simulink model "solar_pv_protected_c07_circuit"  (R2026b)
(part 2 of 16)

      | モデルの範囲　　　　; Simscape標準コンデンサの集中定数表現。材質、DCバイアス、周波数依存ESR/ESL、寿命・温度特性を型番から自動再現するモデルではない。
      | モデル設定　　　　　; c=470 µF、r=1 µΩ、g=0 S。これらは保存モデルの設定値であり、すべてが実部品の保証値という意味ではない。
      | 損失の扱い　　　　　; 保存モデルの直列抵抗rと実部品の周波数・温度依存ESRは区別する。容量値が一致しても損失・リプル電流・寿命の成立確認にはならない。
      | 確認の範囲　　　　　; 本説明は保存回路の部品情報・端子割当・既存設計意図を整理したもの。今回の説明更新によって新たな動作試験や実機検証を実施した意味ではない。
      | 設計記録　　　　　　; evaluation\component_annotations_20261022_r01\before_graph.json
      | evaluation\component_annotations_20261022_r01\before_metadata.json
      | evaluation\protection_capacitor_integration_20261021_r01\final_delivery\independent_readback\physical_bom.json
      | evaluation\protection_capacitor_integration_20261021_r01\capacitor_review\capacitor_inventory_after_c04.json
      | evaluation\layout_readability_20261022_r01\capacitor_review\exact_snapshot_capacitor_review.json
      | 
      | 【周波数・ノイズと配置の説明】
      | 周波数面の役割　　　; 12 V共通電源の負荷変動へ、比較的大きな電荷を供給する。
      | 対象周波数の目安　　; 起動や負荷切替えなど比較的低い周波数側の蓄積が主眼。ただしハイブリッド電解は一般的な液体電解と同一特性ではなく、型番別のインピーダンス曲線で分担を決める。
      | ノイズの発生源　　　; U10/U12の消費電流変化とゲートドライバ負荷。旧K1のコイル負荷は現回路の発生源として扱わない。
      | 他のコンデンサとの差; C45の22 µF MLCCはU11直近のリプル経路を補う。本品470 µFが現回路で必要最小かは未確定で、旧負荷由来の容量を残している。
      | 周波数説明の範囲　　; 狙うノイズの周波数と、この部品が実装後に有効な周波数範囲は別である。実効容量、等価直列抵抗、等価直列インダクタンス、配線を含む自己共振で変わるため、型番名や公称容量だけから有効帯域の上限を断定しない。
      | 周波数説明の根拠　　; 村田製作所：コンデンサのインピーダンス・ESRと周波数の関係
      | https://article.murata.com/en-global/article/impedance-esr-frequency-characteristics-in-capacitors
      | TRACO POWER：TSR 1WI datasheet
      | https://www.tracopower.com/tsr1wi-datasheet
      | 
      | 【この説明欄の略語・記号】
      | 用語1　　　　　　　 ; MLCC：Multilayer Ceramic Capacitor（積層セラミックコンデンサ）。薄いセラミック誘電体と電極を重ねたコンデンサ。対象周波数は容量・実装・寄生成分で変わるため、MLCCという分類だけでは決めない。
      | 用語2　　　　　　　 ; ESR：Equivalent Series Resistance（等価直列抵抗）。コンデンサの損失を直列抵抗で表した量。周波数・温度で変わり、損失とリプル電圧に関係する。
      | 用語3　　　　　　　 ; ESL：Equivalent Series Inductance（等価直列インダクタンス）。端子や電極などの寄生インダクタンスを表す。高い周波数ではバイパス効果を制限する。
      | 用語4　　　　　　　 ; DC：Direct Current（直流）。ここでは直流電源または直流成分。DCバイアスはコンデンサに重なる直流電圧を指す。
      | 用語5　　　　　　　 ; IC：Integrated Circuit（集積回路）。複数の電子素子と機能を小さな半導体チップに集積した部品。
      | 用語6　　　　　　　 ; GND：Ground（回路の基準電位・電流帰路）。この図の共通基準。保護接地や大地への接続を意味するとは限らない。
      settings: AttributesFormatString=|
      | ハイブリッド
      | 470 µF
  C47 : fl_lib/Electrical/Electrical Elements/Capacitor  Description=|  c=1e-06 F  r=1e-6 Ohm  g=0 1/Ohm  i_specify=off  i_priority=None  i=0 A  i_nominal_specify=off  i_nominal_value=1  i_nominal_unit=A  v_specify=off  v_priority=None  v=0 V  v_nominal_specify=off  v_nominal_value=1  v_nominal_unit=V  vc_specify=off  vc_priority=High  vc=0 V  vc_nominal_specify=off  vc_nominal_value=1  vc_nominal_unit=V
      | この回路での名前　　; C47
      | 部品名　　　　　　　; GRM21BR71H105KA12L
      | この回路での役割　　; 12 Vから5 Vを作る補助電源U12の入力を支え、電流の脈動を近くで受け止めるためのコンデンサ。
      | ここでの動き　　　　; U12の12 V入力P12と共通GNDの間に1 µFを置き、入力端子近くで電流の短い往復経路を作る。同じ12 VにつながるC45・C46が離れていても、U12の直近に電荷を用意する役割。
      | 
      | 【詳しい働き・仕様・接続・確認の範囲】
      | 部品種別　　　　　　; 積層セラミックコンデンサ（MLCC）
      | 部品分類　　　　　　; 積層セラミックコンデンサ（MLCC）
      | 公称値　　　　　　　; 1uF 50V X7R
      | 配置目的　　　　　　; 5Vレギュレータ入力局所バイパス。対象ICはU12（TSR 1-2450）。
      | 意図する動作　　　　; U12のP12入力/GND直近。 U12は12V入力で外付22µF必須条件には該当しないが、配線/高周波源インピーダンスを持つ1µF局所Cを維持。
      | 端子と接続　　　　　; 1 1 → P12、2 2 → GND
      | モデルの範囲　　　　; Simscape標準コンデンサの集中定数表現。材質、DCバイアス、周波数依存ESR/ESL、寿命・温度特性を型番から自動再現するモデルではない。
      | モデル設定　　　　　; c=1 µF、r=1 µΩ、g=0 S。これらは保存モデルの設定値であり、すべてが実部品の保証値という意味ではない。
      | 損失の扱い　　　　　; 保存モデルの直列抵抗rと実部品の周波数・温度依存ESRは区別する。容量値が一致しても損失・リプル電流・寿命の成立確認にはならない。
      | 確認の範囲　　　　　; 本説明は保存回路の部品情報・端子割当・既存設計意図を整理したもの。今回の説明更新によって新たな動作試験や実機検証を実施した意味ではない。
      | 設計記録　　　　　　; evaluation\component_annotations_20261022_r01\before_graph.json
      | evaluation\component_annotations_20261022_r01\before_metadata.json
      | evaluation\protection_capacitor_integration_20261021_r01\final_delivery\independent_readback\physical_bom.json
      | evaluation\protection_capacitor_integration_20261021_r01\capacitor_review\capacitor_inventory_after_c04.json
      | evaluation\layout_readability_20261022_r01\capacitor_review\exact_snapshot_capacitor_review.json
      | 
      | 【周波数・ノイズと配置の説明】
      | 周波数面の役割　　　; 5 V補助電源U12の入力直近で電流の脈動を受け止める。
      | 対象周波数の目安　　; U12のメーカー指定スイッチング周波数400～600 kHz（典型500 kHz）と高調波を対象とする。
      | ノイズの発生源　　　; U12が12 Vから5 Vへ降圧する内部スイッチング、およびU7の負荷変動。
      | 他のコンデンサとの差; 離れた12 V共通容量C45/C46と同じネットでも、U12直近の短い電流経路を作る点に意味がある。
      | 周波数説明の範囲　　; 狙うノイズの周波数と、この部品が実装後に有効な周波数範囲は別である。実効容量、等価直列抵抗、等価直列インダクタンス、配線を含む自己共振で変わるため、型番名や公称容量だけから有効帯域の上限を断定しない。
      | 周波数説明の根拠　　; TRACO POWER：TSR 1 datasheet
      | https://www.tracopower.com/products/tsr1.pdf
      | 村田製作所：コンデンサを使いこなす
      | https://www.murata.com/en-GB/products/emc/emifil/library/knowhow/basic/chapter06-p8
      | 
      | 【この説明欄の略語・記号】
      | 用語1　　　　　　　 ; MLCC：Multilayer Ceramic Capacitor（積層セラミックコンデンサ）。薄いセラミック誘電体と電極を重ねたコンデンサ。対象周波数は容量・実装・寄生成分で変わるため、MLCCという分類だけでは決めない。
      | 用語2　　　　　　　 ; ESR：Equivalent Series Resistance（等価直列抵抗）。コンデンサの損失を直列抵抗で表した量。周波数・温度で変わり、損失とリプル電圧に関係する。
      | 用語3　　　　　　　 ; ESL：Equivalent Series Inductance（等価直列インダクタンス）。端子や電極などの寄生インダクタンスを表す。高い周波数ではバイパス効果を制限する。
      | 用語4　　　　　　　 ; DC：Direct Current（直流）。ここでは直流電源または直流成分。DCバイアスはコンデンサに重なる直流電圧を指す。
      | 用語5　　　　　　　 ; X7R：セラミックコンデンサの温度特性記号。英語の頭文字ではなく分類コード。X＝下限−55 ℃、7＝上限+125 ℃、R＝その範囲の容量変化±15%。直流バイアスによる容量変化は別に確認する。
      | 用語6　　　　　　　 ; IC：Integrated Circuit（集積回路）。複数の電子素子と機能を小さな半導体チップに集積した部品。
      | 用語7　　　　　　　 ; GND：Ground（回路の基準電位・電流帰路）。この図の共通基準。保護接地や大地への接続を意味するとは限らない。
      settings: AttributesFormatString=|
      | MLCC
      | 1 µF
  C48 : fl_lib/Electrical/Electrical Elements/Capacitor  Description=|  c=2.2e-05 F  r=1e-6 Ohm  g=0 1/Ohm  i_specify=off  i_priority=None  i=0 A  i_nominal_specify=off  i_nominal_value=1  i_nominal_unit=A  v_specify=off  v_priority=None  v=0 V  v_nominal_specify=off  v_nominal_value=1  v_nominal_unit=V  vc_specify=off  vc_priority=High  vc=0 V  vc_nominal_specify=off  vc_nominal_value=1  vc_nominal_unit=V
      | この回路での名前　　; C48
      | 部品名　　　　　　　; GRM32ER71E226KE15L
      | この回路での役割　　; マイコン基板などへ渡す5 V電源に電荷を蓄え、消費電流の変化を支えるためのコンデンサ。
      | ここでの動き　　　　; 補助電源U12の出力P5と共通GNDの間に22 µFを置き、マイコン基板などが一時的に必要とする電荷を補う。マイコン基板内の各部品のすぐ近くにある小容量コンデンサを置き換えるものではない。
      | 
      | 【詳しい働き・仕様・接続・確認の範囲】
      | 部品種別　　　　　　; 積層セラミックコンデンサ（MLCC）
      | 部品分類　　　　　　; 積層セラミックコンデンサ（MLCC）
      | 公称値　　　　　　　; 22uF 25V X7R
      | 配置目的　　　　　　; 5V出力局所バルク。対象ICはU12（TSR 1-2450）。
      | 意図する動作　　　　; P5分配点とMCU負荷を結ぶ短い往復配線。 Pico無線/制御負荷の過渡とLED電流窓を守るため22µF維持。U12出力max470µFにも余裕。
      | 端子と接続　　　　　; 1 1 → P5、2 2 → GND
      | モデルの範囲　　　　; Simscape標準コンデンサの集中定数表現。材質、DCバイアス、周波数依存ESR/ESL、寿命・温度特性を型番から自動再現するモデルではない。
      | モデル設定　　　　　; c=22 µF、r=1 µΩ、g=0 S。これらは保存モデルの設定値であり、すべてが実部品の保証値という意味ではない。
      | 損失の扱い　　　　　; 保存モデルの直列抵抗rと実部品の周波数・温度依存ESRは区別する。容量値が一致しても損失・リプル電流・寿命の成立確認にはならない。
      | 確認の範囲　　　　　; 本説明は保存回路の部品情報・端子割当・既存設計意図を整理したもの。今回の説明更新によって新たな動作試験や実機検証を実施した意味ではない。
      | 設計記録　　　　　　; evaluation\component_annotations_20261022_r01\before_graph.json
      | evaluation\component_annotations_20261022_r01\before_metadata.json
      | evaluation\protection_capacitor_integration_20261021_r01\final_delivery\independent_readback\physical_bom.json
      | evaluation\protection_capacitor_integration_20261021_r01\capacitor_review\capacitor_inventory_after_c04.json
      | evaluation\layout_readability_20261022_r01\capacitor_review\exact_snapshot_capacitor_review.json
      | 
      | 【周波数・ノイズと配置の説明】
      | 周波数面の役割　　　; 5 V出力の局所蓄積としてRP2040基板などの負荷変動を支える。
      | 対象周波数の目安　　; U12の400～600 kHz（典型500 kHz）の変換成分と高調波、マイコン/無線負荷によるより遅い電流変化を対象にする。
      | ノイズの発生源　　　; U12内部スイッチングとPico Wの処理・通信に伴う電源電流変化。ゲートドライバ入力の発光ダイオードへ供給する電流の変化も5 V系に流れる。
      | 他のコンデンサとの差; 22 µFのMLCCでも電荷蓄積を担う。マイコン基板内の各IC直近の小容量バイパスまで置き換えるものではない。
      | 周波数説明の範囲　　; 狙うノイズの周波数と、この部品が実装後に有効な周波数範囲は別である。実効容量、等価直列抵抗、等価直列インダクタンス、配線を含む自己共振で変わるため、型番名や公称容量だけから有効帯域の上限を断定しない。
      | 周波数説明の根拠　　; TRACO POWER：TSR 1 datasheet
      | https://www.tracopower.com/products/tsr1.pdf
      | TDK：Low-ESL Multilayer Ceramic Capacitors
      | https://product.tdk.com/system/files/dam/doc/content/emc-guidebook/en/eemc_product_01.pdf
      | 村田製作所：コンデンサを使いこなす
      | https://www.murata.com/en-GB/products/emc/emifil/library/knowhow/basic/chapter06-p8
      | 
      | 【この説明欄の略語・記号】
      | 用語1　　　　　　　 ; MLCC：Multilayer Ceramic Capacitor（積層セラミックコンデンサ）。薄いセラミック誘電体と電極を重ねたコンデンサ。対象周波数は容量・実装・寄生成分で変わるため、MLCCという分類だけでは決めない。
      | 用語2　　　　　　　 ; ESR：Equivalent Series Resistance（等価直列抵抗）。コンデンサの損失を直列抵抗で表した量。周波数・温度で変わり、損失とリプル電圧に関係する。
      | 用語3　　　　　　　 ; ESL：Equivalent Series Inductance（等価直列インダクタンス）。端子や電極などの寄生インダクタンスを表す。高い周波数ではバイパス効果を制限する。
      | 用語4　　　　　　　 ; DC：Direct Current（直流）。ここでは直流電源または直流成分。DCバイアスはコンデンサに重なる直流電圧を指す。
      | 用語5　　　　　　　 ; X7R：セラミックコンデンサの温度特性記号。英語の頭文字ではなく分類コード。X＝下限−55 ℃、7＝上限+125 ℃、R＝その範囲の容量変化±15%。直流バイアスによる容量変化は別に確認する。
      | 用語6　　　　　　　 ; IC：Integrated Circuit（集積回路）。複数の電子素子と機能を小さな半導体チップに集積した部品。
      | 用語7　　　　　　　 ; MCU：Microcontroller Unit（マイクロコントローラ）。プログラムを実行し、測定値の処理や出力制御を担当する小型計算機。
      | 用語8　　　　　　　 ; LED：Light-Emitting Diode（発光ダイオード）。本回路のゲートドライバ入力では光によって信号を伝え、入力側と出力側を絶縁するために用いる。
      | 用語9　　　　　　　 ; GND：Ground（回路の基準電位・電流帰路）。この図の共通基準。保護接地や大地への接続を意味するとは限らない。
      settings: AttributesFormatString=|
      | MLCC
      | 22 µF
  C7 : fl_lib/Electrical/Electrical Elements/Capacitor  Description=|  c=3.3e-06 F  r=1e-6 Ohm  g=0 1/Ohm  i_specify=off  i_priority=None  i=0 A  i_nominal_specify=off  i_nominal_value=1  i_nominal_unit=A  v_specify=off  v_priority=None  v=0 V  v_nominal_specify=off  v_nominal_value=1  v_nominal_unit=V  vc_specify=off  vc_priority=High  vc=0 V  vc_nominal_specify=off  vc_nominal_value=1  vc_nominal_unit=V
      | この回路での名前　　; C7
      | 部品名　　　　　　　; R76IR433050H3J
      | この回路での役割　　; 主電力段の切替えに伴う短い電流を近くで受け持ち、入力側の大容量コンデンサを補うためのフィルムコンデンサ。
      | ここでの動き　　　　; 入力電源VINと共通GNDの間に置き、Q1・Q2の切替えに必要な電流の往復経路を短くする。C2〜C4の電解コンデンサとC8〜C10の積層セラミックコンデンサが受け持つ電流を補う設計。
      | 
      | 【詳しい働き・仕様・接続・確認の範囲】
      | 部品種別　　　　　　; フィルムコンデンサ
      | 部品分類　　　　　　; フィルムコンデンサ
      | 公称値　　　　　　　; 3.3 uF
      | 配置目的　　　　　　; 入力フィルム。対象はQ1/Q2、VIN、GND。
      | 意図する動作　　　　; 電力段のパルス電流閉路を短くし、電解だけへ高速成分を押し付けない。 3.3µF維持。10µFへの大型化は本削減数を増やさず、初回の要因を増やすため保留。
      | 端子と接続　　　　　; 2 n → GND、1 p → VIN
      | モデルの範囲　　　　; Simscape標準コンデンサの集中定数表現。材質、DCバイアス、周波数依存ESR/ESL、寿命・温度特性を型番から自動再現するモデルではない。
      | モデル設定　　　　　; c=3.3 µF、r=1 µΩ、g=0 S。これらは保存モデルの設定値であり、すべてが実部品の保証値という意味ではない。
      | 損失の扱い　　　　　; 保存モデルの直列抵抗rと実部品の周波数・温度依存ESRは区別する。容量値が一致しても損失・リプル電流・寿命の成立確認にはならない。
      | 確認の範囲　　　　　; 本説明は保存回路の部品情報・端子割当・既存設計意図を整理したもの。今回の説明更新によって新たな動作試験や実機検証を実施した意味ではない。
      | 設計記録　　　　　　; evaluation\component_annotations_20261022_r01\before_graph.json
      | evaluation\component_annotations_20261022_r01\before_metadata.json
      | evaluation\protection_capacitor_integration_20261021_r01\final_delivery\independent_readback\physical_bom.json
      | evaluation\protection_capacitor_integration_20261021_r01\capacitor_review\capacitor_inventory_after_c04.json
      | 
      | 【周波数・ノイズと配置の説明】
      | 周波数面の役割　　　; 主電力段の反復するパルス電流を受け、入力電解だけに高速成分が集中するのを補う。
      | 対象周波数の目安　　; 主スイッチング周波数とその高調波を対象とする。主電力段の既存比較計算では50 kHzを仮定している。これは比較シナリオの値であり、今回の保存図から実行中PWM周波数を測定した値ではない。 フィルムだから必ずMLCCと電解の中間周波数という固定分類にはしない。
      | ノイズの発生源　　　; Q1/Q2の切替えで入力ループの電流が急変する。配線や部品の寄生成分による振動も重なる。
      | 他のコンデンサとの差; 大容量のC2～C4は電荷蓄積、C8～C10は低い寄生インダクタンスを生かした局所的な帰路を狙う。本品3.3 µFはフィルムのパルス電流特性を使う意図であり、実際の分流は別確認。
      | 周波数説明の範囲　　; 狙うノイズの周波数と、この部品が実装後に有効な周波数範囲は別である。実効容量、等価直列抵抗、等価直列インダクタンス、配線を含む自己共振で変わるため、型番名や公称容量だけから有効帯域の上限を断定しない。
      | 周波数説明の根拠　　; 村田製作所：コンデンサのインピーダンス・ESRと周波数の関係
      | https://article.murata.com/en-global/article/impedance-esr-frequency-characteristics-in-capacitors
      | 村田製作所：コンデンサを使いこなす
      | https://www.murata.com/en-GB/products/emc/emifil/library/knowhow/basic/chapter06-p8
      | 
      | 【この説明欄の略語・記号】
      | 用語1　　　　　　　 ; MLCC：Multilayer Ceramic Capacitor（積層セラミックコンデンサ）。薄いセラミック誘電体と電極を重ねたコンデンサ。対象周波数は容量・実装・寄生成分で変わるため、MLCCという分類だけでは決めない。
      | 用語2　　　　　　　 ; ESR：Equivalent Series Resistance（等価直列抵抗）。コンデンサの損失を直列抵抗で表した量。周波数・温度で変わり、損失とリプル電圧に関係する。
      | 用語3　　　　　　　 ; ESL：Equivalent Series Inductance（等価直列インダクタンス）。端子や電極などの寄生インダクタンスを表す。高い周波数ではバイパス効果を制限する。
      | 用語4　　　　　　　 ; DC：Direct Current（直流）。ここでは直流電源または直流成分。DCバイアスはコンデンサに重なる直流電圧を指す。
      | 用語5　　　　　　　 ; PWM：Pulse Width Modulation（パルス幅変調）。周期に対するON時間の割合を変えて、スイッチの平均的な電力伝達を調整する方式。
      | 用語6　　　　　　　 ; GND：Ground（回路の基準電位・電流帰路）。この図の共通基準。保護接地や大地への接続を意味するとは限らない。
      | 用語7　　　　　　　 ; VIN/VOUT：入力電圧・出力電圧を表す端子／ネット名。INは入力、OUTは出力。電源変換器の電力端子なのか、検出用端子なのかは対象部品によって異なるため、端子と接続の説明に従う。
      settings: AttributesFormatString=|
      | フィルム
      | 3.3 µF
  C8 : fl_lib/Electrical/Electrical Elements/Capacitor  Description=|  c=2.2000000000000001e-06 F  r=1e-6 Ohm  g=0 1/Ohm  i_specify=off  i_priority=None  i=0 A  i_nominal_specify=off  i_nominal_value=1  i_nominal_unit=A  v_specify=off  v_priority=None  v=0 V  v_nominal_specify=off  v_nominal_value=1  v_nominal_unit=V  vc_specify=off  vc_priority=High  vc=0 V  vc_nominal_specify=off  vc_nominal_value=1  vc_nominal_unit=V
      | この回路での名前　　; C8
      | 部品名　　　　　　　; C5750X7T2E225K250KE
      | この回路での役割　　; 主電力段のすぐ近くで速い電流変化を受け止め、遠い電源配線へ流れ出す高周波成分を減らすためのコンデンサ。
      | ここでの動き　　　　; 入力電源VINと共通GNDの間に2.2 µFを3個並列に置き、Q1・Q2が切り替わる瞬間の電流に短い往復経路を作る。C2〜C4の大きな電荷蓄積を補う役割。
      | 
      | 【詳しい働き・仕様・接続・確認の範囲】
      | 部品種別　　　　　　; 積層セラミックコンデンサ（MLCC）
      | 部品分類　　　　　　; 積層セラミックコンデンサ（MLCC）
      | 公称値　　　　　　　; 2.2 uF
      | 配置目的　　　　　　; 入力高速バイパス。対象はQ1ドレインとQ2ソース間のホットループ。
      | 意図する動作　　　　; 現構成は2.2 µFを3個。電力段付近でパルス電流の短い往復経路を作る意図。DCバイアス下の実効容量と高周波の分流・寄生は公称容量だけでは保証しない。
      | 端子と接続　　　　　; 2 n → GND、1 p → VIN
      | モデルの範囲　　　　; Simscape標準コンデンサの集中定数表現。材質、DCバイアス、周波数依存ESR/ESL、寿命・温度特性を型番から自動再現するモデルではない。
      | モデル設定　　　　　; c=2.2 µF、r=1 µΩ、g=0 S。これらは保存モデルの設定値であり、すべてが実部品の保証値という意味ではない。
      | 損失の扱い　　　　　; 保存モデルの直列抵抗rと実部品の周波数・温度依存ESRは区別する。容量値が一致しても損失・リプル電流・寿命の成立確認にはならない。
      | 確認の範囲　　　　　; 本説明は保存回路の部品情報・端子割当・既存設計意図を整理したもの。今回の説明更新によって新たな動作試験や実機検証を実施した意味ではない。
      | 設計記録　　　　　　; evaluation\component_annotations_20261022_r01\before_graph.json
      | evaluation\component_annotations_20261022_r01\before_metadata.json
      | evaluation\protection_capacitor_integration_20261021_r01\final_delivery\independent_readback\physical_bom.json
      | evaluation\protection_capacitor_integration_20261021_r01\capacitor_review\capacitor_inventory_after_c04.json
      | 
      | 【周波数・ノイズと配置の説明】
      | 材質の分類　　　　　; 本品の温度特性分類はX7T。-55～125 ℃の範囲で容量変化+22/-33%を規定する分類コードであり、英単語の略ではない。これは温度による変化の分類で、直流電圧を加えた際の実効容量や高周波特性は別に確認する。
      | 周波数面の役割　　　; 入力側の速い電流変化を電力段の近くで受け止め、遠い電源配線へ流れる高周波成分を減らす。
      | 対象周波数の目安　　; 主スイッチング周波数とその高調波、切替え端の速い変化を対象とする。主電力段の既存比較計算では50 kHzを仮定している。これは比較シナリオの値であり、今回の保存図から実行中PWM周波数を測定した値ではない。 50 kHzなら100 kHz、150 kHzなども成分となり、端の速さや寄生共振によってMHz域も検討対象になる。ただしMHz域での本品の有効性を保証した意味ではない。
      | ノイズの発生源　　　; Q1のオン期間に主電力段へ流れ込む入力電流が脈動し、Q1/Q2の切替え時には寄生容量の充放電電流も加わる。配線の寄生インダクタンスは急な電流変化を電圧の突起や振動に変える。
      | 他のコンデンサとの差; C2～C4の470 µF電解が比較的長い時間の電荷を補い、本品2.2 µFは短い局所経路を作る。C7フィルムとも分担し、3種類の役割には重なりがある。
      | 周波数説明の範囲　　; 狙うノイズの周波数と、この部品が実装後に有効な周波数範囲は別である。実効容量、等価直列抵抗、等価直列インダクタンス、配線を含む自己共振で変わるため、型番名や公称容量だけから有効帯域の上限を断定しない。
      | 周波数説明の根拠　　; TDK：C5750X7T2E225K250KE
      | https://product.tdk.com/ja/search/capacitor/ceramic/mlcc/info?part_no=C5750X7T2E225K250KE
      | 村田製作所：コンデンサのインピーダンス・ESRと周波数の関係
      | https://article.murata.com/en-global/article/impedance-esr-frequency-characteristics-in-capacitors
      | 村田製作所：コンデンサを使いこなす
      | https://www.murata.com/en-GB/products/emc/emifil/library/knowhow/basic/chapter06-p8
      | 
      | 【この説明欄の略語・記号】
      | 用語1　　　　　　　 ; MLCC：Multilayer Ceramic Capacitor（積層セラミックコンデンサ）。薄いセラミック誘電体と電極を重ねたコンデンサ。対象周波数は容量・実装・寄生成分で変わるため、MLCCという分類だけでは決めない。
      | 用語2　　　　　　　 ; ESR：Equivalent Series Resistance（等価直列抵抗）。コンデンサの損失を直列抵抗で表した量。周波数・温度で変わり、損失とリプル電圧に関係する。
      | 用語3　　　　　　　 ; ESL：Equivalent Series Inductance（等価直列インダクタンス）。端子や電極などの寄生インダクタンスを表す。高い周波数ではバイパス効果を制限する。
      | 用語4　　　　　　　 ; DC：Direct Current（直流）。ここでは直流電源または直流成分。DCバイアスはコンデンサに重なる直流電圧を指す。
      | 用語5　　　　　　　 ; X7T：セラミックコンデンサの温度特性記号。英語の頭文字ではなく分類コード。X＝下限−55 ℃、7＝上限+125 ℃、T＝容量変化+22%/−33%。直流バイアスによる容量変化は別に確認する。
      | 用語6　　　　　　　 ; PWM：Pulse Width Modulation（パルス幅変調）。周期に対するON時間の割合を変えて、スイッチの平均的な電力伝達を調整する方式。
      | 用語7　　　　　　　 ; GND：Ground（回路の基準電位・電流帰路）。この図の共通基準。保護接地や大地への接続を意味するとは限らない。
      | 用語8　　　　　　　 ; VIN/VOUT：入力電圧・出力電圧を表す端子／ネット名。INは入力、OUTは出力。電源変換器の電力端子なのか、検出用端子なのかは対象部品によって異なるため、端子と接続の説明に従う。
      settings: AttributesFormatString=|
      | MLCC
      | 2.2 µF
  C9 : fl_lib/Electrical/Electrical Elements/Capacitor  Description=|  c=2.2000000000000001e-06 F  r=1e-6 Ohm  g=0 1/Ohm  i_specify=off  i_priority=None  i=0 A  i_nominal_specify=off  i_nominal_value=1  i_nominal_unit=A  v_specify=off  v_priority=None  v=0 V  v_nominal_specify=off  v_nominal_value=1  v_nominal_unit=V  vc_specify=off  vc_priority=High  vc=0 V  vc_nominal_specify=off  vc_nominal_value=1  vc_nominal_unit=V
      | この回路での名前　　; C9
      | 部品名　　　　　　　; C5750X7T2E225K250KE
      | この回路での役割　　; 主電力段のすぐ近くで速い電流変化を受け止め、遠い電源配線へ流れ出す高周波成分を減らすためのコンデンサ。
      | ここでの動き　　　　; 入力電源VINと共通GNDの間に2.2 µFを3個並列に置き、Q1・Q2が切り替わる瞬間の電流に短い往復経路を作る。C2〜C4の大きな電荷蓄積を補う役割。
      | 
      | 【詳しい働き・仕様・接続・確認の範囲】
      | 部品種別　　　　　　; 積層セラミックコンデンサ（MLCC）
      | 部品分類　　　　　　; 積層セラミックコンデンサ（MLCC）
      | 公称値　　　　　　　; 2.2 uF
      | 配置目的　　　　　　; 入力高速バイパス。対象はQ1ドレインとQ2ソース間のホットループ。
      | 意図する動作　　　　; 現構成は2.2 µFを3個。電力段付近でパルス電流の短い往復経路を作る意図。DCバイアス下の実効容量と高周波の分流・寄生は公称容量だけでは保証しない。
      | 端子と接続　　　　　; 2 n → GND、1 p → VIN
      | モデルの範囲　　　　; Simscape標準コンデンサの集中定数表現。材質、DCバイアス、周波数依存ESR/ESL、寿命・温度特性を型番から自動再現するモデルではない。
      | モデル設定　　　　　; c=2.2 µF、r=1 µΩ、g=0 S。これらは保存モデルの設定値であり、すべてが実部品の保証値という意味ではない。
      | 損失の扱い　　　　　; 保存モデルの直列抵抗rと実部品の周波数・温度依存ESRは区別する。容量値が一致しても損失・リプル電流・寿命の成立確認にはならない。
      | 確認の範囲　　　　　; 本説明は保存回路の部品情報・端子割当・既存設計意図を整理したもの。今回の説明更新によって新たな動作試験や実機検証を実施した意味ではない。
      | 設計記録　　　　　　; evaluation\component_annotations_20261022_r01\before_graph.json
      | evaluation\component_annotations_20261022_r01\before_metadata.json
      | evaluation\protection_capacitor_integration_20261021_r01\final_delivery\independent_readback\physical_bom.json
      | evaluation\protection_capacitor_integration_20261021_r01\capacitor_review\capacitor_inventory_after_c04.json
      | 
      | 【周波数・ノイズと配置の説明】
      | 材質の分類　　　　　; 本品の温度特性分類はX7T。-55～125 ℃の範囲で容量変化+22/-33%を規定する分類コードであり、英単語の略ではない。これは温度による変化の分類で、直流電圧を加えた際の実効容量や高周波特性は別に確認する。
      | 周波数面の役割　　　; 入力側の速い電流変化を電力段の近くで受け止め、遠い電源配線へ流れる高周波成分を減らす。
      | 対象周波数の目安　　; 主スイッチング周波数とその高調波、切替え端の速い変化を対象とする。主電力段の既存比較計算では50 kHzを仮定している。これは比較シナリオの値であり、今回の保存図から実行中PWM周波数を測定した値ではない。 50 kHzなら100 kHz、150 kHzなども成分となり、端の速さや寄生共振によってMHz域も検討対象になる。ただしMHz域での本品の有効性を保証した意味ではない。
      | ノイズの発生源　　　; Q1のオン期間に主電力段へ流れ込む入力電流が脈動し、Q1/Q2の切替え時には寄生容量の充放電電流も加わる。配線の寄生インダクタンスは急な電流変化を電圧の突起や振動に変える。
      | 他のコンデンサとの差; C2～C4の470 µF電解が比較的長い時間の電荷を補い、本品2.2 µFは短い局所経路を作る。C7フィルムとも分担し、3種類の役割には重なりがある。
      | 周波数説明の範囲　　; 狙うノイズの周波数と、この部品が実装後に有効な周波数範囲は別である。実効容量、等価直列抵抗、等価直列インダクタンス、配線を含む自己共振で変わるため、型番名や公称容量だけから有効帯域の上限を断定しない。
      | 周波数説明の根拠　　; TDK：C5750X7T2E225K250KE
      | https://product.tdk.com/ja/search/capacitor/ceramic/mlcc/info?part_no=C5750X7T2E225K250KE
      | 村田製作所：コンデンサのインピーダンス・ESRと周波数の関係
      | https://article.murata.com/en-global/article/impedance-esr-frequency-characteristics-in-capacitors
      | 村田製作所：コンデンサを使いこなす
      | https://www.murata.com/en-GB/products/emc/emifil/library/knowhow/basic/chapter06-p8
      | 
      | 【この説明欄の略語・記号】
      | 用語1　　　　　　　 ; MLCC：Multilayer Ceramic Capacitor（積層セラミックコンデンサ）。薄いセラミック誘電体と電極を重ねたコンデンサ。対象周波数は容量・実装・寄生成分で変わるため、MLCCという分類だけでは決めない。
      | 用語2　　　　　　　 ; ESR：Equivalent Series Resistance（等価直列抵抗）。コンデンサの損失を直列抵抗で表した量。周波数・温度で変わり、損失とリプル電圧に関係する。
      | 用語3　　　　　　　 ; ESL：Equivalent Series Inductance（等価直列インダクタンス）。端子や電極などの寄生インダクタンスを表す。高い周波数ではバイパス効果を制限する。
      | 用語4　　　　　　　 ; DC：Direct Current（直流）。ここでは直流電源または直流成分。DCバイアスはコンデンサに重なる直流電圧を指す。
      | 用語5　　　　　　　 ; X7T：セラミックコンデンサの温度特性記号。英語の頭文字ではなく分類コード。X＝下限−55 ℃、7＝上限+125 ℃、T＝容量変化+22%/−33%。直流バイアスによる容量変化は別に確認する。
      | 用語6　　　　　　　 ; PWM：Pulse Width Modulation（パルス幅変調）。周期に対するON時間の割合を変えて、スイッチの平均的な電力伝達を調整する方式。
      | 用語7　　　　　　　 ; GND：Ground（回路の基準電位・電流帰路）。この図の共通基準。保護接地や大地への接続を意味するとは限らない。
      | 用語8　　　　　　　 ; VIN/VOUT：入力電圧・出力電圧を表す端子／ネット名。INは入力、OUTは出力。電源変換器の電力端子なのか、検出用端子なのかは対象部品によって異なるため、端子と接続の説明に従う。
      settings: AttributesFormatString=|
      | MLCC
      | 2.2 µF
  CircuitNet_BAT_PLUS : ConnectionLabel  Description=|  Label=BAT_PLUS
      | この回路での名前　　; BAT_PLUS
      | 種別　　　　　　　　; ConnectionLabel
      | この回路での役割　　; 保護回路の出力、充電経路のヒューズF3、電池側電圧測定の分圧抵抗R22上側を結ぶ。BT1正極へはF3を介してつながる。
      | この場所の直接接続　; F3（BT1と充電器の間の充電経路を保護するヒューズ／25A DC）: 2
      |                     ; P_COUT（保護回路出力側のコンデンサ／330 µF）: P
      |                     ; P_R7（BAT_PLUSからP_FBへ接続し、P_R8とともに出力電圧クランプの帰還比を作る／236 kΩ）: 1
      |                     ; P_RSNS（保護ICの電流検出抵抗／2.7 mΩ）: 2
      |                     ; P_U1（保護MOSFETを制御する保護IC／LTC4364IMS-1#PBF）: OUT
      | 直接接続の範囲　　　; このラベルから実際の線・分岐・明示的な境界端子だけを追った接続。同名ラベルによる離れた場所への接続はこの欄に含めない。
      | 同一ネットの主接続　; F3（BT1と充電器の間の充電経路を保護するヒューズ／25A DC）: 2
      |                     ; R22（電池側電圧の分圧抵抗・上側／75 kohm 0.1%）: 1
      |                     ; P_U1（保護MOSFETを制御する保護IC／LTC4364IMS-1#PBF）: OUT
      |                     ; P_RSNS（保護ICの電流検出抵抗／2.7 mΩ）: 2
      |                     ; P_COUT（保護回路出力側のコンデンサ／330 µF）: P
      |                     ; P_R7（BAT_PLUSからP_FBへ接続し、P_R8とともに出力電圧クランプの帰還比を作る／236 kΩ）: 1
      | 部品を介する経路　　; R22→R23の上側抵抗とR24の下側抵抗で分圧し、C21とADC U1のCH6へ渡す。ADC入力はBAT_PLUSと同じ導線ではない。F3の反対側はBT1正極のBAT_RAW。
      | 同一ネット全端子　　; F3: 2
      |                     ; P_COUT: P
      |                     ; P_R7: 1
      |                     ; P_RSNS: 2
      |                     ; P_U1: OUT
      |                     ; R22: 1
      | 接続部品数　　　　　; 6部品（部品番号で集計。同一ネット全体）
      | 接続端子数　　　　　; 6端子（423端子の部品対応表で集計。ラベル・境界ポートの重複は含めない）
      | この場所の端子数　　; 5端子／5部品（同名ラベルによる接続を除く）
      | 同階層同名ラベル数　; 2個（このラベル自身を含む）
      | 全階層の接続ラベル　; 2個（実際に同じノードへつながるラベル。名前が違う別名も含む）
      | 接続ルール　　　　　; 同じ階層の同じラベル名を仮想配線として結ぶ。別のSubsystem内とは名前だけでつながらず、明示的なConnection Portと配線をたどる。色は用途の表示であり接続を決めない。
      | 確認の範囲　　　　　; 現在の保存回路の端子・配線から求めた静的接続。抵抗やICの内部を導線として短絡せずに集計した。説明の更新は動作シミュレーション、タイミング、実部品の性能・実機動作を保証するものではない。
      | 記録の基準　　　　　; measurement_label_layout_20261022_r01/after_layout_graph.json。部品対応表は端子名の対応付けにのみ使用。
      | 
      | 【この説明欄の略語・記号】
      | 用語1　　　　　　　 ; DC：Direct Current（直流）。ここでは直流電源または直流成分。DCバイアスはコンデンサに重なる直流電圧を指す。
      | 用語2　　　　　　　 ; ADC：Analog-to-Digital Converter（アナログ・デジタル変換器）。測定電圧をデジタル値へ変換する回路。電流や温度も、センサーで電圧へ変換した後に読み取る。
      | 用語3　　　　　　　 ; IC：Integrated Circuit（集積回路）。複数の電子素子と機能を小さな半導体チップに集積した部品。
      | 用語4　　　　　　　 ; CH：Channel（測定チャネル）。CH0〜CH7はADCの入力番号であり、同時測定を意味しない。
      | 用語5　　　　　　　 ; MOSFET：Metal-Oxide-Semiconductor Field-Effect Transistor（金属・酸化膜・半導体構造の電界効果トランジスタ）。ゲートとソースの電圧でドレインとソースの導通を制御する素子。N-MOSはNチャネル型を表す。
      | 用語6　　　　　　　 ; FB：Feedback（帰還）。出力などを検出して内部制御へ戻すための信号・端子。
  CircuitNet_MAIN_EN : ConnectionLabel  Description=|  Label=MAIN_EN
      | この回路での名前　　; MAIN_EN
      | 種別　　　　　　　　; ConnectionLabel
      | この回路での役割　　; RP2040基板U7のGP11から、保護回路の停止入力へ指令を渡す。直接同じノードなのは直列抵抗P_RSHDN_SERの入力側までで、保護ICのSHDNにはこの抵抗を介して接続する。
      | この場所の直接接続　; U7（RP2040搭載Pico W／SC0918）: 15(GP11)
      | 直接接続の範囲　　　; このラベルから実際の線・分岐・明示的な境界端子だけを追った接続。同名ラベルによる離れた場所への接続はこの欄に含めない。
      | 同一ネットの主接続　; U7（RP2040搭載Pico W／SC0918）: 15(GP11)
      |                     ; P_RSHDN_SER（RP2040のMAIN_ENとLTC4364のSHDN間へ入る／1 kΩ）: 1
      | 同一ネット全端子　　; P_RSHDN_SER: 1
      |                     ; U7: 15(GP11)
      | 接続部品数　　　　　; 2部品（部品番号で集計。同一ネット全体）
      | 接続端子数　　　　　; 2端子（423端子の部品対応表で集計。ラベル・境界ポートの重複は含めない）
      | この場所の端子数　　; 1端子／1部品（同名ラベルによる接続を除く）
      | 同階層同名ラベル数　; 2個（このラベル自身を含む）
      | 全階層の接続ラベル　; 2個（実際に同じノードへつながるラベル。名前が違う別名も含む）
      | 接続ルール　　　　　; 同じ階層の同じラベル名を仮想配線として結ぶ。別のSubsystem内とは名前だけでつながらず、明示的なConnection Portと配線をたどる。色は用途の表示であり接続を決めない。
      | 確認の範囲　　　　　; 現在の保存回路の端子・配線から求めた静的接続。抵抗やICの内部を導線として短絡せずに集計した。説明の更新は動作シミュレーション、タイミング、実部品の性能・実機動作を保証するものではない。
      | 記録の基準　　　　　; measurement_label_layout_20261022_r01/after_layout_graph.json。部品対応表は端子名の対応付けにのみ使用。
      | 
      | 【この説明欄の略語・記号】
      | 用語1　　　　　　　 ; IC：Integrated Circuit（集積回路）。複数の電子素子と機能を小さな半導体チップに集積した部品。
      | 用語2　　　　　　　 ; GPIO：General-Purpose Input/Output（汎用入出力端子）。入力・出力や周辺機能に割り当てられる端子。GPの後の数字はRP2040の端子信号番号で、基板上の物理ピン番号とは別。
      | 用語3　　　　　　　 ; SHDN：Shutdown（停止制御端子）。LTC4364ではLowで停止を指示する。Highは動作許可であり、保護判定を無効にするものではない。
      | 用語4　　　　　　　 ; EN：Enable（動作許可）。対象機能の動作を許可する信号。端子ごとの有効レベルや接続状態に従う。
  CircuitNet_VOUT : ConnectionLabel  Description=|  Label=VOUT
      | この回路での名前　　; VOUT
      | 種別　　　　　　　　; ConnectionLabel
      | この回路での役割　　; 降圧電力段の出力平滑コンデンサ、L1後の出力電流検出抵抗R2の出力側、保護回路の入力を結ぶ。保護回路より上流の電圧をR19の分圧回路でも測る。
      | この場所の直接接続　; C13（出力バルク／470 uF）: 1(p)
      |                     ; C14（出力バルク／470 uF）: 1(p)
      |                     ; C15（出力高速バイパス／10 uF）: 1(p)
      |                     ; C16（出力高速バイパス／10 uF）: 1(p)
      |                     ; R2（L1直後の出力電流を検出する4端子シャント抵抗／CSS4J-4026R-1L00F）: IM, KM
      | 直接接続の範囲　　　; このラベルから実際の線・分岐・明示的な境界端子だけを追った接続。同名ラベルによる離れた場所への接続はこの欄に含めない。
      | 同一ネットの主接続　; C13（出力バルク／470 uF）: 1(p)
      |                     ; C14（出力バルク／470 uF）: 1(p)
      |                     ; C15（出力高速バイパス／10 uF）: 1(p)
      |                     ; C16（出力高速バイパス／10 uF）: 1(p)
      |                     ; R2（L1直後の出力電流を検出する4端子シャント抵抗／CSS4J-4026R-1L00F）: IM, KM
      |                     ; U3（L1直後の出力電流の検出アンプ／INA241A3IDDFR）: 1(IN-)
      |                     ; P_Q1（充電器から蓄電池へ向かう電力経路を開閉し、起動時や異常時には流れる電流・出力電圧を制限するために置く／150V / 4.8mOhm max at25C10V）: D
      |                     ; R19（保護回路より上流の出力電圧の分圧抵抗・上側／75 kohm 0.1%）: 1
      | 部品を介する経路　　; R19→R20の上側抵抗とR21の下側抵抗で分圧し、C20とADC U1のCH2へ渡す。ADC入力はVOUTと同じ導線ではない。電流の測定経路はR2両端→U3→R26/C25→U1 CH3。R2より下流に出力コンデンサがあるため、過渡時の電池端子電流と常時同一ではない。
      | 同一ネット全端子　　; C13: 1(p)
      |                     ; C14: 1(p)
      |                     ; C15: 1(p)
      |                     ; C16: 1(p)
      |                     ; P_Q1: D
      |                     ; P_R1: 1
      |                     ; P_R4: 1
      |                     ; R2: IM, KM
      |                     ; R19: 1
      |                     ; U3: 1(IN-)
      | 接続部品数　　　　　; 10部品（部品番号で集計。同一ネット全体）
      | 接続端子数　　　　　; 11端子（423端子の部品対応表で集計。ラベル・境界ポートの重複は含めない）
      | この場所の端子数　　; 6端子／5部品（同名ラベルによる接続を除く）
      | 同階層同名ラベル数　; 3個（このラベル自身を含む）
      | 全階層の接続ラベル　; 5個（実際に同じノードへつながるラベル。名前が違う別名も含む）
      | 接続ルール　　　　　; 同じ階層の同じラベル名を仮想配線として結ぶ。別のSubsystem内とは名前だけでつながらず、明示的なConnection Portと配線をたどる。色は用途の表示であり接続を決めない。
      | 確認の範囲　　　　　; 現在の保存回路の端子・配線から求めた静的接続。抵抗やICの内部を導線として短絡せずに集計した。説明の更新は動作シミュレーション、タイミング、実部品の性能・実機動作を保証するものではない。
      | 記録の基準　　　　　; measurement_label_layout_20261022_r01/after_layout_graph.json。部品対応表は端子名の対応付けにのみ使用。
      | 
      | 【この説明欄の略語・記号】
      | 用語1　　　　　　　 ; ADC：Analog-to-Digital Converter（アナログ・デジタル変換器）。測定電圧をデジタル値へ変換する回路。電流や温度も、センサーで電圧へ変換した後に読み取る。
      | 用語2　　　　　　　 ; IC：Integrated Circuit（集積回路）。複数の電子素子と機能を小さな半導体チップに集積した部品。
      | 用語3　　　　　　　 ; CH：Channel（測定チャネル）。CH0〜CH7はADCの入力番号であり、同時測定を意味しない。
      | 用語4　　　　　　　 ; GND：Ground（回路の基準電位・電流帰路）。この図の共通基準。保護接地や大地への接続を意味するとは限らない。
      | 用語5　　　　　　　 ; VIN/VOUT：入力電圧・出力電圧を表す端子／ネット名。INは入力、OUTは出力。電源変換器の電力端子なのか、検出用端子なのかは対象部品によって異なるため、端子と接続の説明に従う。
      | 用語6　　　　　　　 ; IP/IM・KP/KM：4端子シャントの端子役割を区別する設計上の表記。IP/IMは主電流端子、KP/KMはKelvin（4端子測定）の検出端子。P/Mは正側・負側の区別であり、端子番号は採用部品の割当を参照する。
      | 用語7　　　　　　　 ; IN+/IN−：差動測定の正側・負側入力。電流検出アンプは両端子の電圧差を読む。IN−は必ずGNDという意味ではない。
  Connection Label : ConnectionLabel  Tag=simrfV2util1/Connection Label  Description=|  Label=GP6
      | この回路での名前　　; GP6
      | 種別　　　　　　　　; ConnectionLabel
      | この回路での役割　　; RP2040基板U7のGP6と、高側ゲート駆動の入力抵抗R34を結ぶPWM指令線。R34の先でQ3の第1ゲートを駆動し、光ゲートドライバの入力LED電流を制御する構成。
      | この場所の直接接続　; U7（RP2040搭載Pico W／SC0918）: 9(GP6)
      | 直接接続の範囲　　　; このラベルから実際の線・分岐・明示的な境界端子だけを追った接続。同名ラベルによる離れた場所への接続はこの欄に含めない。
      | 同一ネットの主接続　; U7（RP2040搭載Pico W／SC0918）: 9(GP6)
      |                     ; R34（高側LED制御MOSFETのゲート直列抵抗／330 ohm 1%）: 1
      | 同一ネット全端子　　; R34: 1
      |                     ; U7: 9(GP6)
      | 接続部品数　　　　　; 2部品（部品番号で集計。同一ネット全体）
      | 接続端子数　　　　　; 2端子（423端子の部品対応表で集計。ラベル・境界ポートの重複は含めない）
      | この場所の端子数　　; 1端子／1部品（同名ラベルによる接続を除く）
      | 同階層同名ラベル数　; 2個（このラベル自身を含む）
      | 全階層の接続ラベル　; 2個（実際に同じノードへつながるラベル。名前が違う別名も含む）
      | 接続ルール　　　　　; 同じ階層の同じラベル名を仮想配線として結ぶ。別のSubsystem内とは名前だけでつながらず、明示的なConnection Portと配線をたどる。色は用途の表示であり接続を決めない。
      | 確認の範囲　　　　　; 現在の保存回路の端子・配線から求めた静的接続。抵抗やICの内部を導線として短絡せずに集計した。説明の更新は動作シミュレーション、タイミング、実部品の性能・実機動作を保証するものではない。
      | 記録の基準　　　　　; measurement_label_layout_20261022_r01/after_layout_graph.json。部品対応表は端子名の対応付けにのみ使用。
      | 
      | 【この説明欄の略語・記号】
      | 用語1　　　　　　　 ; IC：Integrated Circuit（集積回路）。複数の電子素子と機能を小さな半導体チップに集積した部品。
      | 用語2　　　　　　　 ; PWM：Pulse Width Modulation（パルス幅変調）。周期に対するON時間の割合を変えて、スイッチの平均的な電力伝達を調整する方式。
      | 用語3　　　　　　　 ; GPIO：General-Purpose Input/Output（汎用入出力端子）。入力・出力や周辺機能に割り当てられる端子。GPの後の数字はRP2040の端子信号番号で、基板上の物理ピン番号とは別。
      | 用語4　　　　　　　 ; MOSFET：Metal-Oxide-Semiconductor Field-Effect Transistor（金属・酸化膜・半導体構造の電界効果トランジスタ）。ゲートとソースの電圧でドレインとソースの導通を制御する素子。N-MOSはNチャネル型を表す。
      | 用語5　　　　　　　 ; LED：Light-Emitting Diode（発光ダイオード）。本回路のゲートドライバ入力では光によって信号を伝え、入力側と出力側を絶縁するために用いる。
  Connection Label1 : ConnectionLabel  Tag=simrfV2util1/Connection Label  Description=|  Label=GP6
      | この回路での名前　　; GP6
      | 種別　　　　　　　　; ConnectionLabel
      | この回路での役割　　; RP2040基板U7のGP6と、高側ゲート駆動の入力抵抗R34を結ぶPWM指令線。R34の先でQ3の第1ゲートを駆動し、光ゲートドライバの入力LED電流を制御する構成。
      | この場所の直接接続　; R34（高側LED制御MOSFETのゲート直列抵抗／330 ohm 1%）: 1
      | 直接接続の範囲　　　; このラベルから実際の線・分岐・明示的な境界端子だけを追った接続。同名ラベルによる離れた場所への接続はこの欄に含めない。
      | 同一ネットの主接続　; U7（RP2040搭載Pico W／SC0918）: 9(GP6)
      |                     ; R34（高側LED制御MOSFETのゲート直列抵抗／330 ohm 1%）: 1
      | 同一ネット全端子　　; R34: 1
      |                     ; U7: 9(GP6)
      | 接続部品数　　　　　; 2部品（部品番号で集計。同一ネット全体）
      | 接続端子数　　　　　; 2端子（423端子の部品対応表で集計。ラベル・境界ポートの重複は含めない）
      | この場所の端子数　　; 1端子／1部品（同名ラベルによる接続を除く）
      | 同階層同名ラベル数　; 2個（このラベル自身を含む）
      | 全階層の接続ラベル　; 2個（実際に同じノードへつながるラベル。名前が違う別名も含む）
      | 接続ルール　　　　　; 同じ階層の同じラベル名を仮想配線として結ぶ。別のSubsystem内とは名前だけでつながらず、明示的なConnection Portと配線をたどる。色は用途の表示であり接続を決めない。
      | 確認の範囲　　　　　; 現在の保存回路の端子・配線から求めた静的接続。抵抗やICの内部を導線として短絡せずに集計した。説明の更新は動作シミュレーション、タイミング、実部品の性能・実機動作を保証するものではない。
      | 記録の基準　　　　　; measurement_label_layout_20261022_r01/after_layout_graph.json。部品対応表は端子名の対応付けにのみ使用。
      | 
      | 【この説明欄の略語・記号】
      | 用語1　　　　　　　 ; IC：Integrated Circuit（集積回路）。複数の電子素子と機能を小さな半導体チップに集積した部品。
      | 用語2　　　　　　　 ; PWM：Pulse Width Modulation（パルス幅変調）。周期に対するON時間の割合を変えて、スイッチの平均的な電力伝達を調整する方式。
      | 用語3　　　　　　　 ; GPIO：General-Purpose Input/Output（汎用入出力端子）。入力・出力や周辺機能に割り当てられる端子。GPの後の数字はRP2040の端子信号番号で、基板上の物理ピン番号とは別。
      | 用語4　　　　　　　 ; MOSFET：Metal-Oxide-Semiconductor Field-Effect Transistor（金属・酸化膜・半導体構造の電界効果トランジスタ）。ゲートとソースの電圧でドレインとソースの導通を制御する素子。N-MOSはNチャネル型を表す。
      | 用語5　　　　　　　 ; LED：Light-Emitting Diode（発光ダイオード）。本回路のゲートドライバ入力では光によって信号を伝え、入力側と出力側を絶縁するために用いる。
  Connection Label2 : ConnectionLabel  Tag=simrfV2util1/Connection Label  Description=|  Label=GP7
      | この回路での名前　　; GP7
      | 種別　　　　　　　　; ConnectionLabel
      | この回路での役割　　; RP2040基板U7のGP7と、低側ゲート駆動の入力抵抗R41を結ぶPWM指令線。R41の先でQ3の第2ゲートを駆動し、光ゲートドライバの入力LED電流を制御する構成。
      | この場所の直接接続　; U7（RP2040搭載Pico W／SC0918）: 10(GP7)
      | 直接接続の範囲　　　; このラベルから実際の線・分岐・明示的な境界端子だけを追った接続。同名ラベルによる離れた場所への接続はこの欄に含めない。
      | 同一ネットの主接続　; U7（RP2040搭載Pico W／SC0918）: 10(GP7)
      |                     ; R41（低側LED制御MOSFETのゲート直列抵抗／330 ohm 1%）: 1
      | 同一ネット全端子　　; R41: 1
      |                     ; U7: 10(GP7)
      | 接続部品数　　　　　; 2部品（部品番号で集計。同一ネット全体）
      | 接続端子数　　　　　; 2端子（423端子の部品対応表で集計。ラベル・境界ポートの重複は含めない）
      | この場所の端子数　　; 1端子／1部品（同名ラベルによる接続を除く）
      | 同階層同名ラベル数　; 2個（このラベル自身を含む）
      | 全階層の接続ラベル　; 2個（実際に同じノードへつながるラベル。名前が違う別名も含む）
      | 接続ルール　　　　　; 同じ階層の同じラベル名を仮想配線として結ぶ。別のSubsystem内とは名前だけでつながらず、明示的なConnection Portと配線をたどる。色は用途の表示であり接続を決めない。
      | 確認の範囲　　　　　; 現在の保存回路の端子・配線から求めた静的接続。抵抗やICの内部を導線として短絡せずに集計した。説明の更新は動作シミュレーション、タイミング、実部品の性能・実機動作を保証するものではない。
      | 記録の基準　　　　　; measurement_label_layout_20261022_r01/after_layout_graph.json。部品対応表は端子名の対応付けにのみ使用。
      | 
      | 【この説明欄の略語・記号】
      | 用語1　　　　　　　 ; IC：Integrated Circuit（集積回路）。複数の電子素子と機能を小さな半導体チップに集積した部品。
      | 用語2　　　　　　　 ; PWM：Pulse Width Modulation（パルス幅変調）。周期に対するON時間の割合を変えて、スイッチの平均的な電力伝達を調整する方式。
      | 用語3　　　　　　　 ; GPIO：General-Purpose Input/Output（汎用入出力端子）。入力・出力や周辺機能に割り当てられる端子。GPの後の数字はRP2040の端子信号番号で、基板上の物理ピン番号とは別。
      | 用語4　　　　　　　 ; MOSFET：Metal-Oxide-Semiconductor Field-Effect Transistor（金属・酸化膜・半導体構造の電界効果トランジスタ）。ゲートとソースの電圧でドレインとソースの導通を制御する素子。N-MOSはNチャネル型を表す。
      | 用語5　　　　　　　 ; LED：Light-Emitting Diode（発光ダイオード）。本回路のゲートドライバ入力では光によって信号を伝え、入力側と出力側を絶縁するために用いる。
  Connection Label3 : ConnectionLabel  Tag=simrfV2util1/Connection Label  Description=|  Label=GP7
      | この回路での名前　　; GP7
      | 種別　　　　　　　　; ConnectionLabel
      | この回路での役割　　; RP2040基板U7のGP7と、低側ゲート駆動の入力抵抗R41を結ぶPWM指令線。R41の先でQ3の第2ゲートを駆動し、光ゲートドライバの入力LED電流を制御する構成。
      | この場所の直接接続　; R41（低側LED制御MOSFETのゲート直列抵抗／330 ohm 1%）: 1
      | 直接接続の範囲　　　; このラベルから実際の線・分岐・明示的な境界端子だけを追った接続。同名ラベルによる離れた場所への接続はこの欄に含めない。
      | 同一ネットの主接続　; U7（RP2040搭載Pico W／SC0918）: 10(GP7)
      |                     ; R41（低側LED制御MOSFETのゲート直列抵抗／330 ohm 1%）: 1
      | 同一ネット全端子　　; R41: 1
      |                     ; U7: 10(GP7)
      | 接続部品数　　　　　; 2部品（部品番号で集計。同一ネット全体）
      | 接続端子数　　　　　; 2端子（423端子の部品対応表で集計。ラベル・境界ポートの重複は含めない）
      | この場所の端子数　　; 1端子／1部品（同名ラベルによる接続を除く）
      | 同階層同名ラベル数　; 2個（このラベル自身を含む）
      | 全階層の接続ラベル　; 2個（実際に同じノードへつながるラベル。名前が違う別名も含む）
      | 接続ルール　　　　　; 同じ階層の同じラベル名を仮想配線として結ぶ。別のSubsystem内とは名前だけでつながらず、明示的なConnection Portと配線をたどる。色は用途の表示であり接続を決めない。
      | 確認の範囲　　　　　; 現在の保存回路の端子・配線から求めた静的接続。抵抗やICの内部を導線として短絡せずに集計した。説明の更新は動作シミュレーション、タイミング、実部品の性能・実機動作を保証するものではない。
      | 記録の基準　　　　　; measurement_label_layout_20261022_r01/after_layout_graph.json。部品対応表は端子名の対応付けにのみ使用。
      | 
      | 【この説明欄の略語・記号】
      | 用語1　　　　　　　 ; IC：Integrated Circuit（集積回路）。複数の電子素子と機能を小さな半導体チップに集積した部品。
      | 用語2　　　　　　　 ; PWM：Pulse Width Modulation（パルス幅変調）。周期に対するON時間の割合を変えて、スイッチの平均的な電力伝達を調整する方式。
      | 用語3　　　　　　　 ; GPIO：General-Purpose Input/Output（汎用入出力端子）。入力・出力や周辺機能に割り当てられる端子。GPの後の数字はRP2040の端子信号番号で、基板上の物理ピン番号とは別。
      | 用語4　　　　　　　 ; MOSFET：Metal-Oxide-Semiconductor Field-Effect Transistor（金属・酸化膜・半導体構造の電界効果トランジスタ）。ゲートとソースの電圧でドレインとソースの導通を制御する素子。N-MOSはNチャネル型を表す。
      | 用語5　　　　　　　 ; LED：Light-Emitting Diode（発光ダイオード）。本回路のゲートドライバ入力では光によって信号を伝え、入力側と出力側を絶縁するために用いる。
  Connection Label4 : ConnectionLabel  Tag=simrfV2util1/Connection Label  Description=|  Label=BAT_RAW
      | この回路での名前　　; BAT_RAW
      | 種別　　　　　　　　; ConnectionLabel
      | この回路での役割　　; 蓄電池BT1の正極と、充電経路のヒューズF3・補助電源分岐のヒューズF4を結ぶ。電池端子側の電源ノード。
      | この場所の直接接続　; F4（BT1から補助電源への分岐を保護するヒューズ／3.2A DC）: 1
      | 直接接続の範囲　　　; このラベルから実際の線・分岐・明示的な境界端子だけを追った接続。同名ラベルによる離れた場所への接続はこの欄に含めない。
      | 同一ネットの主接続　; BT1（充電先の蓄電池／51.2V 100Ah LiFePO4）: +
      |                     ; F3（BT1と充電器の間の充電経路を保護するヒューズ／25A DC）: 1
      |                     ; F4（BT1から補助電源への分岐を保護するヒューズ／3.2A DC）: 1
      | 同一ネット全端子　　; BT1: +
      |                     ; F3: 1
      |                     ; F4: 1
      | 接続部品数　　　　　; 3部品（部品番号で集計。同一ネット全体）
      | 接続端子数　　　　　; 3端子（423端子の部品対応表で集計。ラベル・境界ポートの重複は含めない）
      | この場所の端子数　　; 1端子／1部品（同名ラベルによる接続を除く）
      | 同階層同名ラベル数　; 2個（このラベル自身を含む）
      | 全階層の接続ラベル　; 2個（実際に同じノードへつながるラベル。名前が違う別名も含む）
      | 接続ルール　　　　　; 同じ階層の同じラベル名を仮想配線として結ぶ。別のSubsystem内とは名前だけでつながらず、明示的なConnection Portと配線をたどる。色は用途の表示であり接続を決めない。
      | 確認の範囲　　　　　; 現在の保存回路の端子・配線から求めた静的接続。抵抗やICの内部を導線として短絡せずに集計した。説明の更新は動作シミュレーション、タイミング、実部品の性能・実機動作を保証するものではない。
      | 記録の基準　　　　　; measurement_label_layout_20261022_r01/after_layout_graph.json。部品対応表は端子名の対応付けにのみ使用。
      | 
      | 【この説明欄の略語・記号】
      | 用語1　　　　　　　 ; DC：Direct Current（直流）。ここでは直流電源または直流成分。DCバイアスはコンデンサに重なる直流電圧を指す。
      | 用語2　　　　　　　 ; IC：Integrated Circuit（集積回路）。複数の電子素子と機能を小さな半導体チップに集積した部品。
      | 用語3　　　　　　　 ; LiFePO4：Lithium Iron Phosphate（リン酸鉄リチウム）。電池の正極材料を示す化学式。英語の頭文字を並べた略語ではない。
  Connection Label5 : ConnectionLabel  Tag=simrfV2util1/Connection Label  Description=|  Label=BAT_RAW
      | この回路での名前　　; BAT_RAW
      | 種別　　　　　　　　; ConnectionLabel
      | この回路での役割　　; 蓄電池BT1の正極と、充電経路のヒューズF3・補助電源分岐のヒューズF4を結ぶ。電池端子側の電源ノード。
      | この場所の直接接続　; BT1（充電先の蓄電池／51.2V 100Ah LiFePO4）: +
      |                     ; F3（BT1と充電器の間の充電経路を保護するヒューズ／25A DC）: 1
      | 直接接続の範囲　　　; このラベルから実際の線・分岐・明示的な境界端子だけを追った接続。同名ラベルによる離れた場所への接続はこの欄に含めない。
      | 同一ネットの主接続　; BT1（充電先の蓄電池／51.2V 100Ah LiFePO4）: +
      |                     ; F3（BT1と充電器の間の充電経路を保護するヒューズ／25A DC）: 1
      |                     ; F4（BT1から補助電源への分岐を保護するヒューズ／3.2A DC）: 1
      | 同一ネット全端子　　; BT1: +
      |                     ; F3: 1
      |                     ; F4: 1
      | 接続部品数　　　　　; 3部品（部品番号で集計。同一ネット全体）
      | 接続端子数　　　　　; 3端子（423端子の部品対応表で集計。ラベル・境界ポートの重複は含めない）
      | この場所の端子数　　; 2端子／2部品（同名ラベルによる接続を除く）
      | 同階層同名ラベル数　; 2個（このラベル自身を含む）
      | 全階層の接続ラベル　; 2個（実際に同じノードへつながるラベル。名前が違う別名も含む）
      | 接続ルール　　　　　; 同じ階層の同じラベル名を仮想配線として結ぶ。別のSubsystem内とは名前だけでつながらず、明示的なConnection Portと配線をたどる。色は用途の表示であり接続を決めない。
      | 確認の範囲　　　　　; 現在の保存回路の端子・配線から求めた静的接続。抵抗やICの内部を導線として短絡せずに集計した。説明の更新は動作シミュレーション、タイミング、実部品の性能・実機動作を保証するものではない。
      | 記録の基準　　　　　; measurement_label_layout_20261022_r01/after_layout_graph.json。部品対応表は端子名の対応付けにのみ使用。
      | 
      | 【この説明欄の略語・記号】
      | 用語1　　　　　　　 ; DC：Direct Current（直流）。ここでは直流電源または直流成分。DCバイアスはコンデンサに重なる直流電圧を指す。
      | 用語2　　　　　　　 ; IC：Integrated Circuit（集積回路）。複数の電子素子と機能を小さな半導体チップに集積した部品。
      | 用語3　　　　　　　 ; LiFePO4：Lithium Iron Phosphate（リン酸鉄リチウム）。電池の正極材料を示す化学式。英語の頭文字を並べた略語ではない。
  D1 : ee_lib/Semiconductors & Converters/Diode  Description=|  Vf=0.6 V  Ron=0.3 Ohm  Goff=1e-8 S  N_series=1  N_parallel=1  ZenerEnable=true  BV=15 V  Rz=0.3 Ohm  enable_fault_composite=simscape.enum.onoff.off  i_specify=off  i_priority=None  i=0 A  i_nominal_specify=off  i_nominal_value=1  i_nominal_unit=A  v_specify=off  v_priority=None  v=0 V  v_nominal_specify=off  v_nominal_value=1  v_nominal_unit=V  ModelType=ee.enum.diode.idealModelType.pwl  TableType=ee.enum.diode.tableType.IfMat  IfMat=[.07, .12, .19, 1.75, 4.24, 7.32, 11.2; .16, .3, .72, 2.14, 5.02, 8.35, 13.12] A  VfMat=[.9, 1.15, 1.25, 1.5, 1.75, 2.17, 2.6, 2.85; .58, .68, .75, 1.1, 1.38, 1.77, 2.27, 2.7] V  TjVec=[25, 125] degC  VfVec=[.5, .7, .9, 1.3, 1.7, 2.1, 2.5] V  IfVec=[.1, .2, .5, 1, 2, 4, 7, 10] A  IrMat=[1e-06, 2e-06, 5e-06, 1e-05, 2.5e-05, 5e-05, .0001; 2e-06, 5e-06, 1e-05, 4e-05, 8e-05, .0002, .0005] A  VrMat=[10, 100, 200, 250, 300, 325, 350; 10, 70, 160, 220, 270, 300, 320] V  VrVec=[10, 20, 40, 50, 70, 80, 100] V  IrVec=[1e-06, 2e-06, 5e-06, 1e-05, 2e-05, 5e-05, .0001] A  rec_loss_model=ee.enum.diode.reverseRecoveryModelTabulateUpTo3D.fixed  ErecVal=0 J  scaleWithIandV=true  ErecMat=zeros(2, 3) J  ErecMat3D=zeros(2, 3, 2) J  TjrecVec=[25, 125] degC  IfrecVec=[.1, 1, 10] A  IrecVal=10 A  VrecVal=10 V  VrecVec=[0, 100] V  tFilter=1 / 1000 / 100 s  thermal_network_parameterization=ee.enum.thermalNetworkTopology.junctionCase  Rth=[0, 10] K/W  Rth_Cauer=[1, 3, 10] K/W  Rth_Foster=[.08, .14, .22, .16] K/W  thermal_mass_parameterization=ee.enum.thermalNetwork.timeconstant  thermal_mass=[0, 1] J/K  thermal_mass_Cauer=[.1, .3, 1] J/K  thermal_mass_Foster=[.001, .005, .05, .5] J/K  thermal_time_constant=[0, 10] s  thermal_time_constant_Cauer=[1, 3, 10] s  thermal_time_constant_Foster=[7e-05, .0007, .01, .08] s  thermal_mass_initial_temperatures=[25, 25] degC  thermal_mass_initial_temperatures_Cauer=[25, 25, 25] degC  thermal_mass_initial_temperatures_Foster=[25, 25, 25, 25] degC  junction_thermal_mass=0.01 J/K  junction_temperature_specify=off  junction_temperature_priority=None  junction_temperature=25 degC  junction_temperature_nominal_specify=off  junction_temperature_nominal_value=1  junction_temperature_nominal_unit=degC  ThermalPort=false  ModelTypePhysical=ee.enum.diode.physicalModelType.exponential  prmExp=ee.enum.diode.expParam.useTwo  I12=[.0137, .545] A  V12=[.6, .7] V  IS=1e-12 A  ec=1  I1=0.0137 A  V1=0.6 V  RS=0 Ohm  C_param=ee.enum.diode.capParam.fixed  CJ=0 pF  CJ0=5 pF  Vvec=[.1, 10, 100] V  Cvec=[3.5, 1, .4] pF  VJ=1 V  Mgrad=0.5  FC=0.5  Q_param=ee.enum.diode.recoveryParam.off  iRM=-7.15 A  iF=4 A  didt=-750 A/us  trr_factor=3  trr=115 ns  Qrr=150 nA*s  Vr=-600 V  Ls=150 nH  Erec=0.03 J  TT=50 ns  tau=100 ns  T_param=ee.enum.diode.temperatureParam.off  Tmeas=25 degC  I1_T2=0.245 A  V1_T2=0.5 V  IS_T2=1.25e-7 A  Tmeas2=125 degC  EG_param=ee.enum.diode.egapParam.material_si  EG=1.11 eV  XTI_param=ee.enum.diode.xtiParam.pn  XTI=3  dBVdT=0 V/K  Tdevice=25 degC  i_capacitor_specify=off  i_capacitor_priority=None  i_capacitor=0 A  i_capacitor_nominal_specify=off  i_capacitor_nominal_value=1  i_capacitor_nominal_unit=A  Qj_specify=off  Qj_priority=None  Qj=0 C  Qj_nominal_specify=off  Qj_nominal_value=1  Qj_nominal_unit=uC
      | この回路での名前　　; D1
      | 部品名　　　　　　　; BZT52H-C15,115
      | この回路での役割　　; 上側MOSFET Q1のゲートに過大な電圧がかかるのを抑える保護用ダイオード。
      | ここでの動き　　　　; Q1のゲートとソースSWの間に接続する。両者の電圧差が上がったときに電流を逃がし、ゲート電圧の上昇を抑える。
      | 
      | 【詳しい働き・仕様・接続・確認の範囲】
      | 部品種別　　　　　　; 上側ゲート保護ツェナーダイオード
      | 公称値　　　　　　　; 15V gate clamp
      | 配置目的　　　　　　; Q1のゲート–ソース間電圧が過大になるのを抑えるため、GATE_H–SW間へ配置する。
      | 意図する動作　　　　; 比較する電圧はGND基準ではなくQ1のソースSW基準。ツェナーの公称電圧は理想的な硬い電圧上限ではない。
      | 端子と接続　　　　　; 1 K → GATE_H、2 A → SW
      | モデルの範囲　　　　; Simscapeダイオード素子による近似。順方向損失、漏れ、温度依存、逆回復・接合容量の型番固有特性を完全に再現するものではない。
      | モデル設定　　　　　; Vf=600 mV、Ron=300 mΩ、BV=15 V。これらは保存モデルの設定値であり、すべてが実部品の保証値という意味ではない。
      | 確認の範囲　　　　　; 本説明は保存回路の部品情報・端子割当・既存設計意図を整理したもの。今回の説明更新によって新たな動作試験や実機検証を実施した意味ではない。
      | 設計記録　　　　　　; evaluation\component_annotations_20261022_r01\before_graph.json
      | evaluation\component_annotations_20261022_r01\before_metadata.json
      | evaluation\protection_capacitor_integration_20261021_r01\final_delivery\independent_readback\physical_bom.json
      | 
      | 【この説明欄の略語・記号】
      | 用語1　　　　　　　 ; MOSFET：Metal-Oxide-Semiconductor Field-Effect Transistor（金属・酸化膜・半導体構造の電界効果トランジスタ）。ゲートとソースの電圧でドレインとソースの導通を制御する素子。N-MOSはNチャネル型を表す。
      | 用語2　　　　　　　 ; BV：Breakdown Voltage（降伏電圧）。ダイオードなどに逆方向電圧を加えたときの降伏特性を表すモデル値。
      | 用語3　　　　　　　 ; Vf：Forward Voltage（順方向電圧）。ダイオードが順方向に電流を流すときの電圧降下。電流・温度で変わる。
      | 用語4　　　　　　　 ; Ron：On-Resistance（導通抵抗）。ここでは半導体ブロックのON状態の抵抗近似に用いる設定名。
      | 用語5　　　　　　　 ; GND：Ground（回路の基準電位・電流帰路）。この図の共通基準。保護接地や大地への接続を意味するとは限らない。
      | 用語6　　　　　　　 ; SW：Switching Node（スイッチング点）。主電力段の上下MOSFETとL1がつながる、電圧が高速に切り替わる点。GNDとは別電位。
      settings: AttributesFormatString=ツェナー 15 V
  D2 : ee_lib/Semiconductors & Converters/Diode  Description=|  Vf=0.6 V  Ron=0.3 Ohm  Goff=1e-8 S  N_series=1  N_parallel=1  ZenerEnable=true  BV=15 V  Rz=0.3 Ohm  enable_fault_composite=simscape.enum.onoff.off  i_specify=off  i_priority=None  i=0 A  i_nominal_specify=off  i_nominal_value=1  i_nominal_unit=A  v_specify=off  v_priority=None  v=0 V  v_nominal_specify=off  v_nominal_value=1  v_nominal_unit=V  ModelType=ee.enum.diode.idealModelType.pwl  TableType=ee.enum.diode.tableType.IfMat  IfMat=[.07, .12, .19, 1.75, 4.24, 7.32, 11.2; .16, .3, .72, 2.14, 5.02, 8.35, 13.12] A  VfMat=[.9, 1.15, 1.25, 1.5, 1.75, 2.17, 2.6, 2.85; .58, .68, .75, 1.1, 1.38, 1.77, 2.27, 2.7] V  TjVec=[25, 125] degC  VfVec=[.5, .7, .9, 1.3, 1.7, 2.1, 2.5] V  IfVec=[.1, .2, .5, 1, 2, 4, 7, 10] A  IrMat=[1e-06, 2e-06, 5e-06, 1e-05, 2.5e-05, 5e-05, .0001; 2e-06, 5e-06, 1e-05, 4e-05, 8e-05, .0002, .0005] A  VrMat=[10, 100, 200, 250, 300, 325, 350; 10, 70, 160, 220, 270, 300, 320] V  VrVec=[10, 20, 40, 50, 70, 80, 100] V  IrVec=[1e-06, 2e-06, 5e-06, 1e-05, 2e-05, 5e-05, .0001] A  rec_loss_model=ee.enum.diode.reverseRecoveryModelTabulateUpTo3D.fixed  ErecVal=0 J  scaleWithIandV=true  ErecMat=zeros(2, 3) J  ErecMat3D=zeros(2, 3, 2) J  TjrecVec=[25, 125] degC  IfrecVec=[.1, 1, 10] A  IrecVal=10 A  VrecVal=10 V  VrecVec=[0, 100] V  tFilter=1 / 1000 / 100 s  thermal_network_parameterization=ee.enum.thermalNetworkTopology.junctionCase  Rth=[0, 10] K/W  Rth_Cauer=[1, 3, 10] K/W  Rth_Foster=[.08, .14, .22, .16] K/W  thermal_mass_parameterization=ee.enum.thermalNetwork.timeconstant  thermal_mass=[0, 1] J/K  thermal_mass_Cauer=[.1, .3, 1] J/K  thermal_mass_Foster=[.001, .005, .05, .5] J/K  thermal_time_constant=[0, 10] s  thermal_time_constant_Cauer=[1, 3, 10] s  thermal_time_constant_Foster=[7e-05, .0007, .01, .08] s  thermal_mass_initial_temperatures=[25, 25] degC  thermal_mass_initial_temperatures_Cauer=[25, 25, 25] degC  thermal_mass_initial_temperatures_Foster=[25, 25, 25, 25] degC  junction_thermal_mass=0.01 J/K  junction_temperature_specify=off  junction_temperature_priority=None  junction_temperature=25 degC  junction_temperature_nominal_specify=off  junction_temperature_nominal_value=1  junction_temperature_nominal_unit=degC  ThermalPort=false  ModelTypePhysical=ee.enum.diode.physicalModelType.exponential  prmExp=ee.enum.diode.expParam.useTwo  I12=[.0137, .545] A  V12=[.6, .7] V  IS=1e-12 A  ec=1  I1=0.0137 A  V1=0.6 V  RS=0 Ohm  C_param=ee.enum.diode.capParam.fixed  CJ=0 pF  CJ0=5 pF  Vvec=[.1, 10, 100] V  Cvec=[3.5, 1, .4] pF  VJ=1 V  Mgrad=0.5  FC=0.5  Q_param=ee.enum.diode.recoveryParam.off  iRM=-7.15 A  iF=4 A  didt=-750 A/us  trr_factor=3  trr=115 ns  Qrr=150 nA*s  Vr=-600 V  Ls=150 nH  Erec=0.03 J  TT=50 ns  tau=100 ns  T_param=ee.enum.diode.temperatureParam.off  Tmeas=25 degC  I1_T2=0.245 A  V1_T2=0.5 V  IS_T2=1.25e-7 A  Tmeas2=125 degC  EG_param=ee.enum.diode.egapParam.material_si  EG=1.11 eV  XTI_param=ee.enum.diode.xtiParam.pn  XTI=3  dBVdT=0 V/K  Tdevice=25 degC  i_capacitor_specify=off  i_capacitor_priority=None  i_capacitor=0 A  i_capacitor_nominal_specify=off  i_capacitor_nominal_value=1  i_capacitor_nominal_unit=A  Qj_specify=off  Qj_priority=None  Qj=0 C  Qj_nominal_specify=off  Qj_nominal_value=1  Qj_nominal_unit=uC
      | この回路での名前　　; D2
      | 部品名　　　　　　　; BZT52H-C15,115
      | この回路での役割　　; 下側MOSFET Q2のゲートに過大な電圧がかかるのを抑える保護用ダイオード。
      | ここでの動き　　　　; Q2のゲートとソース側GNDの間に接続し、両者の電圧差が上がったときに電流を逃がす。
      | 
      | 【詳しい働き・仕様・接続・確認の範囲】
      | 部品種別　　　　　　; 下側ゲート保護ツェナーダイオード
      | 公称値　　　　　　　; 15V gate clamp
      | 配置目的　　　　　　; Q2のゲート–ソース間電圧が過大になるのを抑えるため、GATE_L–GND間へ配置する。
      | 意図する動作　　　　; 連続・パルス電力、動抵抗、配線寄生を含むクランプ性能は未確認。
      | 端子と接続　　　　　; 1 K → GATE_L、2 A → GND
      | モデルの範囲　　　　; Simscapeダイオード素子による近似。順方向損失、漏れ、温度依存、逆回復・接合容量の型番固有特性を完全に再現するものではない。
      | モデル設定　　　　　; Vf=600 mV、Ron=300 mΩ、BV=15 V。これらは保存モデルの設定値であり、すべてが実部品の保証値という意味ではない。
      | 確認の範囲　　　　　; 本説明は保存回路の部品情報・端子割当・既存設計意図を整理したもの。今回の説明更新によって新たな動作試験や実機検証を実施した意味ではない。
      | 設計記録　　　　　　; evaluation\component_annotations_20261022_r01\before_graph.json
      | evaluation\component_annotations_20261022_r01\before_metadata.json
      | evaluation\protection_capacitor_integration_20261021_r01\final_delivery\independent_readback\physical_bom.json
      | 
      | 【この説明欄の略語・記号】
      | 用語1　　　　　　　 ; BV：Breakdown Voltage（降伏電圧）。ダイオードなどに逆方向電圧を加えたときの降伏特性を表すモデル値。
      | 用語2　　　　　　　 ; Vf：Forward Voltage（順方向電圧）。ダイオードが順方向に電流を流すときの電圧降下。電流・温度で変わる。
      | 用語3　　　　　　　 ; Ron：On-Resistance（導通抵抗）。ここでは半導体ブロックのON状態の抵抗近似に用いる設定名。
      | 用語4　　　　　　　 ; GND：Ground（回路の基準電位・電流帰路）。この図の共通基準。保護接地や大地への接続を意味するとは限らない。
      settings: AttributesFormatString=ツェナー 15 V
  D3 : Subsystem  Description=|  mask(Simscape実部品合成記号){PartRef=D3, PartMPN=SS14-E3/61T, PartValue=SS14-E3/61T, DesignValue=40V 1A Schottky VSYS OR, SourceRef=vishay_ss14}
      | この回路での名前　　; D3
      | 部品名　　　　　　　; SS14-E3/61T
      | この回路での役割　　; マイコン基板U7へ5 Vを渡し、基板側から補助5 V電源へ電流が戻るのを抑えるダイオード。
      | ここでの動き　　　　; 補助5 V電源からマイコンの電源入力へ向かう方向には電流を通し、逆方向は抑える。電流を通す際には電圧降下と損失が生じる。
      | 
      | 【詳しい働き・仕様・接続・確認の範囲】
      | 部品種別　　　　　　; Pico電源用ショットキーダイオード
      | 公称値　　　　　　　; 40V 1A Schottky VSYS OR
      | 配置目的　　　　　　; P5からVSYS_5Vへ電力を供給し、VSYS側から5 V電源側への逆向き電流を抑える。
      | 意図する動作　　　　; 順方向電圧による電圧低下・損失がある。図面の方向はA=P5、K=VSYS_5V。USBなど他電源との全状態での適合は別確認。
      | 端子と接続　　　　　; 1 K → VSYS_5V、2 A → P5
      | モデルの範囲　　　　; Simscapeダイオード素子による近似。順方向損失、漏れ、温度依存、逆回復・接合容量の型番固有特性を完全に再現するものではない。
      | モデル設定　　　　　; Vf=600 mV、Ron=300 mΩ、BV=30 V。これらは保存モデルの設定値であり、すべてが実部品の保証値という意味ではない。
      | 確認の範囲　　　　　; 本説明は保存回路の部品情報・端子割当・既存設計意図を整理したもの。今回の説明更新によって新たな動作試験や実機検証を実施した意味ではない。
      | 設計記録　　　　　　; evaluation\component_annotations_20261022_r01\before_graph.json
      | evaluation\component_annotations_20261022_r01\before_metadata.json
      | evaluation\protection_capacitor_integration_20261021_r01\final_delivery\independent_readback\physical_bom.json
      | 
      | 【この説明欄の略語・記号】
      | 用語1　　　　　　　 ; USB：Universal Serial Bus（USB通信・給電規格）。Pico基板の接続・給電経路として現れる名称。
      | 用語2　　　　　　　 ; BV：Breakdown Voltage（降伏電圧）。ダイオードなどに逆方向電圧を加えたときの降伏特性を表すモデル値。
      | 用語3　　　　　　　 ; Vf：Forward Voltage（順方向電圧）。ダイオードが順方向に電流を流すときの電圧降下。電流・温度で変わる。
      | 用語4　　　　　　　 ; Ron：On-Resistance（導通抵抗）。ここでは半導体ブロックのON状態の抵抗近似に用いる設定名。
      settings: AttributesFormatString=Schottky SS14
      mask Display:
      | color('black');
      | plot([0 .34],[.5 .5]);
      | plot([.34 .34 .66 .34],[.2 .8 .5 .2]);
      | plot([.58 .66 .66 .74],[.8 .8 .2 .2]);
      | plot([.66 1],[.5 .5]);
      | text(0,.82,'2:A','horizontalAlignment','left');
      | text(1,.82,'1:K','horizontalAlignment','right');
  F1 : ee_lib/Switches & Breakers/Fuse  Description=|  prm=1  I_rated=1 A  melt_margin=1  T_fuse=0 s  I2t=1 A^2*s  I_vec=[1.9, 2, 2.5, 30] A  t_vec=[10000, 1, .3, .001] s  R_closed=0.01 Ohm  G_open=1e-8 1/Ohm  exposemeasurement=ee.enum.exposemeasurement.hidden
      | この回路での名前　　; F1
      | 部品名　　　　　　　; 0001.2706.11
      | この回路での役割　　; 12 V電源モジュールU11へ向かう補助電源入力の過電流に対処するヒューズ。
      | ここでの動き　　　　; 電池からU11へ流れる電流の経路に直列に入る。異常電流が続いたときに溶断して回路を切ることを狙う。補助分岐配線を受け持つF4との役割は別。
      | 
      | 【詳しい働き・仕様・接続・確認の範囲】
      | 部品種別　　　　　　; 補助電源モジュール用ヒューズ
      | 公称値　　　　　　　; 1.6A 300VDC time-lag T SMD
      | 配置目的　　　　　　; U11を含む補助電源入力の過電流に対処するために入れる。
      | 意図する動作　　　　; F4の補助配線保護とは保護対象が異なる。遮断協調・DC遮断能力・配線温度は公称電流だけでは保証されない。
      | 端子と接続　　　　　; 1 1 → BAT_AUX_FUSED、2 2 → BAT_AUX
      | モデルの範囲　　　　; Simscape標準ヒューズ。製品の時間–電流曲線、I²t、DCアーク遮断、遮断容量に適合済みのモデルではない。
      | モデル設定　　　　　; I_rated=1 A、R_closed=10 mΩ、melt_margin=1 。これらは保存モデルの設定値であり、すべてが実部品の保証値という意味ではない。
      | 確認の範囲　　　　　; 本説明は保存回路の部品情報・端子割当・既存設計意図を整理したもの。今回の説明更新によって新たな動作試験や実機検証を実施した意味ではない。
      | 設計記録　　　　　　; evaluation\component_annotations_20261022_r01\before_graph.json
      | evaluation\component_annotations_20261022_r01\before_metadata.json
      | evaluation\protection_capacitor_integration_20261021_r01\final_delivery\independent_readback\physical_bom.json
      | 
      | 【この説明欄の略語・記号】
      | 用語1　　　　　　　 ; DC：Direct Current（直流）。ここでは直流電源または直流成分。DCバイアスはコンデンサに重なる直流電圧を指す。
      | 用語2　　　　　　　 ; SMD：Surface-Mount Device（表面実装部品）。基板表面のパッドへはんだ付けする形式の部品。
      settings: AttributesFormatString=1.6A 300VDC time-lag T SMD
  F2 : ee_lib/Switches & Breakers/Fuse  Description=|  prm=1  I_rated=1 A  melt_margin=1  T_fuse=0 s  I2t=1 A^2*s  I_vec=[1.9, 2, 2.5, 30] A  t_vec=[10000, 1, .3, .001] s  R_closed=0.01 Ohm  G_open=1e-8 1/Ohm  exposemeasurement=ee.enum.exposemeasurement.hidden
      | この回路での名前　　; F2
      | 部品名　　　　　　　; HP10M20
      | この回路での役割　　; 太陽電池から充電器へ向かう入力配線を、過電流から保護するためのヒューズ。
      | ここでの動き　　　　; パネル列の出力に直列に入り、異常電流が続いたときに溶断して経路を切る。実際の遮断条件は電流の大きさと継続時間などに依存する。
      | 
      | 【詳しい働き・仕様・接続・確認の範囲】
      | 部品種別　　　　　　; PV入力ヒューズ
      | 公称値　　　　　　　; 20A gPV
      | 配置目的　　　　　　; PV入力配線の過電流保護を担う。
      | 意図する動作　　　　; 20 A gPVの部品情報を保持。パネル列の短絡電流、逆給電、直流電圧に対する適合・遮断協調は別確認。
      | 端子と接続　　　　　; 1 1 → PV_RAW、2 2 → PV_FUSED
      | モデルの範囲　　　　; Simscape標準ヒューズ。製品の時間–電流曲線、I²t、DCアーク遮断、遮断容量に適合済みのモデルではない。
      | モデル設定　　　　　; I_rated=1 A、R_closed=10 mΩ、melt_margin=1 。これらは保存モデルの設定値であり、すべてが実部品の保証値という意味ではない。
      | 確認の範囲　　　　　; 本説明は保存回路の部品情報・端子割当・既存設計意図を整理したもの。今回の説明更新によって新たな動作試験や実機検証を実施した意味ではない。
      | 設計記録　　　　　　; evaluation\component_annotations_20261022_r01\before_graph.json
      | evaluation\component_annotations_20261022_r01\before_metadata.json
      | evaluation\protection_capacitor_integration_20261021_r01\final_delivery\independent_readback\physical_bom.json
      | 
      | 【この説明欄の略語・記号】
      | 用語1　　　　　　　 ; DC：Direct Current（直流）。ここでは直流電源または直流成分。DCバイアスはコンデンサに重なる直流電圧を指す。
      | 用語2　　　　　　　 ; PV：Photovoltaic（太陽光発電）。光を電気へ変える発電方式。PVを含むネット名は太陽電池側の測定・電力経路を表す。
      settings: AttributesFormatString=20A gPV
  F3 : ee_lib/Switches & Breakers/Fuse  Description=|  prm=1  I_rated=1 A  melt_margin=1  T_fuse=0 s  I2t=1 A^2*s  I_vec=[1.9, 2, 2.5, 30] A  t_vec=[10000, 1, .3, .001] s  R_closed=0.01 Ohm  G_open=1e-8 1/Ohm  exposemeasurement=ee.enum.exposemeasurement.hidden
      | この回路での名前　　; F3
      | 部品名　　　　　　　; LP-CC-25
      | この回路での役割　　; 電池と充電器を結ぶ主充電経路を、過電流から保護するためのヒューズ。
      | ここでの動き　　　　; 電池プラス端子と保護回路出力の間に直列に入る。電池から故障箇所へ大電流が流れる場合も保護の対象になる。
      | 
      | 【詳しい働き・仕様・接続・確認の範囲】
      | 部品種別　　　　　　; 電池充電経路ヒューズ
      | 公称値　　　　　　　; 25A DC
      | 配置目的　　　　　　; BT1と充電器の間の大電流経路を保護する。
      | 意図する動作　　　　; 電池は故障時の電流供給源にもなる。25 Aは公称定格であり、25 Aで瞬時遮断する意味ではない。
      | 端子と接続　　　　　; 1 1 → BAT_RAW、2 2 → BAT_PLUS
      | モデルの範囲　　　　; Simscape標準ヒューズ。製品の時間–電流曲線、I²t、DCアーク遮断、遮断容量に適合済みのモデルではない。
      | モデル設定　　　　　; I_rated=1 A、R_closed=10 mΩ、melt_margin=1 。これらは保存モデルの設定値であり、すべてが実部品の保証値という意味ではない。
      | 確認の範囲　　　　　; 本説明は保存回路の部品情報・端子割当・既存設計意図を整理したもの。今回の説明更新によって新たな動作試験や実機検証を実施した意味ではない。
      | 設計記録　　　　　　; evaluation\component_annotations_20261022_r01\before_graph.json
      | evaluation\component_annotations_20261022_r01\before_metadata.json
      | evaluation\protection_capacitor_integration_20261021_r01\final_delivery\independent_readback\physical_bom.json
      | 
      | 【この説明欄の略語・記号】
      | 用語1　　　　　　　 ; DC：Direct Current（直流）。ここでは直流電源または直流成分。DCバイアスはコンデンサに重なる直流電圧を指す。
      settings: AttributesFormatString=25A DC
  F4 : ee_lib/Switches & Breakers/Fuse  Description=|  prm=1  I_rated=1 A  melt_margin=1  T_fuse=0 s  I2t=1 A^2*s  I_vec=[1.9, 2, 2.5, 30] A  t_vec=[10000, 1, .3, .001] s  R_closed=0.01 Ohm  G_open=1e-8 1/Ohm  exposemeasurement=ee.enum.exposemeasurement.hidden
      | この回路での名前　　; F4
      | 部品名　　　　　　　; LP-CC-3-2/10
      | この回路での役割　　; 電池から補助電源へ分岐する配線を、過電流から保護するためのヒューズ。
      | ここでの動き　　　　; 主充電経路のF3とは別に、電池からF1・U11へ向かう補助分岐に直列に入る。
      | 
      | 【詳しい働き・仕様・接続・確認の範囲】
      | 部品種別　　　　　　; 電池補助電源分岐ヒューズ
      | 公称値　　　　　　　; 3.2A DC
      | 配置目的　　　　　　; BT1から補助電源へ向かう分岐配線を保護する。
      | 意図する動作　　　　; F3の主充電経路とは別の分岐を対象とする。F1との遮断協調・実配線保護の成立は別確認。
      | 端子と接続　　　　　; 1 1 → BAT_RAW、2 2 → BAT_AUX_FUSED
      | モデルの範囲　　　　; Simscape標準ヒューズ。製品の時間–電流曲線、I²t、DCアーク遮断、遮断容量に適合済みのモデルではない。
      | モデル設定　　　　　; I_rated=1 A、R_closed=10 mΩ、melt_margin=1 。これらは保存モデルの設定値であり、すべてが実部品の保証値という意味ではない。
      | 確認の範囲　　　　　; 本説明は保存回路の部品情報・端子割当・既存設計意図を整理したもの。今回の説明更新によって新たな動作試験や実機検証を実施した意味ではない。
      | 設計記録　　　　　　; evaluation\component_annotations_20261022_r01\before_graph.json
      | evaluation\component_annotations_20261022_r01\before_metadata.json
      | evaluation\protection_capacitor_integration_20261021_r01\final_delivery\independent_readback\physical_bom.json
      | 
      | 【この説明欄の略語・記号】
      | 用語1　　　　　　　 ; DC：Direct Current（直流）。ここでは直流電源または直流成分。DCバイアスはコンデンサに重なる直流電圧を指す。
      settings: AttributesFormatString=3.2A DC
  GND_Label_001 : ConnectionLabel  Description=|  Label=GND
      | この回路での名前　　; GND
      | 種別　　　　　　　　; ConnectionLabel
      | この回路での役割　　; 電池BT1の負極、太陽電池列の負極、制御・測定・保護回路のGNDを結ぶ共通の帰路。高側駆動の浮動帰路SWとは別のノード。
      | 共通帰路の代表接続　; BT1（充電先の蓄電池／51.2V 100Ah LiFePO4）: -
      |                     ; PV1（直列太陽電池列の負極側パネル／400W panel 1/2）: -
      |                     ; U7（RP2040搭載Pico W／SC0918）: 3(GND), 8(GND), 13(GND), 18(GND), 23(GND), 28(GND), 33(AGND), 38(GND)
      |                     ; U1（外付けADC／MCP3208-CI/SL）: 8(CH7), 9(DGND), 14(AGND)
      |                     ; P_U1（保護MOSFETを制御する保護IC／LTC4364IMS-1#PBF）: GND
      |                     ; Q2（同期整流降圧回路の下側スイッチ／TK9R6E15Q5,S1X）: 3(S)
      |                     ; U9（低側の光ゲートドライバ／ACPL-P346-560E）: 4(VEE)
      |                     ; U10（高側ゲート用の浮動電源を作る絶縁DC/DC／UCC14131QDWNRQ1）: 1(GNDP), 2(GNDP), 5(GNDP), 8(GNDP), 9(GNDP), 10(GNDP), 11(GNDP), 12(GNDP), 13(GNDP), 14(GNDP), 15(GNDP), 16(GNDP), 17(GNDP), 18(GNDP)
      | この場所の直接接続　; BT1（充電先の蓄電池／51.2V 100Ah LiFePO4）: -
      | 直接接続の範囲　　　; このラベルから実際の線・分岐・明示的な境界端子だけを追った接続。同名ラベルによる離れた場所への接続はこの欄に含めない。
      | 同一ネット全端子　　; BT1: -
      |                     ; C1: 2(n)
      |                     ; C2: 2(n)
      |                     ; C3: 2(n)
      |                     ; C4: 2(n)
      |                     ; C7: 2(n)
      |                     ; C8: 2(n)
      |                     ; C9: 2(n)
      |                     ; C10: 2(n)
      |                     ; C13: 2(n)
      |                     ; C14: 2(n)
      |                     ; C15: 2(n)
      |                     ; C16: 2(n)
      |                     ; C17: 2
      |                     ; C18: 2
      |                     ; C19: 2
      |                     ; C20: 2
      |                     ; C21: 2
      |                     ; C22: 2
      |                     ; C23: 2
      |                     ; C24: 2
      |                     ; C25: 2
      |                     ; C26: 2
      |                     ; C27: 2
      |                     ; C28: 2
      |                     ; C29: 2
      |                     ; C30: 2
      |                     ; C31: 2
      |                     ; C33: 2
      |                     ; C34: 2
      |                     ; C35: 2
      |                     ; C36: 2
      |                     ; C40: 2
      |                     ; C41: 2
      |                     ; C42: 2
      |                     ; C43: 2
      |                     ; C44: 2
      |                     ; C45: 2
      |                     ; C46: 2
      |                     ; C47: 2
      |                     ; C48: 2
      |                     ; D2: 2(A)
      |                     ; PV1: -
      |                     ; P_CHG: N
      |                     ; P_COUT: N
      |                     ; P_CTMR: N
      |                     ; P_D1: A
      |                     ; P_R3: 2
      |                     ; P_R8: 2
      |                     ; P_RSHDN_PD: 2
      |                     ; P_U1: GND
      |                     ; Q2: 3(S)
      |                     ; Q3: 1(S1), 4(S2)
      |                     ; R1: 2(n)
      |                     ; R18: 2
      |                     ; R21: 2
      |                     ; R24: 2
      |                     ; R35: 2
      |                     ; R42: 2
      |                     ; R44: 2
      |                     ; R48: 2
      |                     ; U1: 8(CH7), 9(DGND), 14(AGND)
      |                     ; U2: 2(GND), 3(REF2), 4(RESERVED_GND)
      |                     ; U3: 2(GND), 3(REF2), 4(RESERVED_GND)
      |                     ; U4: 3(GND)
      |                     ; U5: 3(GND)
      |                     ; U6: 3(GND)
      |                     ; U7: 3(GND), 8(GND), 13(GND), 18(GND), 23(GND), 28(GND), 33(AGND), 38(GND)
      |                     ; U9: 4(VEE)
      |                     ; U10: 1(GNDP), 2(GNDP), 5(GNDP), 8(GNDP), 9(GNDP), 10(GNDP), 11(GNDP), 12(GNDP), 13(GNDP), 14(GNDP), 15(GNDP), 16(GNDP), 17(GNDP), 18(GNDP)
      |                     ; U11: 2(GND)
      |                     ; U12: 2(GND)
      | 接続部品数　　　　　; 72部品（部品番号で集計。同一ネット全体）
      | 接続端子数　　　　　; 99端子（423端子の部品対応表で集計。ラベル・境界ポートの重複は含めない）
      | この場所の端子数　　; 1端子／1部品（同名ラベルによる接続を除く）
      | 同階層同名ラベル数　; 75個（このラベル自身を含む）
      | 全階層の接続ラベル　; 87個（実際に同じノードへつながるラベル。名前が違う別名も含む）
      | 接続ルール　　　　　; 同じ階層の同じラベル名を仮想配線として結ぶ。別のSubsystem内とは名前だけでつながらず、明示的なConnection Portと配線をたどる。色は用途の表示であり接続を決めない。
      | 確認の範囲　　　　　; 現在の保存回路の端子・配線から求めた静的接続。抵抗やICの内部を導線として短絡せずに集計した。説明の更新は動作シミュレーション、タイミング、実部品の性能・実機動作を保証するものではない。
      | 記録の基準　　　　　; measurement_label_layout_20261022_r01/after_layout_graph.json。部品対応表は端子名の対応付けにのみ使用。
      | 
      | 【この説明欄の略語・記号】
      | 用語1　　　　　　　 ; DC：Direct Current（直流）。ここでは直流電源または直流成分。DCバイアスはコンデンサに重なる直流電圧を指す。
      | 用語2　　　　　　　 ; DC/DC：DC-to-DC Converter（直流電圧変換器）。直流入力を別の直流電圧へ変換する電源回路。絶縁の有無は個々の部品説明で確認する。
      | 用語3　　　　　　　 ; ADC：Analog-to-Digital Converter（アナログ・デジタル変換器）。測定電圧をデジタル値へ変換する回路。電流や温度も、センサーで電圧へ変換した後に読み取る。
      | 用語4　　　　　　　 ; IC：Integrated Circuit（集積回路）。複数の電子素子と機能を小さな半導体チップに集積した部品。
      | 用語5　　　　　　　 ; CH：Channel（測定チャネル）。CH0〜CH7はADCの入力番号であり、同時測定を意味しない。
      | 用語6　　　　　　　 ; MOSFET：Metal-Oxide-Semiconductor Field-Effect Transistor（金属・酸化膜・半導体構造の電界効果トランジスタ）。ゲートとソースの電圧でドレインとソースの導通を制御する素子。N-MOSはNチャネル型を表す。
      | 用語7　　　　　　　 ; LiFePO4：Lithium Iron Phosphate（リン酸鉄リチウム）。電池の正極材料を示す化学式。英語の頭文字を並べた略語ではない。
      | 用語8　　　　　　　 ; GND：Ground（回路の基準電位・電流帰路）。この図の共通基準。保護接地や大地への接続を意味するとは限らない。
      | 用語9　　　　　　　 ; AGND：Analog Ground（アナログ回路の基準端子）。アナログ部分の電流帰路。現図では共通GNDへ接続されるが、実装時の電流経路への配慮は別途必要。
      | 用語10　　　　　　　; DGND：Digital Ground（デジタル回路の基準端子）。デジタル部分の電流帰路。現図では共通GNDへ接続される。
      | 用語11　　　　　　　; VREF/REF：基準電圧を表す端子名。REFはReference（基準）の意味。ADCの変換尺度や電流アンプの出力基準に使う。REF1/REF2の接続電位は個別に確認する。
      | 用語12　　　　　　　; VCC/VDD/VEE/VS：ICの電源端子名。文字の歴史的な由来を現在の接続機能へ当てはめない。現回路のVEEはU8/U10では浮動基準SW、U9ではGND。各電圧・基準は端子と接続を参照する。
      | 用語13　　　　　　　; GNDP：U10の一次側電源の基準端子。絶縁電源の入力側GND。二次側基準VEE=SWと直接同一の導体ではない。
      | 用語14　　　　　　　; SW：Switching Node（スイッチング点）。主電力段の上下MOSFETとL1がつながる、電圧が高速に切り替わる点。GNDとは別電位。
  GND_Label_002 : ConnectionLabel  Description=|  Label=GND
      | この回路での名前　　; GND
      | 種別　　　　　　　　; ConnectionLabel
      | この回路での役割　　; 電池BT1の負極、太陽電池列の負極、制御・測定・保護回路のGNDを結ぶ共通の帰路。高側駆動の浮動帰路SWとは別のノード。
      | 共通帰路の代表接続　; BT1（充電先の蓄電池／51.2V 100Ah LiFePO4）: -
      |                     ; PV1（直列太陽電池列の負極側パネル／400W panel 1/2）: -
      |                     ; U7（RP2040搭載Pico W／SC0918）: 3(GND), 8(GND), 13(GND), 18(GND), 23(GND), 28(GND), 33(AGND), 38(GND)
      |                     ; U1（外付けADC／MCP3208-CI/SL）: 8(CH7), 9(DGND), 14(AGND)
      |                     ; P_U1（保護MOSFETを制御する保護IC／LTC4364IMS-1#PBF）: GND
      |                     ; Q2（同期整流降圧回路の下側スイッチ／TK9R6E15Q5,S1X）: 3(S)
      |                     ; U9（低側の光ゲートドライバ／ACPL-P346-560E）: 4(VEE)
      |                     ; U10（高側ゲート用の浮動電源を作る絶縁DC/DC／UCC14131QDWNRQ1）: 1(GNDP), 2(GNDP), 5(GNDP), 8(GNDP), 9(GNDP), 10(GNDP), 11(GNDP), 12(GNDP), 13(GNDP), 14(GNDP), 15(GNDP), 16(GNDP), 17(GNDP), 18(GNDP)
      | この場所の直接接続　; C1（SWスナバ／22 nF）: 2(n)
      | 直接接続の範囲　　　; このラベルから実際の線・分岐・明示的な境界端子だけを追った接続。同名ラベルによる離れた場所への接続はこの欄に含めない。
      | 同一ネット全端子　　; BT1: -
      |                     ; C1: 2(n)
      |                     ; C2: 2(n)
      |                     ; C3: 2(n)
      |                     ; C4: 2(n)
      |                     ; C7: 2(n)
      |                     ; C8: 2(n)
      |                     ; C9: 2(n)
      |                     ; C10: 2(n)
      |                     ; C13: 2(n)
      |                     ; C14: 2(n)
      |                     ; C15: 2(n)
      |                     ; C16: 2(n)
      |                     ; C17: 2
      |                     ; C18: 2
      |                     ; C19: 2
      |                     ; C20: 2
      |                     ; C21: 2
      |                     ; C22: 2
      |                     ; C23: 2
      |                     ; C24: 2
      |                     ; C25: 2
      |                     ; C26: 2
      |                     ; C27: 2
      |                     ; C28: 2
      |                     ; C29: 2
      |                     ; C30: 2
      |                     ; C31: 2
      |                     ; C33: 2
      |                     ; C34: 2
      |                     ; C35: 2
      |                     ; C36: 2
      |                     ; C40: 2
      |                     ; C41: 2
      |                     ; C42: 2
      |                     ; C43: 2
      |                     ; C44: 2
      |                     ; C45: 2
      |                     ; C46: 2
      |                     ; C47: 2
      |                     ; C48: 2
      |                     ; D2: 2(A)
      |                     ; PV1: -
      |                     ; P_CHG: N
      |                     ; P_COUT: N
      |                     ; P_CTMR: N
      |                     ; P_D1: A
      |                     ; P_R3: 2
      |                     ; P_R8: 2
      |                     ; P_RSHDN_PD: 2
      |                     ; P_U1: GND
      |                     ; Q2: 3(S)
      |                     ; Q3: 1(S1), 4(S2)
      |                     ; R1: 2(n)
      |                     ; R18: 2
      |                     ; R21: 2
      |                     ; R24: 2
      |                     ; R35: 2
      |                     ; R42: 2
      |                     ; R44: 2
      |                     ; R48: 2
      |                     ; U1: 8(CH7), 9(DGND), 14(AGND)
      |                     ; U2: 2(GND), 3(REF2), 4(RESERVED_GND)
      |                     ; U3: 2(GND), 3(REF2), 4(RESERVED_GND)
      |                     ; U4: 3(GND)
      |                     ; U5: 3(GND)
      |                     ; U6: 3(GND)
      |                     ; U7: 3(GND), 8(GND), 13(GND), 18(GND), 23(GND), 28(GND), 33(AGND), 38(GND)
      |                     ; U9: 4(VEE)
      |                     ; U10: 1(GNDP), 2(GNDP), 5(GNDP), 8(GNDP), 9(GNDP), 10(GNDP), 11(GNDP), 12(GNDP), 13(GNDP), 14(GNDP), 15(GNDP), 16(GNDP), 17(GNDP), 18(GNDP)
      |                     ; U11: 2(GND)
      |                     ; U12: 2(GND)
      | 接続部品数　　　　　; 72部品（部品番号で集計。同一ネット全体）
      | 接続端子数　　　　　; 99端子（423端子の部品対応表で集計。ラベル・境界ポートの重複は含めない）
      | この場所の端子数　　; 1端子／1部品（同名ラベルによる接続を除く）
      | 同階層同名ラベル数　; 75個（このラベル自身を含む）
      | 全階層の接続ラベル　; 87個（実際に同じノードへつながるラベル。名前が違う別名も含む）
      | 接続ルール　　　　　; 同じ階層の同じラベル名を仮想配線として結ぶ。別のSubsystem内とは名前だけでつながらず、明示的なConnection Portと配線をたどる。色は用途の表示であり接続を決めない。
      | 確認の範囲　　　　　; 現在の保存回路の端子・配線から求めた静的接続。抵抗やICの内部を導線として短絡せずに集計した。説明の更新は動作シミュレーション、タイミング、実部品の性能・実機動作を保証するものではない。
      | 記録の基準　　　　　; measurement_label_layout_20261022_r01/after_layout_graph.json。部品対応表は端子名の対応付けにのみ使用。
      | 
      | 【この説明欄の略語・記号】
      | 用語1　　　　　　　 ; DC：Direct Current（直流）。ここでは直流電源または直流成分。DCバイアスはコンデンサに重なる直流電圧を指す。
      | 用語2　　　　　　　 ; DC/DC：DC-to-DC Converter（直流電圧変換器）。直流入力を別の直流電圧へ変換する電源回路。絶縁の有無は個々の部品説明で確認する。
      | 用語3　　　　　　　 ; ADC：Analog-to-Digital Converter（アナログ・デジタル変換器）。測定電圧をデジタル値へ変換する回路。電流や温度も、センサーで電圧へ変換した後に読み取る。
      | 用語4　　　　　　　 ; IC：Integrated Circuit（集積回路）。複数の電子素子と機能を小さな半導体チップに集積した部品。
      | 用語5　　　　　　　 ; CH：Channel（測定チャネル）。CH0〜CH7はADCの入力番号であり、同時測定を意味しない。
      | 用語6　　　　　　　 ; MOSFET：Metal-Oxide-Semiconductor Field-Effect Transistor（金属・酸化膜・半導体構造の電界効果トランジスタ）。ゲートとソースの電圧でドレインとソースの導通を制御する素子。N-MOSはNチャネル型を表す。
      | 用語7　　　　　　　 ; LiFePO4：Lithium Iron Phosphate（リン酸鉄リチウム）。電池の正極材料を示す化学式。英語の頭文字を並べた略語ではない。
      | 用語8　　　　　　　 ; GND：Ground（回路の基準電位・電流帰路）。この図の共通基準。保護接地や大地への接続を意味するとは限らない。
      | 用語9　　　　　　　 ; AGND：Analog Ground（アナログ回路の基準端子）。アナログ部分の電流帰路。現図では共通GNDへ接続されるが、実装時の電流経路への配慮は別途必要。
      | 用語10　　　　　　　; DGND：Digital Ground（デジタル回路の基準端子）。デジタル部分の電流帰路。現図では共通GNDへ接続される。
      | 用語11　　　　　　　; VREF/REF：基準電圧を表す端子名。REFはReference（基準）の意味。ADCの変換尺度や電流アンプの出力基準に使う。REF1/REF2の接続電位は個別に確認する。
      | 用語12　　　　　　　; VCC/VDD/VEE/VS：ICの電源端子名。文字の歴史的な由来を現在の接続機能へ当てはめない。現回路のVEEはU8/U10では浮動基準SW、U9ではGND。各電圧・基準は端子と接続を参照する。
      | 用語13　　　　　　　; GNDP：U10の一次側電源の基準端子。絶縁電源の入力側GND。二次側基準VEE=SWと直接同一の導体ではない。
      | 用語14　　　　　　　; SW：Switching Node（スイッチング点）。主電力段の上下MOSFETとL1がつながる、電圧が高速に切り替わる点。GNDとは別電位。
  GND_Label_003 : ConnectionLabel  Description=|  Label=GND
      | この回路での名前　　; GND
      | 種別　　　　　　　　; ConnectionLabel
      | この回路での役割　　; 電池BT1の負極、太陽電池列の負極、制御・測定・保護回路のGNDを結ぶ共通の帰路。高側駆動の浮動帰路SWとは別のノード。
      | 共通帰路の代表接続　; BT1（充電先の蓄電池／51.2V 100Ah LiFePO4）: -
      |                     ; PV1（直列太陽電池列の負極側パネル／400W panel 1/2）: -
      |                     ; U7（RP2040搭載Pico W／SC0918）: 3(GND), 8(GND), 13(GND), 18(GND), 23(GND), 28(GND), 33(AGND), 38(GND)
      |                     ; U1（外付けADC／MCP3208-CI/SL）: 8(CH7), 9(DGND), 14(AGND)
      |                     ; P_U1（保護MOSFETを制御する保護IC／LTC4364IMS-1#PBF）: GND
      |                     ; Q2（同期整流降圧回路の下側スイッチ／TK9R6E15Q5,S1X）: 3(S)
      |                     ; U9（低側の光ゲートドライバ／ACPL-P346-560E）: 4(VEE)
      |                     ; U10（高側ゲート用の浮動電源を作る絶縁DC/DC／UCC14131QDWNRQ1）: 1(GNDP), 2(GNDP), 5(GNDP), 8(GNDP), 9(GNDP), 10(GNDP), 11(GNDP), 12(GNDP), 13(GNDP), 14(GNDP), 15(GNDP), 16(GNDP), 17(GNDP), 18(GNDP)
      | この場所の直接接続　; C10（入力高速バイパス／2.2 uF）: 2(n)
      | 直接接続の範囲　　　; このラベルから実際の線・分岐・明示的な境界端子だけを追った接続。同名ラベルによる離れた場所への接続はこの欄に含めない。
      | 同一ネット全端子　　; BT1: -
      |                     ; C1: 2(n)
      |                     ; C2: 2(n)
      |                     ; C3: 2(n)
      |                     ; C4: 2(n)
      |                     ; C7: 2(n)
      |                     ; C8: 2(n)
      |                     ; C9: 2(n)
      |                     ; C10: 2(n)
      |                     ; C13: 2(n)
      |                     ; C14: 2(n)
      |                     ; C15: 2(n)
      |                     ; C16: 2(n)
      |                     ; C17: 2
      |                     ; C18: 2
      |                     ; C19: 2
      |                     ; C20: 2
      |                     ; C21: 2
      |                     ; C22: 2
      |                     ; C23: 2
      |                     ; C24: 2
      |                     ; C25: 2
      |                     ; C26: 2
      |                     ; C27: 2
      |                     ; C28: 2
      |                     ; C29: 2
      |                     ; C30: 2
      |                     ; C31: 2
      |                     ; C33: 2
      |                     ; C34: 2
      |                     ; C35: 2
      |                     ; C36: 2
      |                     ; C40: 2
      |                     ; C41: 2
      |                     ; C42: 2
      |                     ; C43: 2
      |                     ; C44: 2
      |                     ; C45: 2
      |                     ; C46: 2
      |                     ; C47: 2
      |                     ; C48: 2
      |                     ; D2: 2(A)
      |                     ; PV1: -
      |                     ; P_CHG: N
      |                     ; P_COUT: N
      |                     ; P_CTMR: N
      |                     ; P_D1: A
      |                     ; P_R3: 2
      |                     ; P_R8: 2
      |                     ; P_RSHDN_PD: 2
      |                     ; P_U1: GND
      |                     ; Q2: 3(S)
      |                     ; Q3: 1(S1), 4(S2)
      |                     ; R1: 2(n)
      |                     ; R18: 2
      |                     ; R21: 2
      |                     ; R24: 2
      |                     ; R35: 2
      |                     ; R42: 2
      |                     ; R44: 2
      |                     ; R48: 2
      |                     ; U1: 8(CH7), 9(DGND), 14(AGND)
      |                     ; U2: 2(GND), 3(REF2), 4(RESERVED_GND)
      |                     ; U3: 2(GND), 3(REF2), 4(RESERVED_GND)
      |                     ; U4: 3(GND)
      |                     ; U5: 3(GND)
      |                     ; U6: 3(GND)
      |                     ; U7: 3(GND), 8(GND), 13(GND), 18(GND), 23(GND), 28(GND), 33(AGND), 38(GND)
      |                     ; U9: 4(VEE)
      |                     ; U10: 1(GNDP), 2(GNDP), 5(GNDP), 8(GNDP), 9(GNDP), 10(GNDP), 11(GNDP), 12(GNDP), 13(GNDP), 14(GNDP), 15(GNDP), 16(GNDP), 17(GNDP), 18(GNDP)
      |                     ; U11: 2(GND)
      |                     ; U12: 2(GND)
      | 接続部品数　　　　　; 72部品（部品番号で集計。同一ネット全体）
      | 接続端子数　　　　　; 99端子（423端子の部品対応表で集計。ラベル・境界ポートの重複は含めない）
      | この場所の端子数　　; 1端子／1部品（同名ラベルによる接続を除く）
      | 同階層同名ラベル数　; 75個（このラベル自身を含む）
      | 全階層の接続ラベル　; 87個（実際に同じノードへつながるラベル。名前が違う別名も含む）
      | 接続ルール　　　　　; 同じ階層の同じラベル名を仮想配線として結ぶ。別のSubsystem内とは名前だけでつながらず、明示的なConnection Portと配線をたどる。色は用途の表示であり接続を決めない。
      | 確認の範囲　　　　　; 現在の保存回路の端子・配線から求めた静的接続。抵抗やICの内部を導線として短絡せずに集計した。説明の更新は動作シミュレーション、タイミング、実部品の性能・実機動作を保証するものではない。
      | 記録の基準　　　　　; measurement_label_layout_20261022_r01/after_layout_graph.json。部品対応表は端子名の対応付けにのみ使用。
      | 
      | 【この説明欄の略語・記号】
      | 用語1　　　　　　　 ; DC：Direct Current（直流）。ここでは直流電源または直流成分。DCバイアスはコンデンサに重なる直流電圧を指す。
      | 用語2　　　　　　　 ; DC/DC：DC-to-DC Converter（直流電圧変換器）。直流入力を別の直流電圧へ変換する電源回路。絶縁の有無は個々の部品説明で確認する。
      | 用語3　　　　　　　 ; ADC：Analog-to-Digital Converter（アナログ・デジタル変換器）。測定電圧をデジタル値へ変換する回路。電流や温度も、センサーで電圧へ変換した後に読み取る。
      | 用語4　　　　　　　 ; IC：Integrated Circuit（集積回路）。複数の電子素子と機能を小さな半導体チップに集積した部品。
      | 用語5　　　　　　　 ; CH：Channel（測定チャネル）。CH0〜CH7はADCの入力番号であり、同時測定を意味しない。
      | 用語6　　　　　　　 ; MOSFET：Metal-Oxide-Semiconductor Field-Effect Transistor（金属・酸化膜・半導体構造の電界効果トランジスタ）。ゲートとソースの電圧でドレインとソースの導通を制御する素子。N-MOSはNチャネル型を表す。
      | 用語7　　　　　　　 ; LiFePO4：Lithium Iron Phosphate（リン酸鉄リチウム）。電池の正極材料を示す化学式。英語の頭文字を並べた略語ではない。
      | 用語8　　　　　　　 ; GND：Ground（回路の基準電位・電流帰路）。この図の共通基準。保護接地や大地への接続を意味するとは限らない。
      | 用語9　　　　　　　 ; AGND：Analog Ground（アナログ回路の基準端子）。アナログ部分の電流帰路。現図では共通GNDへ接続されるが、実装時の電流経路への配慮は別途必要。
      | 用語10　　　　　　　; DGND：Digital Ground（デジタル回路の基準端子）。デジタル部分の電流帰路。現図では共通GNDへ接続される。
      | 用語11　　　　　　　; VREF/REF：基準電圧を表す端子名。REFはReference（基準）の意味。ADCの変換尺度や電流アンプの出力基準に使う。REF1/REF2の接続電位は個別に確認する。
      | 用語12　　　　　　　; VCC/VDD/VEE/VS：ICの電源端子名。文字の歴史的な由来を現在の接続機能へ当てはめない。現回路のVEEはU8/U10では浮動基準SW、U9ではGND。各電圧・基準は端子と接続を参照する。
      | 用語13　　　　　　　; GNDP：U10の一次側電源の基準端子。絶縁電源の入力側GND。二次側基準VEE=SWと直接同一の導体ではない。
      | 用語14　　　　　　　; SW：Switching Node（スイッチング点）。主電力段の上下MOSFETとL1がつながる、電圧が高速に切り替わる点。GNDとは別電位。
  GND_Label_006 : ConnectionLabel  Description=|  Label=GND
      | この回路での名前　　; GND
      | 種別　　　　　　　　; ConnectionLabel
      | この回路での役割　　; 電池BT1の負極、太陽電池列の負極、制御・測定・保護回路のGNDを結ぶ共通の帰路。高側駆動の浮動帰路SWとは別のノード。
      | 共通帰路の代表接続　; BT1（充電先の蓄電池／51.2V 100Ah LiFePO4）: -
      |                     ; PV1（直列太陽電池列の負極側パネル／400W panel 1/2）: -
      |                     ; U7（RP2040搭載Pico W／SC0918）: 3(GND), 8(GND), 13(GND), 18(GND), 23(GND), 28(GND), 33(AGND), 38(GND)
      |                     ; U1（外付けADC／MCP3208-CI/SL）: 8(CH7), 9(DGND), 14(AGND)
      |                     ; P_U1（保護MOSFETを制御する保護IC／LTC4364IMS-1#PBF）: GND
      |                     ; Q2（同期整流降圧回路の下側スイッチ／TK9R6E15Q5,S1X）: 3(S)
      |                     ; U9（低側の光ゲートドライバ／ACPL-P346-560E）: 4(VEE)
      |                     ; U10（高側ゲート用の浮動電源を作る絶縁DC/DC／UCC14131QDWNRQ1）: 1(GNDP), 2(GNDP), 5(GNDP), 8(GNDP), 9(GNDP), 10(GNDP), 11(GNDP), 12(GNDP), 13(GNDP), 14(GNDP), 15(GNDP), 16(GNDP), 17(GNDP), 18(GNDP)
      | この場所の直接接続　; C13（出力バルク／470 uF）: 2(n)
      | 直接接続の範囲　　　; このラベルから実際の線・分岐・明示的な境界端子だけを追った接続。同名ラベルによる離れた場所への接続はこの欄に含めない。
      | 同一ネット全端子　　; BT1: -
      |                     ; C1: 2(n)
      |                     ; C2: 2(n)
      |                     ; C3: 2(n)
      |                     ; C4: 2(n)
      |                     ; C7: 2(n)
      |                     ; C8: 2(n)
      |                     ; C9: 2(n)
      |                     ; C10: 2(n)
      |                     ; C13: 2(n)
      |                     ; C14: 2(n)
      |                     ; C15: 2(n)
      |                     ; C16: 2(n)
      |                     ; C17: 2
      |                     ; C18: 2
      |                     ; C19: 2
      |                     ; C20: 2
      |                     ; C21: 2
      |                     ; C22: 2
      |                     ; C23: 2
      |                     ; C24: 2
      |                     ; C25: 2
      |                     ; C26: 2
      |                     ; C27: 2
      |                     ; C28: 2
      |                     ; C29: 2
      |                     ; C30: 2
      |                     ; C31: 2
      |                     ; C33: 2
      |                     ; C34: 2
      |                     ; C35: 2
      |                     ; C36: 2
      |                     ; C40: 2
      |                     ; C41: 2
      |                     ; C42: 2
      |                     ; C43: 2
      |                     ; C44: 2
      |                     ; C45: 2
      |                     ; C46: 2
      |                     ; C47: 2
      |                     ; C48: 2
      |                     ; D2: 2(A)
      |                     ; PV1: -
      |                     ; P_CHG: N
      |                     ; P_COUT: N
      |                     ; P_CTMR: N
      |                     ; P_D1: A
      |                     ; P_R3: 2
      |                     ; P_R8: 2
      |                     ; P_RSHDN_PD: 2
      |                     ; P_U1: GND
      |                     ; Q2: 3(S)
      |                     ; Q3: 1(S1), 4(S2)
      |                     ; R1: 2(n)
      |                     ; R18: 2
      |                     ; R21: 2
      |                     ; R24: 2
      |                     ; R35: 2
      |                     ; R42: 2
      |                     ; R44: 2
      |                     ; R48: 2
      |                     ; U1: 8(CH7), 9(DGND), 14(AGND)
      |                     ; U2: 2(GND), 3(REF2), 4(RESERVED_GND)
      |                     ; U3: 2(GND), 3(REF2), 4(RESERVED_GND)
      |                     ; U4: 3(GND)
      |                     ; U5: 3(GND)
      |                     ; U6: 3(GND)
      |                     ; U7: 3(GND), 8(GND), 13(GND), 18(GND), 23(GND), 28(GND), 33(AGND), 38(GND)
      |                     ; U9: 4(VEE)
      |                     ; U10: 1(GNDP), 2(GNDP), 5(GNDP), 8(GNDP), 9(GNDP), 10(GNDP), 11(GNDP), 12(GNDP), 13(GNDP), 14(GNDP), 15(GNDP), 16(GNDP), 17(GNDP), 18(GNDP)
      |                     ; U11: 2(GND)
      |                     ; U12: 2(GND)
      | 接続部品数　　　　　; 72部品（部品番号で集計。同一ネット全体）
      | 接続端子数　　　　　; 99端子（423端子の部品対応表で集計。ラベル・境界ポートの重複は含めない）
      | この場所の端子数　　; 1端子／1部品（同名ラベルによる接続を除く）
      | 同階層同名ラベル数　; 75個（このラベル自身を含む）
      | 全階層の接続ラベル　; 87個（実際に同じノードへつながるラベル。名前が違う別名も含む）
      | 接続ルール　　　　　; 同じ階層の同じラベル名を仮想配線として結ぶ。別のSubsystem内とは名前だけでつながらず、明示的なConnection Portと配線をたどる。色は用途の表示であり接続を決めない。
      | 確認の範囲　　　　　; 現在の保存回路の端子・配線から求めた静的接続。抵抗やICの内部を導線として短絡せずに集計した。説明の更新は動作シミュレーション、タイミング、実部品の性能・実機動作を保証するものではない。
      | 記録の基準　　　　　; measurement_label_layout_20261022_r01/after_layout_graph.json。部品対応表は端子名の対応付けにのみ使用。
      | 
      | 【この説明欄の略語・記号】
      | 用語1　　　　　　　 ; DC：Direct Current（直流）。ここでは直流電源または直流成分。DCバイアスはコンデンサに重なる直流電圧を指す。
      | 用語2　　　　　　　 ; DC/DC：DC-to-DC Converter（直流電圧変換器）。直流入力を別の直流電圧へ変換する電源回路。絶縁の有無は個々の部品説明で確認する。
      | 用語3　　　　　　　 ; ADC：Analog-to-Digital Converter（アナログ・デジタル変換器）。測定電圧をデジタル値へ変換する回路。電流や温度も、センサーで電圧へ変換した後に読み取る。
      | 用語4　　　　　　　 ; IC：Integrated Circuit（集積回路）。複数の電子素子と機能を小さな半導体チップに集積した部品。
      | 用語5　　　　　　　 ; CH：Channel（測定チャネル）。CH0〜CH7はADCの入力番号であり、同時測定を意味しない。
      | 用語6　　　　　　　 ; MOSFET：Metal-Oxide-Semiconductor Field-Effect Transistor（金属・酸化膜・半導体構造の電界効果トランジスタ）。ゲートとソースの電圧でドレインとソースの導通を制御する素子。N-MOSはNチャネル型を表す。
      | 用語7　　　　　　　 ; LiFePO4：Lithium Iron Phosphate（リン酸鉄リチウム）。電池の正極材料を示す化学式。英語の頭文字を並べた略語ではない。
      | 用語8　　　　　　　 ; GND：Ground（回路の基準電位・電流帰路）。この図の共通基準。保護接地や大地への接続を意味するとは限らない。
      | 用語9　　　　　　　 ; AGND：Analog Ground（アナログ回路の基準端子）。アナログ部分の電流帰路。現図では共通GNDへ接続されるが、実装時の電流経路への配慮は別途必要。
      | 用語10　　　　　　　; DGND：Digital Ground（デジタル回路の基準端子）。デジタル部分の電流帰路。現図では共通GNDへ接続される。
      | 用語11　　　　　　　; VREF/REF：基準電圧を表す端子名。REFはReference（基準）の意味。ADCの変換尺度や電流アンプの出力基準に使う。REF1/REF2の接続電位は個別に確認する。
      | 用語12　　　　　　　; VCC/VDD/VEE/VS：ICの電源端子名。文字の歴史的な由来を現在の接続機能へ当てはめない。現回路のVEEはU8/U10では浮動基準SW、U9ではGND。各電圧・基準は端子と接続を参照する。
      | 用語13　　　　　　　; GNDP：U10の一次側電源の基準端子。絶縁電源の入力側GND。二次側基準VEE=SWと直接同一の導体ではない。
      | 用語14　　　　　　　; SW：Switching Node（スイッチング点）。主電力段の上下MOSFETとL1がつながる、電圧が高速に切り替わる点。GNDとは別電位。
  GND_Label_007 : ConnectionLabel  Description=|  Label=GND
      | この回路での名前　　; GND
      | 種別　　　　　　　　; ConnectionLabel
      | この回路での役割　　; 電池BT1の負極、太陽電池列の負極、制御・測定・保護回路のGNDを結ぶ共通の帰路。高側駆動の浮動帰路SWとは別のノード。
      | 共通帰路の代表接続　; BT1（充電先の蓄電池／51.2V 100Ah LiFePO4）: -
      |                     ; PV1（直列太陽電池列の負極側パネル／400W panel 1/2）: -
      |                     ; U7（RP2040搭載Pico W／SC0918）: 3(GND), 8(GND), 13(GND), 18(GND), 23(GND), 28(GND), 33(AGND), 38(GND)
      |                     ; U1（外付けADC／MCP3208-CI/SL）: 8(CH7), 9(DGND), 14(AGND)
      |                     ; P_U1（保護MOSFETを制御する保護IC／LTC4364IMS-1#PBF）: GND
      |                     ; Q2（同期整流降圧回路の下側スイッチ／TK9R6E15Q5,S1X）: 3(S)
      |                     ; U9（低側の光ゲートドライバ／ACPL-P346-560E）: 4(VEE)
      |                     ; U10（高側ゲート用の浮動電源を作る絶縁DC/DC／UCC14131QDWNRQ1）: 1(GNDP), 2(GNDP), 5(GNDP), 8(GNDP), 9(GNDP), 10(GNDP), 11(GNDP), 12(GNDP), 13(GNDP), 14(GNDP), 15(GNDP), 16(GNDP), 17(GNDP), 18(GNDP)
      | この場所の直接接続　; C14（出力バルク／470 uF）: 2(n)
      | 直接接続の範囲　　　; このラベルから実際の線・分岐・明示的な境界端子だけを追った接続。同名ラベルによる離れた場所への接続はこの欄に含めない。
      | 同一ネット全端子　　; BT1: -
      |                     ; C1: 2(n)
      |                     ; C2: 2(n)
      |                     ; C3: 2(n)
      |                     ; C4: 2(n)
      |                     ; C7: 2(n)
      |                     ; C8: 2(n)
      |                     ; C9: 2(n)
      |                     ; C10: 2(n)
      |                     ; C13: 2(n)
      |                     ; C14: 2(n)
      |                     ; C15: 2(n)
      |                     ; C16: 2(n)
      |                     ; C17: 2
      |                     ; C18: 2
      |                     ; C19: 2
      |                     ; C20: 2
      |                     ; C21: 2
      |                     ; C22: 2
      |                     ; C23: 2
      |                     ; C24: 2
      |                     ; C25: 2
      |                     ; C26: 2
      |                     ; C27: 2
      |                     ; C28: 2
      |                     ; C29: 2
      |                     ; C30: 2
      |                     ; C31: 2
      |                     ; C33: 2
      |                     ; C34: 2
      |                     ; C35: 2
      |                     ; C36: 2
      |                     ; C40: 2
      |                     ; C41: 2
      |                     ; C42: 2
      |                     ; C43: 2
      |                     ; C44: 2
      |                     ; C45: 2
      |                     ; C46: 2
      |                     ; C47: 2
      |                     ; C48: 2
      |                     ; D2: 2(A)
      |                     ; PV1: -
      |                     ; P_CHG: N
      |                     ; P_COUT: N
      |                     ; P_CTMR: N
      |                     ; P_D1: A
      |                     ; P_R3: 2
      |                     ; P_R8: 2
      |                     ; P_RSHDN_PD: 2
      |                     ; P_U1: GND
      |                     ; Q2: 3(S)
      |                     ; Q3: 1(S1), 4(S2)
      |                     ; R1: 2(n)
      |                     ; R18: 2
      |                     ; R21: 2
      |                     ; R24: 2
      |                     ; R35: 2
      |                     ; R42: 2
      |                     ; R44: 2
      |                     ; R48: 2
      |                     ; U1: 8(CH7), 9(DGND), 14(AGND)
      |                     ; U2: 2(GND), 3(REF2), 4(RESERVED_GND)
      |                     ; U3: 2(GND), 3(REF2), 4(RESERVED_GND)
      |                     ; U4: 3(GND)
      |                     ; U5: 3(GND)
      |                     ; U6: 3(GND)
      |                     ; U7: 3(GND), 8(GND), 13(GND), 18(GND), 23(GND), 28(GND), 33(AGND), 38(GND)
      |                     ; U9: 4(VEE)
      |                     ; U10: 1(GNDP), 2(GNDP), 5(GNDP), 8(GNDP), 9(GNDP), 10(GNDP), 11(GNDP), 12(GNDP), 13(GNDP), 14(GNDP), 15(GNDP), 16(GNDP), 17(GNDP), 18(GNDP)
      |                     ; U11: 2(GND)
      |                     ; U12: 2(GND)
      | 接続部品数　　　　　; 72部品（部品番号で集計。同一ネット全体）
      | 接続端子数　　　　　; 99端子（423端子の部品対応表で集計。ラベル・境界ポートの重複は含めない）
      | この場所の端子数　　; 1端子／1部品（同名ラベルによる接続を除く）
      | 同階層同名ラベル数　; 75個（このラベル自身を含む）
      | 全階層の接続ラベル　; 87個（実際に同じノードへつながるラベル。名前が違う別名も含む）
      | 接続ルール　　　　　; 同じ階層の同じラベル名を仮想配線として結ぶ。別のSubsystem内とは名前だけでつながらず、明示的なConnection Portと配線をたどる。色は用途の表示であり接続を決めない。
      | 確認の範囲　　　　　; 現在の保存回路の端子・配線から求めた静的接続。抵抗やICの内部を導線として短絡せずに集計した。説明の更新は動作シミュレーション、タイミング、実部品の性能・実機動作を保証するものではない。
      | 記録の基準　　　　　; measurement_label_layout_20261022_r01/after_layout_graph.json。部品対応表は端子名の対応付けにのみ使用。
      | 
      | 【この説明欄の略語・記号】
      | 用語1　　　　　　　 ; DC：Direct Current（直流）。ここでは直流電源または直流成分。DCバイアスはコンデンサに重なる直流電圧を指す。
      | 用語2　　　　　　　 ; DC/DC：DC-to-DC Converter（直流電圧変換器）。直流入力を別の直流電圧へ変換する電源回路。絶縁の有無は個々の部品説明で確認する。
      | 用語3　　　　　　　 ; ADC：Analog-to-Digital Converter（アナログ・デジタル変換器）。測定電圧をデジタル値へ変換する回路。電流や温度も、センサーで電圧へ変換した後に読み取る。
      | 用語4　　　　　　　 ; IC：Integrated Circuit（集積回路）。複数の電子素子と機能を小さな半導体チップに集積した部品。
      | 用語5　　　　　　　 ; CH：Channel（測定チャネル）。CH0〜CH7はADCの入力番号であり、同時測定を意味しない。
      | 用語6　　　　　　　 ; MOSFET：Metal-Oxide-Semiconductor Field-Effect Transistor（金属・酸化膜・半導体構造の電界効果トランジスタ）。ゲートとソースの電圧でドレインとソースの導通を制御する素子。N-MOSはNチャネル型を表す。
      | 用語7　　　　　　　 ; LiFePO4：Lithium Iron Phosphate（リン酸鉄リチウム）。電池の正極材料を示す化学式。英語の頭文字を並べた略語ではない。
      | 用語8　　　　　　　 ; GND：Ground（回路の基準電位・電流帰路）。この図の共通基準。保護接地や大地への接続を意味するとは限らない。
      | 用語9　　　　　　　 ; AGND：Analog Ground（アナログ回路の基準端子）。アナログ部分の電流帰路。現図では共通GNDへ接続されるが、実装時の電流経路への配慮は別途必要。
      | 用語10　　　　　　　; DGND：Digital Ground（デジタル回路の基準端子）。デジタル部分の電流帰路。現図では共通GNDへ接続される。
      | 用語11　　　　　　　; VREF/REF：基準電圧を表す端子名。REFはReference（基準）の意味。ADCの変換尺度や電流アンプの出力基準に使う。REF1/REF2の接続電位は個別に確認する。
      | 用語12　　　　　　　; VCC/VDD/VEE/VS：ICの電源端子名。文字の歴史的な由来を現在の接続機能へ当てはめない。現回路のVEEはU8/U10では浮動基準SW、U9ではGND。各電圧・基準は端子と接続を参照する。
      | 用語13　　　　　　　; GNDP：U10の一次側電源の基準端子。絶縁電源の入力側GND。二次側基準VEE=SWと直接同一の導体ではない。
      | 用語14　　　　　　　; SW：Switching Node（スイッチング点）。主電力段の上下MOSFETとL1がつながる、電圧が高速に切り替わる点。GNDとは別電位。
  GND_Label_008 : ConnectionLabel  Description=|  Label=GND
      | この回路での名前　　; GND
      | 種別　　　　　　　　; ConnectionLabel
      | この回路での役割　　; 電池BT1の負極、太陽電池列の負極、制御・測定・保護回路のGNDを結ぶ共通の帰路。高側駆動の浮動帰路SWとは別のノード。
      | 共通帰路の代表接続　; BT1（充電先の蓄電池／51.2V 100Ah LiFePO4）: -
      |                     ; PV1（直列太陽電池列の負極側パネル／400W panel 1/2）: -
      |                     ; U7（RP2040搭載Pico W／SC0918）: 3(GND), 8(GND), 13(GND), 18(GND), 23(GND), 28(GND), 33(AGND), 38(GND)
      |                     ; U1（外付けADC／MCP3208-CI/SL）: 8(CH7), 9(DGND), 14(AGND)
      |                     ; P_U1（保護MOSFETを制御する保護IC／LTC4364IMS-1#PBF）: GND
      |                     ; Q2（同期整流降圧回路の下側スイッチ／TK9R6E15Q5,S1X）: 3(S)
      |                     ; U9（低側の光ゲートドライバ／ACPL-P346-560E）: 4(VEE)
      |                     ; U10（高側ゲート用の浮動電源を作る絶縁DC/DC／UCC14131QDWNRQ1）: 1(GNDP), 2(GNDP), 5(GNDP), 8(GNDP), 9(GNDP), 10(GNDP), 11(GNDP), 12(GNDP), 13(GNDP), 14(GNDP), 15(GNDP), 16(GNDP), 17(GNDP), 18(GNDP)
      | この場所の直接接続　; C15（出力高速バイパス／10 uF）: 2(n)
      | 直接接続の範囲　　　; このラベルから実際の線・分岐・明示的な境界端子だけを追った接続。同名ラベルによる離れた場所への接続はこの欄に含めない。
      | 同一ネット全端子　　; BT1: -
      |                     ; C1: 2(n)
      |                     ; C2: 2(n)
      |                     ; C3: 2(n)
      |                     ; C4: 2(n)
      |                     ; C7: 2(n)
      |                     ; C8: 2(n)
      |                     ; C9: 2(n)
      |                     ; C10: 2(n)
      |                     ; C13: 2(n)
      |                     ; C14: 2(n)
      |                     ; C15: 2(n)
      |                     ; C16: 2(n)
      |                     ; C17: 2
      |                     ; C18: 2
      |                     ; C19: 2
      |                     ; C20: 2
      |                     ; C21: 2
      |                     ; C22: 2
      |                     ; C23: 2
      |                     ; C24: 2
      |                     ; C25: 2
      |                     ; C26: 2
      |                     ; C27: 2
      |                     ; C28: 2
      |                     ; C29: 2
      |                     ; C30: 2
      |                     ; C31: 2
      |                     ; C33: 2
      |                     ; C34: 2
      |                     ; C35: 2
      |                     ; C36: 2
      |                     ; C40: 2
      |                     ; C41: 2
      |                     ; C42: 2
      |                     ; C43: 2
      |                     ; C44: 2
      |                     ; C45: 2
      |                     ; C46: 2
      |                     ; C47: 2
      |                     ; C48: 2
      |                     ; D2: 2(A)
      |                     ; PV1: -
      |                     ; P_CHG: N
      |                     ; P_COUT: N
      |                     ; P_CTMR: N
      |                     ; P_D1: A
      |                     ; P_R3: 2
      |                     ; P_R8: 2
      |                     ; P_RSHDN_PD: 2
      |                     ; P_U1: GND
      |                     ; Q2: 3(S)
      |                     ; Q3: 1(S1), 4(S2)
      |                     ; R1: 2(n)
      |                     ; R18: 2
      |                     ; R21: 2
      |                     ; R24: 2
      |                     ; R35: 2
      |                     ; R42: 2
      |                     ; R44: 2
      |                     ; R48: 2
      |                     ; U1: 8(CH7), 9(DGND), 14(AGND)
      |                     ; U2: 2(GND), 3(REF2), 4(RESERVED_GND)
      |                     ; U3: 2(GND), 3(REF2), 4(RESERVED_GND)
      |                     ; U4: 3(GND)
      |                     ; U5: 3(GND)
      |                     ; U6: 3(GND)
      |                     ; U7: 3(GND), 8(GND), 13(GND), 18(GND), 23(GND), 28(GND), 33(AGND), 38(GND)
      |                     ; U9: 4(VEE)
      |                     ; U10: 1(GNDP), 2(GNDP), 5(GNDP), 8(GNDP), 9(GNDP), 10(GNDP), 11(GNDP), 12(GNDP), 13(GNDP), 14(GNDP), 15(GNDP), 16(GNDP), 17(GNDP), 18(GNDP)
      |                     ; U11: 2(GND)
      |                     ; U12: 2(GND)
      | 接続部品数　　　　　; 72部品（部品番号で集計。同一ネット全体）
      | 接続端子数　　　　　; 99端子（423端子の部品対応表で集計。ラベル・境界ポートの重複は含めない）
      | この場所の端子数　　; 1端子／1部品（同名ラベルによる接続を除く）
      | 同階層同名ラベル数　; 75個（このラベル自身を含む）
      | 全階層の接続ラベル　; 87個（実際に同じノードへつながるラベル。名前が違う別名も含む）
      | 接続ルール　　　　　; 同じ階層の同じラベル名を仮想配線として結ぶ。別のSubsystem内とは名前だけでつながらず、明示的なConnection Portと配線をたどる。色は用途の表示であり接続を決めない。
      | 確認の範囲　　　　　; 現在の保存回路の端子・配線から求めた静的接続。抵抗やICの内部を導線として短絡せずに集計した。説明の更新は動作シミュレーション、タイミング、実部品の性能・実機動作を保証するものではない。
      | 記録の基準　　　　　; measurement_label_layout_20261022_r01/after_layout_graph.json。部品対応表は端子名の対応付けにのみ使用。
      | 
      | 【この説明欄の略語・記号】
      | 用語1　　　　　　　 ; DC：Direct Current（直流）。ここでは直流電源または直流成分。DCバイアスはコンデンサに重なる直流電圧を指す。
      | 用語2　　　　　　　 ; DC/DC：DC-to-DC Converter（直流電圧変換器）。直流入力を別の直流電圧へ変換する電源回路。絶縁の有無は個々の部品説明で確認する。
      | 用語3　　　　　　　 ; ADC：Analog-to-Digital Converter（アナログ・デジタル変換器）。測定電圧をデジタル値へ変換する回路。電流や温度も、センサーで電圧へ変換した後に読み取る。
      | 用語4　　　　　　　 ; IC：Integrated Circuit（集積回路）。複数の電子素子と機能を小さな半導体チップに集積した部品。
      | 用語5　　　　　　　 ; CH：Channel（測定チャネル）。CH0〜CH7はADCの入力番号であり、同時測定を意味しない。
      | 用語6　　　　　　　 ; MOSFET：Metal-Oxide-Semiconductor Field-Effect Transistor（金属・酸化膜・半導体構造の電界効果トランジスタ）。ゲートとソースの電圧でドレインとソースの導通を制御する素子。N-MOSはNチャネル型を表す。
      | 用語7　　　　　　　 ; LiFePO4：Lithium Iron Phosphate（リン酸鉄リチウム）。電池の正極材料を示す化学式。英語の頭文字を並べた略語ではない。
      | 用語8　　　　　　　 ; GND：Ground（回路の基準電位・電流帰路）。この図の共通基準。保護接地や大地への接続を意味するとは限らない。
      | 用語9　　　　　　　 ; AGND：Analog Ground（アナログ回路の基準端子）。アナログ部分の電流帰路。現図では共通GNDへ接続されるが、実装時の電流経路への配慮は別途必要。
      | 用語10　　　　　　　; DGND：Digital Ground（デジタル回路の基準端子）。デジタル部分の電流帰路。現図では共通GNDへ接続される。
      | 用語11　　　　　　　; VREF/REF：基準電圧を表す端子名。REFはReference（基準）の意味。ADCの変換尺度や電流アンプの出力基準に使う。REF1/REF2の接続電位は個別に確認する。
      | 用語12　　　　　　　; VCC/VDD/VEE/VS：ICの電源端子名。文字の歴史的な由来を現在の接続機能へ当てはめない。現回路のVEEはU8/U10では浮動基準SW、U9ではGND。各電圧・基準は端子と接続を参照する。
      | 用語13　　　　　　　; GNDP：U10の一次側電源の基準端子。絶縁電源の入力側GND。二次側基準VEE=SWと直接同一の導体ではない。
      | 用語14　　　　　　　; SW：Switching Node（スイッチング点）。主電力段の上下MOSFETとL1がつながる、電圧が高速に切り替わる点。GNDとは別電位。
  GND_Label_009 : ConnectionLabel  Description=|  Label=GND
      | この回路での名前　　; GND
      | 種別　　　　　　　　; ConnectionLabel
      | この回路での役割　　; 電池BT1の負極、太陽電池列の負極、制御・測定・保護回路のGNDを結ぶ共通の帰路。高側駆動の浮動帰路SWとは別のノード。
      | 共通帰路の代表接続　; BT1（充電先の蓄電池／51.2V 100Ah LiFePO4）: -
      |                     ; PV1（直列太陽電池列の負極側パネル／400W panel 1/2）: -
      |                     ; U7（RP2040搭載Pico W／SC0918）: 3(GND), 8(GND), 13(GND), 18(GND), 23(GND), 28(GND), 33(AGND), 38(GND)
      |                     ; U1（外付けADC／MCP3208-CI/SL）: 8(CH7), 9(DGND), 14(AGND)
      |                     ; P_U1（保護MOSFETを制御する保護IC／LTC4364IMS-1#PBF）: GND
      |                     ; Q2（同期整流降圧回路の下側スイッチ／TK9R6E15Q5,S1X）: 3(S)
      |                     ; U9（低側の光ゲートドライバ／ACPL-P346-560E）: 4(VEE)
      |                     ; U10（高側ゲート用の浮動電源を作る絶縁DC/DC／UCC14131QDWNRQ1）: 1(GNDP), 2(GNDP), 5(GNDP), 8(GNDP), 9(GNDP), 10(GNDP), 11(GNDP), 12(GNDP), 13(GNDP), 14(GNDP), 15(GNDP), 16(GNDP), 17(GNDP), 18(GNDP)
      | この場所の直接接続　; C16（出力高速バイパス／10 uF）: 2(n)
      | 直接接続の範囲　　　; このラベルから実際の線・分岐・明示的な境界端子だけを追った接続。同名ラベルによる離れた場所への接続はこの欄に含めない。
      | 同一ネット全端子　　; BT1: -
      |                     ; C1: 2(n)
      |                     ; C2: 2(n)
      |                     ; C3: 2(n)
      |                     ; C4: 2(n)
      |                     ; C7: 2(n)
      |                     ; C8: 2(n)
      |                     ; C9: 2(n)
      |                     ; C10: 2(n)
      |                     ; C13: 2(n)
      |                     ; C14: 2(n)
      |                     ; C15: 2(n)
      |                     ; C16: 2(n)
      |                     ; C17: 2
      |                     ; C18: 2
      |                     ; C19: 2
      |                     ; C20: 2
      |                     ; C21: 2
      |                     ; C22: 2
      |                     ; C23: 2
      |                     ; C24: 2
      |                     ; C25: 2
      |                     ; C26: 2
      |                     ; C27: 2
      |                     ; C28: 2
      |                     ; C29: 2
      |                     ; C30: 2
      |                     ; C31: 2
      |                     ; C33: 2
      |                     ; C34: 2
      |                     ; C35: 2
      |                     ; C36: 2
      |                     ; C40: 2
      |                     ; C41: 2
      |                     ; C42: 2
      |                     ; C43: 2
      |                     ; C44: 2
      |                     ; C45: 2
      |                     ; C46: 2
      |                     ; C47: 2
      |                     ; C48: 2
      |                     ; D2: 2(A)
      |                     ; PV1: -
      |                     ; P_CHG: N
      |                     ; P_COUT: N
      |                     ; P_CTMR: N
      |                     ; P_D1: A
      |                     ; P_R3: 2
      |                     ; P_R8: 2
      |                     ; P_RSHDN_PD: 2
      |                     ; P_U1: GND
      |                     ; Q2: 3(S)
      |                     ; Q3: 1(S1), 4(S2)
      |                     ; R1: 2(n)
      |                     ; R18: 2
      |                     ; R21: 2
      |                     ; R24: 2
      |                     ; R35: 2
      |                     ; R42: 2
      |                     ; R44: 2
      |                     ; R48: 2
      |                     ; U1: 8(CH7), 9(DGND), 14(AGND)
      |                     ; U2: 2(GND), 3(REF2), 4(RESERVED_GND)
      |                     ; U3: 2(GND), 3(REF2), 4(RESERVED_GND)
      |                     ; U4: 3(GND)
      |                     ; U5: 3(GND)
      |                     ; U6: 3(GND)
      |                     ; U7: 3(GND), 8(GND), 13(GND), 18(GND), 23(GND), 28(GND), 33(AGND), 38(GND)
      |                     ; U9: 4(VEE)
      |                     ; U10: 1(GNDP), 2(GNDP), 5(GNDP), 8(GNDP), 9(GNDP), 10(GNDP), 11(GNDP), 12(GNDP), 13(GNDP), 14(GNDP), 15(GNDP), 16(GNDP), 17(GNDP), 18(GNDP)
      |                     ; U11: 2(GND)
      |                     ; U12: 2(GND)
      | 接続部品数　　　　　; 72部品（部品番号で集計。同一ネット全体）
      | 接続端子数　　　　　; 99端子（423端子の部品対応表で集計。ラベル・境界ポートの重複は含めない）
      | この場所の端子数　　; 1端子／1部品（同名ラベルによる接続を除く）
      | 同階層同名ラベル数　; 75個（このラベル自身を含む）
      | 全階層の接続ラベル　; 87個（実際に同じノードへつながるラベル。名前が違う別名も含む）
      | 接続ルール　　　　　; 同じ階層の同じラベル名を仮想配線として結ぶ。別のSubsystem内とは名前だけでつながらず、明示的なConnection Portと配線をたどる。色は用途の表示であり接続を決めない。
      | 確認の範囲　　　　　; 現在の保存回路の端子・配線から求めた静的接続。抵抗やICの内部を導線として短絡せずに集計した。説明の更新は動作シミュレーション、タイミング、実部品の性能・実機動作を保証するものではない。
      | 記録の基準　　　　　; measurement_label_layout_20261022_r01/after_layout_graph.json。部品対応表は端子名の対応付けにのみ使用。
      | 
      | 【この説明欄の略語・記号】
      | 用語1　　　　　　　 ; DC：Direct Current（直流）。ここでは直流電源または直流成分。DCバイアスはコンデンサに重なる直流電圧を指す。
      | 用語2　　　　　　　 ; DC/DC：DC-to-DC Converter（直流電圧変換器）。直流入力を別の直流電圧へ変換する電源回路。絶縁の有無は個々の部品説明で確認する。
      | 用語3　　　　　　　 ; ADC：Analog-to-Digital Converter（アナログ・デジタル変換器）。測定電圧をデジタル値へ変換する回路。電流や温度も、センサーで電圧へ変換した後に読み取る。
      | 用語4　　　　　　　 ; IC：Integrated Circuit（集積回路）。複数の電子素子と機能を小さな半導体チップに集積した部品。
      | 用語5　　　　　　　 ; CH：Channel（測定チャネル）。CH0〜CH7はADCの入力番号であり、同時測定を意味しない。
      | 用語6　　　　　　　 ; MOSFET：Metal-Oxide-Semiconductor Field-Effect Transistor（金属・酸化膜・半導体構造の電界効果トランジスタ）。ゲートとソースの電圧でドレインとソースの導通を制御する素子。N-MOSはNチャネル型を表す。
      | 用語7　　　　　　　 ; LiFePO4：Lithium Iron Phosphate（リン酸鉄リチウム）。電池の正極材料を示す化学式。英語の頭文字を並べた略語ではない。
      | 用語8　　　　　　　 ; GND：Ground（回路の基準電位・電流帰路）。この図の共通基準。保護接地や大地への接続を意味するとは限らない。
      | 用語9　　　　　　　 ; AGND：Analog Ground（アナログ回路の基準端子）。アナログ部分の電流帰路。現図では共通GNDへ接続されるが、実装時の電流経路への配慮は別途必要。
      | 用語10　　　　　　　; DGND：Digital Ground（デジタル回路の基準端子）。デジタル部分の電流帰路。現図では共通GNDへ接続される。
      | 用語11　　　　　　　; VREF/REF：基準電圧を表す端子名。REFはReference（基準）の意味。ADCの変換尺度や電流アンプの出力基準に使う。REF1/REF2の接続電位は個別に確認する。
      | 用語12　　　　　　　; VCC/VDD/VEE/VS：ICの電源端子名。文字の歴史的な由来を現在の接続機能へ当てはめない。現回路のVEEはU8/U10では浮動基準SW、U9ではGND。各電圧・基準は端子と接続を参照する。
      | 用語13　　　　　　　; GNDP：U10の一次側電源の基準端子。絶縁電源の入力側GND。二次側基準VEE=SWと直接同一の導体ではない。
      | 用語14　　　　　　　; SW：Switching Node（スイッチング点）。主電力段の上下MOSFETとL1がつながる、電圧が高速に切り替わる点。GNDとは別電位。
  GND_Label_010 : ConnectionLabel  Description=|  Label=GND
      | この回路での名前　　; GND
      | 種別　　　　　　　　; ConnectionLabel
      | この回路での役割　　; 電池BT1の負極、太陽電池列の負極、制御・測定・保護回路のGNDを結ぶ共通の帰路。高側駆動の浮動帰路SWとは別のノード。
      | 共通帰路の代表接続　; BT1（充電先の蓄電池／51.2V 100Ah LiFePO4）: -
      |                     ; PV1（直列太陽電池列の負極側パネル／400W panel 1/2）: -
      |                     ; U7（RP2040搭載Pico W／SC0918）: 3(GND), 8(GND), 13(GND), 18(GND), 23(GND), 28(GND), 33(AGND), 38(GND)
      |                     ; U1（外付けADC／MCP3208-CI/SL）: 8(CH7), 9(DGND), 14(AGND)
      |                     ; P_U1（保護MOSFETを制御する保護IC／LTC4364IMS-1#PBF）: GND
      |                     ; Q2（同期整流降圧回路の下側スイッチ／TK9R6E15Q5,S1X）: 3(S)
      |                     ; U9（低側の光ゲートドライバ／ACPL-P346-560E）: 4(VEE)
      |                     ; U10（高側ゲート用の浮動電源を作る絶縁DC/DC／UCC14131QDWNRQ1）: 1(GNDP), 2(GNDP), 5(GNDP), 8(GNDP), 9(GNDP), 10(GNDP), 11(GNDP), 12(GNDP), 13(GNDP), 14(GNDP), 15(GNDP), 16(GNDP), 17(GNDP), 18(GNDP)
      | この場所の直接接続　; C17（ADC電源バイパス／100 nF）: 2
      | 直接接続の範囲　　　; このラベルから実際の線・分岐・明示的な境界端子だけを追った接続。同名ラベルによる離れた場所への接続はこの欄に含めない。
      | 同一ネット全端子　　; BT1: -
      |                     ; C1: 2(n)
      |                     ; C2: 2(n)
      |                     ; C3: 2(n)
      |                     ; C4: 2(n)
      |                     ; C7: 2(n)
      |                     ; C8: 2(n)
      |                     ; C9: 2(n)
      |                     ; C10: 2(n)
      |                     ; C13: 2(n)
      |                     ; C14: 2(n)
      |                     ; C15: 2(n)
      |                     ; C16: 2(n)
      |                     ; C17: 2
      |                     ; C18: 2
      |                     ; C19: 2
      |                     ; C20: 2
      |                     ; C21: 2
      |                     ; C22: 2
      |                     ; C23: 2
      |                     ; C24: 2
      |                     ; C25: 2
      |                     ; C26: 2
      |                     ; C27: 2
      |                     ; C28: 2
      |                     ; C29: 2
      |                     ; C30: 2
      |                     ; C31: 2
      |                     ; C33: 2
      |                     ; C34: 2
      |                     ; C35: 2
      |                     ; C36: 2
      |                     ; C40: 2
      |                     ; C41: 2
      |                     ; C42: 2
      |                     ; C43: 2
      |                     ; C44: 2
      |                     ; C45: 2
      |                     ; C46: 2
      |                     ; C47: 2
      |                     ; C48: 2
      |                     ; D2: 2(A)
      |                     ; PV1: -
      |                     ; P_CHG: N
      |                     ; P_COUT: N
      |                     ; P_CTMR: N
      |                     ; P_D1: A
      |                     ; P_R3: 2
      |                     ; P_R8: 2
      |                     ; P_RSHDN_PD: 2
      |                     ; P_U1: GND
      |                     ; Q2: 3(S)
      |                     ; Q3: 1(S1), 4(S2)
      |                     ; R1: 2(n)
      |                     ; R18: 2
      |                     ; R21: 2
      |                     ; R24: 2
      |                     ; R35: 2
      |                     ; R42: 2
      |                     ; R44: 2
      |                     ; R48: 2
      |                     ; U1: 8(CH7), 9(DGND), 14(AGND)
      |                     ; U2: 2(GND), 3(REF2), 4(RESERVED_GND)
      |                     ; U3: 2(GND), 3(REF2), 4(RESERVED_GND)
      |                     ; U4: 3(GND)
      |                     ; U5: 3(GND)
      |                     ; U6: 3(GND)
      |                     ; U7: 3(GND), 8(GND), 13(GND), 18(GND), 23(GND), 28(GND), 33(AGND), 38(GND)
      |                     ; U9: 4(VEE)
      |                     ; U10: 1(GNDP), 2(GNDP), 5(GNDP), 8(GNDP), 9(GNDP), 10(GNDP), 11(GNDP), 12(GNDP), 13(GNDP), 14(GNDP), 15(GNDP), 16(GNDP), 17(GNDP), 18(GNDP)
      |                     ; U11: 2(GND)
      |                     ; U12: 2(GND)
      | 接続部品数　　　　　; 72部品（部品番号で集計。同一ネット全体）
      | 接続端子数　　　　　; 99端子（423端子の部品対応表で集計。ラベル・境界ポートの重複は含めない）
      | この場所の端子数　　; 1端子／1部品（同名ラベルによる接続を除く）
      | 同階層同名ラベル数　; 75個（このラベル自身を含む）
      | 全階層の接続ラベル　; 87個（実際に同じノードへつながるラベル。名前が違う別名も含む）
      | 接続ルール　　　　　; 同じ階層の同じラベル名を仮想配線として結ぶ。別のSubsystem内とは名前だけでつながらず、明示的なConnection Portと配線をたどる。色は用途の表示であり接続を決めない。
      | 確認の範囲　　　　　; 現在の保存回路の端子・配線から求めた静的接続。抵抗やICの内部を導線として短絡せずに集計した。説明の更新は動作シミュレーション、タイミング、実部品の性能・実機動作を保証するものではない。
      | 記録の基準　　　　　; measurement_label_layout_20261022_r01/after_layout_graph.json。部品対応表は端子名の対応付けにのみ使用。
      | 
      | 【この説明欄の略語・記号】
      | 用語1　　　　　　　 ; DC：Direct Current（直流）。ここでは直流電源または直流成分。DCバイアスはコンデンサに重なる直流電圧を指す。
      | 用語2　　　　　　　 ; DC/DC：DC-to-DC Converter（直流電圧変換器）。直流入力を別の直流電圧へ変換する電源回路。絶縁の有無は個々の部品説明で確認する。
      | 用語3　　　　　　　 ; ADC：Analog-to-Digital Converter（アナログ・デジタル変換器）。測定電圧をデジタル値へ変換する回路。電流や温度も、センサーで電圧へ変換した後に読み取る。
      | 用語4　　　　　　　 ; IC：Integrated Circuit（集積回路）。複数の電子素子と機能を小さな半導体チップに集積した部品。
      | 用語5　　　　　　　 ; CH：Channel（測定チャネル）。CH0〜CH7はADCの入力番号であり、同時測定を意味しない。
      | 用語6　　　　　　　 ; MOSFET：Metal-Oxide-Semiconductor Field-Effect Transistor（金属・酸化膜・半導体構造の電界効果トランジスタ）。ゲートとソースの電圧でドレインとソースの導通を制御する素子。N-MOSはNチャネル型を表す。
      | 用語7　　　　　　　 ; LiFePO4：Lithium Iron Phosphate（リン酸鉄リチウム）。電池の正極材料を示す化学式。英語の頭文字を並べた略語ではない。
      | 用語8　　　　　　　 ; GND：Ground（回路の基準電位・電流帰路）。この図の共通基準。保護接地や大地への接続を意味するとは限らない。
      | 用語9　　　　　　　 ; AGND：Analog Ground（アナログ回路の基準端子）。アナログ部分の電流帰路。現図では共通GNDへ接続されるが、実装時の電流経路への配慮は別途必要。
      | 用語10　　　　　　　; DGND：Digital Ground（デジタル回路の基準端子）。デジタル部分の電流帰路。現図では共通GNDへ接続される。
      | 用語11　　　　　　　; VREF/REF：基準電圧を表す端子名。REFはReference（基準）の意味。ADCの変換尺度や電流アンプの出力基準に使う。REF1/REF2の接続電位は個別に確認する。
      | 用語12　　　　　　　; VCC/VDD/VEE/VS：ICの電源端子名。文字の歴史的な由来を現在の接続機能へ当てはめない。現回路のVEEはU8/U10では浮動基準SW、U9ではGND。各電圧・基準は端子と接続を参照する。
      | 用語13　　　　　　　; GNDP：U10の一次側電源の基準端子。絶縁電源の入力側GND。二次側基準VEE=SWと直接同一の導体ではない。
      | 用語14　　　　　　　; SW：Switching Node（スイッチング点）。主電力段の上下MOSFETとL1がつながる、電圧が高速に切り替わる点。GNDとは別電位。
  GND_Label_011 : ConnectionLabel  Description=|  Label=GND
      | この回路での名前　　; GND
      | 種別　　　　　　　　; ConnectionLabel
      | この回路での役割　　; 電池BT1の負極、太陽電池列の負極、制御・測定・保護回路のGNDを結ぶ共通の帰路。高側駆動の浮動帰路SWとは別のノード。
      | 共通帰路の代表接続　; BT1（充電先の蓄電池／51.2V 100Ah LiFePO4）: -
      |                     ; PV1（直列太陽電池列の負極側パネル／400W panel 1/2）: -
      |                     ; U7（RP2040搭載Pico W／SC0918）: 3(GND), 8(GND), 13(GND), 18(GND), 23(GND), 28(GND), 33(AGND), 38(GND)
      |                     ; U1（外付けADC／MCP3208-CI/SL）: 8(CH7), 9(DGND), 14(AGND)
      |                     ; P_U1（保護MOSFETを制御する保護IC／LTC4364IMS-1#PBF）: GND
      |                     ; Q2（同期整流降圧回路の下側スイッチ／TK9R6E15Q5,S1X）: 3(S)
      |                     ; U9（低側の光ゲートドライバ／ACPL-P346-560E）: 4(VEE)
      |                     ; U10（高側ゲート用の浮動電源を作る絶縁DC/DC／UCC14131QDWNRQ1）: 1(GNDP), 2(GNDP), 5(GNDP), 8(GNDP), 9(GNDP), 10(GNDP), 11(GNDP), 12(GNDP), 13(GNDP), 14(GNDP), 15(GNDP), 16(GNDP), 17(GNDP), 18(GNDP)
      | この場所の直接接続　; C18（3V3測定群の局所バルク／2.2 uF）: 2
      | 直接接続の範囲　　　; このラベルから実際の線・分岐・明示的な境界端子だけを追った接続。同名ラベルによる離れた場所への接続はこの欄に含めない。
      | 同一ネット全端子　　; BT1: -
      |                     ; C1: 2(n)
      |                     ; C2: 2(n)
      |                     ; C3: 2(n)
      |                     ; C4: 2(n)
      |                     ; C7: 2(n)
      |                     ; C8: 2(n)
      |                     ; C9: 2(n)
      |                     ; C10: 2(n)
      |                     ; C13: 2(n)
      |                     ; C14: 2(n)
      |                     ; C15: 2(n)
      |                     ; C16: 2(n)
      |                     ; C17: 2
      |                     ; C18: 2
      |                     ; C19: 2
      |                     ; C20: 2
      |                     ; C21: 2
      |                     ; C22: 2
      |                     ; C23: 2
      |                     ; C24: 2
      |                     ; C25: 2
      |                     ; C26: 2
      |                     ; C27: 2
      |                     ; C28: 2
      |                     ; C29: 2
      |                     ; C30: 2
      |                     ; C31: 2
      |                     ; C33: 2
      |                     ; C34: 2
      |                     ; C35: 2
      |                     ; C36: 2
      |                     ; C40: 2
      |                     ; C41: 2
      |                     ; C42: 2
      |                     ; C43: 2
      |                     ; C44: 2
      |                     ; C45: 2
      |                     ; C46: 2
      |                     ; C47: 2
      |                     ; C48: 2
      |                     ; D2: 2(A)
      |                     ; PV1: -
      |                     ; P_CHG: N
      |                     ; P_COUT: N
      |                     ; P_CTMR: N
      |                     ; P_D1: A
      |                     ; P_R3: 2
      |                     ; P_R8: 2
      |                     ; P_RSHDN_PD: 2
      |                     ; P_U1: GND
      |                     ; Q2: 3(S)
      |                     ; Q3: 1(S1), 4(S2)
      |                     ; R1: 2(n)
      |                     ; R18: 2
      |                     ; R21: 2
      |                     ; R24: 2
      |                     ; R35: 2
      |                     ; R42: 2
      |                     ; R44: 2
      |                     ; R48: 2
      |                     ; U1: 8(CH7), 9(DGND), 14(AGND)
      |                     ; U2: 2(GND), 3(REF2), 4(RESERVED_GND)
      |                     ; U3: 2(GND), 3(REF2), 4(RESERVED_GND)
      |                     ; U4: 3(GND)
      |                     ; U5: 3(GND)
      |                     ; U6: 3(GND)
      |                     ; U7: 3(GND), 8(GND), 13(GND), 18(GND), 23(GND), 28(GND), 33(AGND), 38(GND)
      |                     ; U9: 4(VEE)
      |                     ; U10: 1(GNDP), 2(GNDP), 5(GNDP), 8(GNDP), 9(GNDP), 10(GNDP), 11(GNDP), 12(GNDP), 13(GNDP), 14(GNDP), 15(GNDP), 16(GNDP), 17(GNDP), 18(GNDP)
      |                     ; U11: 2(GND)
      |                     ; U12: 2(GND)
      | 接続部品数　　　　　; 72部品（部品番号で集計。同一ネット全体）
      | 接続端子数　　　　　; 99端子（423端子の部品対応表で集計。ラベル・境界ポートの重複は含めない）
      | この場所の端子数　　; 1端子／1部品（同名ラベルによる接続を除く）
      | 同階層同名ラベル数　; 75個（このラベル自身を含む）
      | 全階層の接続ラベル　; 87個（実際に同じノードへつながるラベル。名前が違う別名も含む）
      | 接続ルール　　　　　; 同じ階層の同じラベル名を仮想配線として結ぶ。別のSubsystem内とは名前だけでつながらず、明示的なConnection Portと配線をたどる。色は用途の表示であり接続を決めない。
      | 確認の範囲　　　　　; 現在の保存回路の端子・配線から求めた静的接続。抵抗やICの内部を導線として短絡せずに集計した。説明の更新は動作シミュレーション、タイミング、実部品の性能・実機動作を保証するものではない。
      | 記録の基準　　　　　; measurement_label_layout_20261022_r01/after_layout_graph.json。部品対応表は端子名の対応付けにのみ使用。
      | 
      | 【この説明欄の略語・記号】
      | 用語1　　　　　　　 ; DC：Direct Current（直流）。ここでは直流電源または直流成分。DCバイアスはコンデンサに重なる直流電圧を指す。
      | 用語2　　　　　　　 ; DC/DC：DC-to-DC Converter（直流電圧変換器）。直流入力を別の直流電圧へ変換する電源回路。絶縁の有無は個々の部品説明で確認する。
      | 用語3　　　　　　　 ; ADC：Analog-to-Digital Converter（アナログ・デジタル変換器）。測定電圧をデジタル値へ変換する回路。電流や温度も、センサーで電圧へ変換した後に読み取る。
      | 用語4　　　　　　　 ; IC：Integrated Circuit（集積回路）。複数の電子素子と機能を小さな半導体チップに集積した部品。
      | 用語5　　　　　　　 ; CH：Channel（測定チャネル）。CH0〜CH7はADCの入力番号であり、同時測定を意味しない。
      | 用語6　　　　　　　 ; MOSFET：Metal-Oxide-Semiconductor Field-Effect Transistor（金属・酸化膜・半導体構造の電界効果トランジスタ）。ゲートとソースの電圧でドレインとソースの導通を制御する素子。N-MOSはNチャネル型を表す。
      | 用語7　　　　　　　 ; LiFePO4：Lithium Iron Phosphate（リン酸鉄リチウム）。電池の正極材料を示す化学式。英語の頭文字を並べた略語ではない。
      | 用語8　　　　　　　 ; GND：Ground（回路の基準電位・電流帰路）。この図の共通基準。保護接地や大地への接続を意味するとは限らない。
      | 用語9　　　　　　　 ; AGND：Analog Ground（アナログ回路の基準端子）。アナログ部分の電流帰路。現図では共通GNDへ接続されるが、実装時の電流経路への配慮は別途必要。
      | 用語10　　　　　　　; DGND：Digital Ground（デジタル回路の基準端子）。デジタル部分の電流帰路。現図では共通GNDへ接続される。
      | 用語11　　　　　　　; VREF/REF：基準電圧を表す端子名。REFはReference（基準）の意味。ADCの変換尺度や電流アンプの出力基準に使う。REF1/REF2の接続電位は個別に確認する。
      | 用語12　　　　　　　; VCC/VDD/VEE/VS：ICの電源端子名。文字の歴史的な由来を現在の接続機能へ当てはめない。現回路のVEEはU8/U10では浮動基準SW、U9ではGND。各電圧・基準は端子と接続を参照する。
      | 用語13　　　　　　　; GNDP：U10の一次側電源の基準端子。絶縁電源の入力側GND。二次側基準VEE=SWと直接同一の導体ではない。
      | 用語14　　　　　　　; SW：Switching Node（スイッチング点）。主電力段の上下MOSFETとL1がつながる、電圧が高速に切り替わる点。GNDとは別電位。
  GND_Label_012 : ConnectionLabel  Description=|  Label=GND
      | この回路での名前　　; GND
      | 種別　　　　　　　　; ConnectionLabel
      | この回路での役割　　; 電池BT1の負極、太陽電池列の負極、制御・測定・保護回路のGNDを結ぶ共通の帰路。高側駆動の浮動帰路SWとは別のノード。
      | 共通帰路の代表接続　; BT1（充電先の蓄電池／51.2V 100Ah LiFePO4）: -
      |                     ; PV1（直列太陽電池列の負極側パネル／400W panel 1/2）: -
      |                     ; U7（RP2040搭載Pico W／SC0918）: 3(GND), 8(GND), 13(GND), 18(GND), 23(GND), 28(GND), 33(AGND), 38(GND)
      |                     ; U1（外付けADC／MCP3208-CI/SL）: 8(CH7), 9(DGND), 14(AGND)
      |                     ; P_U1（保護MOSFETを制御する保護IC／LTC4364IMS-1#PBF）: GND
      |                     ; Q2（同期整流降圧回路の下側スイッチ／TK9R6E15Q5,S1X）: 3(S)
      |                     ; U9（低側の光ゲートドライバ／ACPL-P346-560E）: 4(VEE)
      |                     ; U10（高側ゲート用の浮動電源を作る絶縁DC/DC／UCC14131QDWNRQ1）: 1(GNDP), 2(GNDP), 5(GNDP), 8(GNDP), 9(GNDP), 10(GNDP), 11(GNDP), 12(GNDP), 13(GNDP), 14(GNDP), 15(GNDP), 16(GNDP), 17(GNDP), 18(GNDP)
      | この場所の直接接続　; C19（PV入力電圧の分圧後の信号を平滑するコンデンサ／100 nF）: 2
      | 直接接続の範囲　　　; このラベルから実際の線・分岐・明示的な境界端子だけを追った接続。同名ラベルによる離れた場所への接続はこの欄に含めない。
      | 同一ネット全端子　　; BT1: -
      |                     ; C1: 2(n)
      |                     ; C2: 2(n)
      |                     ; C3: 2(n)
      |                     ; C4: 2(n)
      |                     ; C7: 2(n)
      |                     ; C8: 2(n)
      |                     ; C9: 2(n)
      |                     ; C10: 2(n)
      |                     ; C13: 2(n)
      |                     ; C14: 2(n)
      |                     ; C15: 2(n)
      |                     ; C16: 2(n)
      |                     ; C17: 2
      |                     ; C18: 2
      |                     ; C19: 2
      |                     ; C20: 2
      |                     ; C21: 2
      |                     ; C22: 2
      |                     ; C23: 2
      |                     ; C24: 2
      |                     ; C25: 2
      |                     ; C26: 2
      |                     ; C27: 2
      |                     ; C28: 2
      |                     ; C29: 2
      |                     ; C30: 2
      |                     ; C31: 2
      |                     ; C33: 2
      |                     ; C34: 2
      |                     ; C35: 2
      |                     ; C36: 2
      |                     ; C40: 2
      |                     ; C41: 2
      |                     ; C42: 2
      |                     ; C43: 2
      |                     ; C44: 2
      |                     ; C45: 2
      |                     ; C46: 2
      |                     ; C47: 2
      |                     ; C48: 2
      |                     ; D2: 2(A)
      |                     ; PV1: -
      |                     ; P_CHG: N
      |                     ; P_COUT: N
      |                     ; P_CTMR: N
      |                     ; P_D1: A
      |                     ; P_R3: 2
      |                     ; P_R8: 2
      |                     ; P_RSHDN_PD: 2
      |                     ; P_U1: GND
      |                     ; Q2: 3(S)
      |                     ; Q3: 1(S1), 4(S2)
      |                     ; R1: 2(n)
      |                     ; R18: 2
      |                     ; R21: 2
      |                     ; R24: 2
      |                     ; R35: 2
      |                     ; R42: 2
      |                     ; R44: 2
      |                     ; R48: 2
      |                     ; U1: 8(CH7), 9(DGND), 14(AGND)
      |                     ; U2: 2(GND), 3(REF2), 4(RESERVED_GND)
      |                     ; U3: 2(GND), 3(REF2), 4(RESERVED_GND)
      |                     ; U4: 3(GND)
      |                     ; U5: 3(GND)
      |                     ; U6: 3(GND)
      |                     ; U7: 3(GND), 8(GND), 13(GND), 18(GND), 23(GND), 28(GND), 33(AGND), 38(GND)
      |                     ; U9: 4(VEE)
      |                     ; U10: 1(GNDP), 2(GNDP), 5(GNDP), 8(GNDP), 9(GNDP), 10(GNDP), 11(GNDP), 12(GNDP), 13(GNDP), 14(GNDP), 15(GNDP), 16(GNDP), 17(GNDP), 18(GNDP)
      |                     ; U11: 2(GND)
      |                     ; U12: 2(GND)
      | 接続部品数　　　　　; 72部品（部品番号で集計。同一ネット全体）
      | 接続端子数　　　　　; 99端子（423端子の部品対応表で集計。ラベル・境界ポートの重複は含めない）
      | この場所の端子数　　; 1端子／1部品（同名ラベルによる接続を除く）
      | 同階層同名ラベル数　; 75個（このラベル自身を含む）
      | 全階層の接続ラベル　; 87個（実際に同じノードへつながるラベル。名前が違う別名も含む）
      | 接続ルール　　　　　; 同じ階層の同じラベル名を仮想配線として結ぶ。別のSubsystem内とは名前だけでつながらず、明示的なConnection Portと配線をたどる。色は用途の表示であり接続を決めない。
      | 確認の範囲　　　　　; 現在の保存回路の端子・配線から求めた静的接続。抵抗やICの内部を導線として短絡せずに集計した。説明の更新は動作シミュレーション、タイミング、実部品の性能・実機動作を保証するものではない。
      | 記録の基準　　　　　; measurement_label_layout_20261022_r01/after_layout_graph.json。部品対応表は端子名の対応付けにのみ使用。
      | 
      | 【この説明欄の略語・記号】
      | 用語1　　　　　　　 ; DC：Direct Current（直流）。ここでは直流電源または直流成分。DCバイアスはコンデンサに重なる直流電圧を指す。
      | 用語2　　　　　　　 ; DC/DC：DC-to-DC Converter（直流電圧変換器）。直流入力を別の直流電圧へ変換する電源回路。絶縁の有無は個々の部品説明で確認する。
      | 用語3　　　　　　　 ; ADC：Analog-to-Digital Converter（アナログ・デジタル変換器）。測定電圧をデジタル値へ変換する回路。電流や温度も、センサーで電圧へ変換した後に読み取る。
      | 用語4　　　　　　　 ; IC：Integrated Circuit（集積回路）。複数の電子素子と機能を小さな半導体チップに集積した部品。
      | 用語5　　　　　　　 ; CH：Channel（測定チャネル）。CH0〜CH7はADCの入力番号であり、同時測定を意味しない。
      | 用語6　　　　　　　 ; MOSFET：Metal-Oxide-Semiconductor Field-Effect Transistor（金属・酸化膜・半導体構造の電界効果トランジスタ）。ゲートとソースの電圧でドレインとソースの導通を制御する素子。N-MOSはNチャネル型を表す。
      | 用語7　　　　　　　 ; LiFePO4：Lithium Iron Phosphate（リン酸鉄リチウム）。電池の正極材料を示す化学式。英語の頭文字を並べた略語ではない。
      | 用語8　　　　　　　 ; PV：Photovoltaic（太陽光発電）。光を電気へ変える発電方式。PVを含むネット名は太陽電池側の測定・電力経路を表す。
      | 用語9　　　　　　　 ; GND：Ground（回路の基準電位・電流帰路）。この図の共通基準。保護接地や大地への接続を意味するとは限らない。
      | 用語10　　　　　　　; AGND：Analog Ground（アナログ回路の基準端子）。アナログ部分の電流帰路。現図では共通GNDへ接続されるが、実装時の電流経路への配慮は別途必要。
      | 用語11　　　　　　　; DGND：Digital Ground（デジタル回路の基準端子）。デジタル部分の電流帰路。現図では共通GNDへ接続される。
      | 用語12　　　　　　　; VREF/REF：基準電圧を表す端子名。REFはReference（基準）の意味。ADCの変換尺度や電流アンプの出力基準に使う。REF1/REF2の接続電位は個別に確認する。
      | 用語13　　　　　　　; VCC/VDD/VEE/VS：ICの電源端子名。文字の歴史的な由来を現在の接続機能へ当てはめない。現回路のVEEはU8/U10では浮動基準SW、U9ではGND。各電圧・基準は端子と接続を参照する。
      | 用語14　　　　　　　; GNDP：U10の一次側電源の基準端子。絶縁電源の入力側GND。二次側基準VEE=SWと直接同一の導体ではない。
      | 用語15　　　　　　　; SW：Switching Node（スイッチング点）。主電力段の上下MOSFETとL1がつながる、電圧が高速に切り替わる点。GNDとは別電位。
  GND_Label_013 : ConnectionLabel  Description=|  Label=GND
      | この回路での名前　　; GND
      | 種別　　　　　　　　; ConnectionLabel
      | この回路での役割　　; 電池BT1の負極、太陽電池列の負極、制御・測定・保護回路のGNDを結ぶ共通の帰路。高側駆動の浮動帰路SWとは別のノード。
      | 共通帰路の代表接続　; BT1（充電先の蓄電池／51.2V 100Ah LiFePO4）: -
      |                     ; PV1（直列太陽電池列の負極側パネル／400W panel 1/2）: -
      |                     ; U7（RP2040搭載Pico W／SC0918）: 3(GND), 8(GND), 13(GND), 18(GND), 23(GND), 28(GND), 33(AGND), 38(GND)
      |                     ; U1（外付けADC／MCP3208-CI/SL）: 8(CH7), 9(DGND), 14(AGND)
      |                     ; P_U1（保護MOSFETを制御する保護IC／LTC4364IMS-1#PBF）: GND
      |                     ; Q2（同期整流降圧回路の下側スイッチ／TK9R6E15Q5,S1X）: 3(S)
      |                     ; U9（低側の光ゲートドライバ／ACPL-P346-560E）: 4(VEE)
      |                     ; U10（高側ゲート用の浮動電源を作る絶縁DC/DC／UCC14131QDWNRQ1）: 1(GNDP), 2(GNDP), 5(GNDP), 8(GNDP), 9(GNDP), 10(GNDP), 11(GNDP), 12(GNDP), 13(GNDP), 14(GNDP), 15(GNDP), 16(GNDP), 17(GNDP), 18(GNDP)
      | この場所の直接接続　; C2（入力バルク／470 uF）: 2(n)
      | 直接接続の範囲　　　; このラベルから実際の線・分岐・明示的な境界端子だけを追った接続。同名ラベルによる離れた場所への接続はこの欄に含めない。
      | 同一ネット全端子　　; BT1: -
      |                     ; C1: 2(n)
      |                     ; C2: 2(n)
      |                     ; C3: 2(n)
      |                     ; C4: 2(n)
      |                     ; C7: 2(n)
      |                     ; C8: 2(n)
      |                     ; C9: 2(n)
      |                     ; C10: 2(n)
      |                     ; C13: 2(n)
      |                     ; C14: 2(n)
      |                     ; C15: 2(n)
      |                     ; C16: 2(n)
      |                     ; C17: 2
      |                     ; C18: 2
      |                     ; C19: 2
      |                     ; C20: 2
      |                     ; C21: 2
      |                     ; C22: 2
      |                     ; C23: 2
      |                     ; C24: 2
      |                     ; C25: 2
      |                     ; C26: 2
      |                     ; C27: 2
      |                     ; C28: 2
      |                     ; C29: 2
      |                     ; C30: 2
      |                     ; C31: 2
      |                     ; C33: 2
      |                     ; C34: 2
      |                     ; C35: 2
      |                     ; C36: 2
      |                     ; C40: 2
      |                     ; C41: 2
      |                     ; C42: 2
      |                     ; C43: 2
      |                     ; C44: 2
      |                     ; C45: 2
      |                     ; C46: 2
      |                     ; C47: 2
      |                     ; C48: 2
      |                     ; D2: 2(A)
      |                     ; PV1: -
      |                     ; P_CHG: N
      |                     ; P_COUT: N
      |                     ; P_CTMR: N
      |                     ; P_D1: A
      |                     ; P_R3: 2
      |                     ; P_R8: 2
      |                     ; P_RSHDN_PD: 2
      |                     ; P_U1: GND
      |                     ; Q2: 3(S)
      |                     ; Q3: 1(S1), 4(S2)
      |                     ; R1: 2(n)
      |                     ; R18: 2
      |                     ; R21: 2
      |                     ; R24: 2
      |                     ; R35: 2
      |                     ; R42: 2
      |                     ; R44: 2
      |                     ; R48: 2
      |                     ; U1: 8(CH7), 9(DGND), 14(AGND)
      |                     ; U2: 2(GND), 3(REF2), 4(RESERVED_GND)
      |                     ; U3: 2(GND), 3(REF2), 4(RESERVED_GND)
      |                     ; U4: 3(GND)
      |                     ; U5: 3(GND)
      |                     ; U6: 3(GND)
      |                     ; U7: 3(GND), 8(GND), 13(GND), 18(GND), 23(GND), 28(GND), 33(AGND), 38(GND)
      |                     ; U9: 4(VEE)
      |                     ; U10: 1(GNDP), 2(GNDP), 5(GNDP), 8(GNDP), 9(GNDP), 10(GNDP), 11(GNDP), 12(GNDP), 13(GNDP), 14(GNDP), 15(GNDP), 16(GNDP), 17(GNDP), 18(GNDP)
      |                     ; U11: 2(GND)
      |                     ; U12: 2(GND)
      | 接続部品数　　　　　; 72部品（部品番号で集計。同一ネット全体）
      | 接続端子数　　　　　; 99端子（423端子の部品対応表で集計。ラベル・境界ポートの重複は含めない）
      | この場所の端子数　　; 1端子／1部品（同名ラベルによる接続を除く）
      | 同階層同名ラベル数　; 75個（このラベル自身を含む）
      | 全階層の接続ラベル　; 87個（実際に同じノードへつながるラベル。名前が違う別名も含む）
      | 接続ルール　　　　　; 同じ階層の同じラベル名を仮想配線として結ぶ。別のSubsystem内とは名前だけでつながらず、明示的なConnection Portと配線をたどる。色は用途の表示であり接続を決めない。
      | 確認の範囲　　　　　; 現在の保存回路の端子・配線から求めた静的接続。抵抗やICの内部を導線として短絡せずに集計した。説明の更新は動作シミュレーション、タイミング、実部品の性能・実機動作を保証するものではない。
      | 記録の基準　　　　　; measurement_label_layout_20261022_r01/after_layout_graph.json。部品対応表は端子名の対応付けにのみ使用。
      | 
      | 【この説明欄の略語・記号】
      | 用語1　　　　　　　 ; DC：Direct Current（直流）。ここでは直流電源または直流成分。DCバイアスはコンデンサに重なる直流電圧を指す。
      | 用語2　　　　　　　 ; DC/DC：DC-to-DC Converter（直流電圧変換器）。直流入力を別の直流電圧へ変換する電源回路。絶縁の有無は個々の部品説明で確認する。
      | 用語3　　　　　　　 ; ADC：Analog-to-Digital Converter（アナログ・デジタル変換器）。測定電圧をデジタル値へ変換する回路。電流や温度も、センサーで電圧へ変換した後に読み取る。
      | 用語4　　　　　　　 ; IC：Integrated Circuit（集積回路）。複数の電子素子と機能を小さな半導体チップに集積した部品。
      | 用語5　　　　　　　 ; CH：Channel（測定チャネル）。CH0〜CH7はADCの入力番号であり、同時測定を意味しない。
      | 用語6　　　　　　　 ; MOSFET：Metal-Oxide-Semiconductor Field-Effect Transistor（金属・酸化膜・半導体構造の電界効果トランジスタ）。ゲートとソースの電圧でドレインとソースの導通を制御する素子。N-MOSはNチャネル型を表す。
      | 用語7　　　　　　　 ; LiFePO4：Lithium Iron Phosphate（リン酸鉄リチウム）。電池の正極材料を示す化学式。英語の頭文字を並べた略語ではない。
      | 用語8　　　　　　　 ; GND：Ground（回路の基準電位・電流帰路）。この図の共通基準。保護接地や大地への接続を意味するとは限らない。
      | 用語9　　　　　　　 ; AGND：Analog Ground（アナログ回路の基準端子）。アナログ部分の電流帰路。現図では共通GNDへ接続されるが、実装時の電流経路への配慮は別途必要。
      | 用語10　　　　　　　; DGND：Digital Ground（デジタル回路の基準端子）。デジタル部分の電流帰路。現図では共通GNDへ接続される。
      | 用語11　　　　　　　; VREF/REF：基準電圧を表す端子名。REFはReference（基準）の意味。ADCの変換尺度や電流アンプの出力基準に使う。REF1/REF2の接続電位は個別に確認する。
      | 用語12　　　　　　　; VCC/VDD/VEE/VS：ICの電源端子名。文字の歴史的な由来を現在の接続機能へ当てはめない。現回路のVEEはU8/U10では浮動基準SW、U9ではGND。各電圧・基準は端子と接続を参照する。
      | 用語13　　　　　　　; GNDP：U10の一次側電源の基準端子。絶縁電源の入力側GND。二次側基準VEE=SWと直接同一の導体ではない。
      | 用語14　　　　　　　; SW：Switching Node（スイッチング点）。主電力段の上下MOSFETとL1がつながる、電圧が高速に切り替わる点。GNDとは別電位。
  GND_Label_014 : ConnectionLabel  Description=|  Label=GND
      | この回路での名前　　; GND
      | 種別　　　　　　　　; ConnectionLabel
      | この回路での役割　　; 電池BT1の負極、太陽電池列の負極、制御・測定・保護回路のGNDを結ぶ共通の帰路。高側駆動の浮動帰路SWとは別のノード。
      | 共通帰路の代表接続　; BT1（充電先の蓄電池／51.2V 100Ah LiFePO4）: -
      |                     ; PV1（直列太陽電池列の負極側パネル／400W panel 1/2）: -
      |                     ; U7（RP2040搭載Pico W／SC0918）: 3(GND), 8(GND), 13(GND), 18(GND), 23(GND), 28(GND), 33(AGND), 38(GND)
      |                     ; U1（外付けADC／MCP3208-CI/SL）: 8(CH7), 9(DGND), 14(AGND)
      |                     ; P_U1（保護MOSFETを制御する保護IC／LTC4364IMS-1#PBF）: GND
      |                     ; Q2（同期整流降圧回路の下側スイッチ／TK9R6E15Q5,S1X）: 3(S)
      |                     ; U9（低側の光ゲートドライバ／ACPL-P346-560E）: 4(VEE)
      |                     ; U10（高側ゲート用の浮動電源を作る絶縁DC/DC／UCC14131QDWNRQ1）: 1(GNDP), 2(GNDP), 5(GNDP), 8(GNDP), 9(GNDP), 10(GNDP), 11(GNDP), 12(GNDP), 13(GNDP), 14(GNDP), 15(GNDP), 16(GNDP), 17(GNDP), 18(GNDP)
      | この場所の直接接続　; C20（出力電圧の分圧後の信号を平滑するコンデンサ／100 nF）: 2
      | 直接接続の範囲　　　; このラベルから実際の線・分岐・明示的な境界端子だけを追った接続。同名ラベルによる離れた場所への接続はこの欄に含めない。
      | 同一ネット全端子　　; BT1: -
      |                     ; C1: 2(n)
      |                     ; C2: 2(n)
      |                     ; C3: 2(n)
      |                     ; C4: 2(n)
      |                     ; C7: 2(n)
      |                     ; C8: 2(n)
      |                     ; C9: 2(n)
      |                     ; C10: 2(n)
      |                     ; C13: 2(n)
      |                     ; C14: 2(n)
      |                     ; C15: 2(n)
      |                     ; C16: 2(n)
      |                     ; C17: 2
      |                     ; C18: 2
      |                     ; C19: 2
      |                     ; C20: 2
      |                     ; C21: 2
      |                     ; C22: 2
      |                     ; C23: 2
      |                     ; C24: 2
      |                     ; C25: 2
      |                     ; C26: 2
      |                     ; C27: 2
      |                     ; C28: 2
      |                     ; C29: 2
      |                     ; C30: 2
      |                     ; C31: 2
      |                     ; C33: 2
      |                     ; C34: 2
      |                     ; C35: 2
      |                     ; C36: 2
      |                     ; C40: 2
      |                     ; C41: 2
      |                     ; C42: 2
      |                     ; C43: 2
      |                     ; C44: 2
      |                     ; C45: 2
      |                     ; C46: 2
      |                     ; C47: 2
      |                     ; C48: 2
      |                     ; D2: 2(A)
      |                     ; PV1: -
      |                     ; P_CHG: N
      |                     ; P_COUT: N
      |                     ; P_CTMR: N
      |                     ; P_D1: A
      |                     ; P_R3: 2
      |                     ; P_R8: 2
      |                     ; P_RSHDN_PD: 2
      |                     ; P_U1: GND
      |                     ; Q2: 3(S)
      |                     ; Q3: 1(S1), 4(S2)
      |                     ; R1: 2(n)
      |                     ; R18: 2
      |                     ; R21: 2
      |                     ; R24: 2
      |                     ; R35: 2
      |                     ; R42: 2
      |                     ; R44: 2
      |                     ; R48: 2
      |                     ; U1: 8(CH7), 9(DGND), 14(AGND)
      |                     ; U2: 2(GND), 3(REF2), 4(RESERVED_GND)
      |                     ; U3: 2(GND), 3(REF2), 4(RESERVED_GND)
      |                     ; U4: 3(GND)
      |                     ; U5: 3(GND)
      |                     ; U6: 3(GND)
      |                     ; U7: 3(GND), 8(GND), 13(GND), 18(GND), 23(GND), 28(GND), 33(AGND), 38(GND)
      |                     ; U9: 4(VEE)
      |                     ; U10: 1(GNDP), 2(GNDP), 5(GNDP), 8(GNDP), 9(GNDP), 10(GNDP), 11(GNDP), 12(GNDP), 13(GNDP), 14(GNDP), 15(GNDP), 16(GNDP), 17(GNDP), 18(GNDP)
      |                     ; U11: 2(GND)
      |                     ; U12: 2(GND)
      | 接続部品数　　　　　; 72部品（部品番号で集計。同一ネット全体）
      | 接続端子数　　　　　; 99端子（423端子の部品対応表で集計。ラベル・境界ポートの重複は含めない）
      | この場所の端子数　　; 1端子／1部品（同名ラベルによる接続を除く）
      | 同階層同名ラベル数　; 75個（このラベル自身を含む）
      | 全階層の接続ラベル　; 87個（実際に同じノードへつながるラベル。名前が違う別名も含む）
      | 接続ルール　　　　　; 同じ階層の同じラベル名を仮想配線として結ぶ。別のSubsystem内とは名前だけでつながらず、明示的なConnection Portと配線をたどる。色は用途の表示であり接続を決めない。
      | 確認の範囲　　　　　; 現在の保存回路の端子・配線から求めた静的接続。抵抗やICの内部を導線として短絡せずに集計した。説明の更新は動作シミュレーション、タイミング、実部品の性能・実機動作を保証するものではない。
      | 記録の基準　　　　　; measurement_label_layout_20261022_r01/after_layout_graph.json。部品対応表は端子名の対応付けにのみ使用。
      | 
      | 【この説明欄の略語・記号】
      | 用語1　　　　　　　 ; DC：Direct Current（直流）。ここでは直流電源または直流成分。DCバイアスはコンデンサに重なる直流電圧を指す。
      | 用語2　　　　　　　 ; DC/DC：DC-to-DC Converter（直流電圧変換器）。直流入力を別の直流電圧へ変換する電源回路。絶縁の有無は個々の部品説明で確認する。
      | 用語3　　　　　　　 ; ADC：Analog-to-Digital Converter（アナログ・デジタル変換器）。測定電圧をデジタル値へ変換する回路。電流や温度も、センサーで電圧へ変換した後に読み取る。
      | 用語4　　　　　　　 ; IC：Integrated Circuit（集積回路）。複数の電子素子と機能を小さな半導体チップに集積した部品。
      | 用語5　　　　　　　 ; CH：Channel（測定チャネル）。CH0〜CH7はADCの入力番号であり、同時測定を意味しない。
      | 用語6　　　　　　　 ; MOSFET：Metal-Oxide-Semiconductor Field-Effect Transistor（金属・酸化膜・半導体構造の電界効果トランジスタ）。ゲートとソースの電圧でドレインとソースの導通を制御する素子。N-MOSはNチャネル型を表す。
      | 用語7　　　　　　　 ; LiFePO4：Lithium Iron Phosphate（リン酸鉄リチウム）。電池の正極材料を示す化学式。英語の頭文字を並べた略語ではない。
      | 用語8　　　　　　　 ; GND：Ground（回路の基準電位・電流帰路）。この図の共通基準。保護接地や大地への接続を意味するとは限らない。
      | 用語9　　　　　　　 ; AGND：Analog Ground（アナログ回路の基準端子）。アナログ部分の電流帰路。現図では共通GNDへ接続されるが、実装時の電流経路への配慮は別途必要。
      | 用語10　　　　　　　; DGND：Digital Ground（デジタル回路の基準端子）。デジタル部分の電流帰路。現図では共通GNDへ接続される。
      | 用語11　　　　　　　; VREF/REF：基準電圧を表す端子名。REFはReference（基準）の意味。ADCの変換尺度や電流アンプの出力基準に使う。REF1/REF2の接続電位は個別に確認する。
      | 用語12　　　　　　　; VCC/VDD/VEE/VS：ICの電源端子名。文字の歴史的な由来を現在の接続機能へ当てはめない。現回路のVEEはU8/U10では浮動基準SW、U9ではGND。各電圧・基準は端子と接続を参照する。
      | 用語13　　　　　　　; GNDP：U10の一次側電源の基準端子。絶縁電源の入力側GND。二次側基準VEE=SWと直接同一の導体ではない。
      | 用語14　　　　　　　; SW：Switching Node（スイッチング点）。主電力段の上下MOSFETとL1がつながる、電圧が高速に切り替わる点。GNDとは別電位。
  GND_Label_015 : ConnectionLabel  Description=|  Label=GND
      | この回路での名前　　; GND
      | 種別　　　　　　　　; ConnectionLabel
      | この回路での役割　　; 電池BT1の負極、太陽電池列の負極、制御・測定・保護回路のGNDを結ぶ共通の帰路。高側駆動の浮動帰路SWとは別のノード。
      | 共通帰路の代表接続　; BT1（充電先の蓄電池／51.2V 100Ah LiFePO4）: -
      |                     ; PV1（直列太陽電池列の負極側パネル／400W panel 1/2）: -
      |                     ; U7（RP2040搭載Pico W／SC0918）: 3(GND), 8(GND), 13(GND), 18(GND), 23(GND), 28(GND), 33(AGND), 38(GND)
      |                     ; U1（外付けADC／MCP3208-CI/SL）: 8(CH7), 9(DGND), 14(AGND)
      |                     ; P_U1（保護MOSFETを制御する保護IC／LTC4364IMS-1#PBF）: GND
      |                     ; Q2（同期整流降圧回路の下側スイッチ／TK9R6E15Q5,S1X）: 3(S)
      |                     ; U9（低側の光ゲートドライバ／ACPL-P346-560E）: 4(VEE)
      |                     ; U10（高側ゲート用の浮動電源を作る絶縁DC/DC／UCC14131QDWNRQ1）: 1(GNDP), 2(GNDP), 5(GNDP), 8(GNDP), 9(GNDP), 10(GNDP), 11(GNDP), 12(GNDP), 13(GNDP), 14(GNDP), 15(GNDP), 16(GNDP), 17(GNDP), 18(GNDP)
      | この場所の直接接続　; C21（電池側電圧の分圧後の信号を平滑するコンデンサ／100 nF）: 2
      | 直接接続の範囲　　　; このラベルから実際の線・分岐・明示的な境界端子だけを追った接続。同名ラベルによる離れた場所への接続はこの欄に含めない。
      | 同一ネット全端子　　; BT1: -
      |                     ; C1: 2(n)
      |                     ; C2: 2(n)
      |                     ; C3: 2(n)
      |                     ; C4: 2(n)
      |                     ; C7: 2(n)
      |                     ; C8: 2(n)
      |                     ; C9: 2(n)
      |                     ; C10: 2(n)
      |                     ; C13: 2(n)
      |                     ; C14: 2(n)
      |                     ; C15: 2(n)
      |                     ; C16: 2(n)
      |                     ; C17: 2
      |                     ; C18: 2
      |                     ; C19: 2
      |                     ; C20: 2
      |                     ; C21: 2
      |                     ; C22: 2
      |                     ; C23: 2
      |                     ; C24: 2
      |                     ; C25: 2
      |                     ; C26: 2
      |                     ; C27: 2
      |                     ; C28: 2
      |                     ; C29: 2
      |                     ; C30: 2
      |                     ; C31: 2
      |                     ; C33: 2
      |                     ; C34: 2
      |                     ; C35: 2
      |                     ; C36: 2
      |                     ; C40: 2
      |                     ; C41: 2
      |                     ; C42: 2
      |                     ; C43: 2
      |                     ; C44: 2
      |                     ; C45: 2
      |                     ; C46: 2
      |                     ; C47: 2
      |                     ; C48: 2
      |                     ; D2: 2(A)
      |                     ; PV1: -
      |                     ; P_CHG: N
      |                     ; P_COUT: N
      |                     ; P_CTMR: N
      |                     ; P_D1: A
      |                     ; P_R3: 2
      |                     ; P_R8: 2
      |                     ; P_RSHDN_PD: 2
      |                     ; P_U1: GND
      |                     ; Q2: 3(S)
      |                     ; Q3: 1(S1), 4(S2)
      |                     ; R1: 2(n)
      |                     ; R18: 2
      |                     ; R21: 2
      |                     ; R24: 2
      |                     ; R35: 2
      |                     ; R42: 2
      |                     ; R44: 2
      |                     ; R48: 2
      |                     ; U1: 8(CH7), 9(DGND), 14(AGND)
      |                     ; U2: 2(GND), 3(REF2), 4(RESERVED_GND)
      |                     ; U3: 2(GND), 3(REF2), 4(RESERVED_GND)
      |                     ; U4: 3(GND)
      |                     ; U5: 3(GND)
      |                     ; U6: 3(GND)
      |                     ; U7: 3(GND), 8(GND), 13(GND), 18(GND), 23(GND), 28(GND), 33(AGND), 38(GND)
      |                     ; U9: 4(VEE)
      |                     ; U10: 1(GNDP), 2(GNDP), 5(GNDP), 8(GNDP), 9(GNDP), 10(GNDP), 11(GNDP), 12(GNDP), 13(GNDP), 14(GNDP), 15(GNDP), 16(GNDP), 17(GNDP), 18(GNDP)
      |                     ; U11: 2(GND)
      |                     ; U12: 2(GND)
      | 接続部品数　　　　　; 72部品（部品番号で集計。同一ネット全体）
      | 接続端子数　　　　　; 99端子（423端子の部品対応表で集計。ラベル・境界ポートの重複は含めない）
      | この場所の端子数　　; 1端子／1部品（同名ラベルによる接続を除く）
      | 同階層同名ラベル数　; 75個（このラベル自身を含む）
      | 全階層の接続ラベル　; 87個（実際に同じノードへつながるラベル。名前が違う別名も含む）
      | 接続ルール　　　　　; 同じ階層の同じラベル名を仮想配線として結ぶ。別のSubsystem内とは名前だけでつながらず、明示的なConnection Portと配線をたどる。色は用途の表示であり接続を決めない。
      | 確認の範囲　　　　　; 現在の保存回路の端子・配線から求めた静的接続。抵抗やICの内部を導線として短絡せずに集計した。説明の更新は動作シミュレーション、タイミング、実部品の性能・実機動作を保証するものではない。
      | 記録の基準　　　　　; measurement_label_layout_20261022_r01/after_layout_graph.json。部品対応表は端子名の対応付けにのみ使用。
      | 
      | 【この説明欄の略語・記号】
      | 用語1　　　　　　　 ; DC：Direct Current（直流）。ここでは直流電源または直流成分。DCバイアスはコンデンサに重なる直流電圧を指す。
      | 用語2　　　　　　　 ; DC/DC：DC-to-DC Converter（直流電圧変換器）。直流入力を別の直流電圧へ変換する電源回路。絶縁の有無は個々の部品説明で確認する。
      | 用語3　　　　　　　 ; ADC：Analog-to-Digital Converter（アナログ・デジタル変換器）。測定電圧をデジタル値へ変換する回路。電流や温度も、センサーで電圧へ変換した後に読み取る。
      | 用語4　　　　　　　 ; IC：Integrated Circuit（集積回路）。複数の電子素子と機能を小さな半導体チップに集積した部品。
      | 用語5　　　　　　　 ; CH：Channel（測定チャネル）。CH0〜CH7はADCの入力番号であり、同時測定を意味しない。
      | 用語6　　　　　　　 ; MOSFET：Metal-Oxide-Semiconductor Field-Effect Transistor（金属・酸化膜・半導体構造の電界効果トランジスタ）。ゲートとソースの電圧でドレインとソースの導通を制御する素子。N-MOSはNチャネル型を表す。
      | 用語7　　　　　　　 ; LiFePO4：Lithium Iron Phosphate（リン酸鉄リチウム）。電池の正極材料を示す化学式。英語の頭文字を並べた略語ではない。
      | 用語8　　　　　　　 ; GND：Ground（回路の基準電位・電流帰路）。この図の共通基準。保護接地や大地への接続を意味するとは限らない。
      | 用語9　　　　　　　 ; AGND：Analog Ground（アナログ回路の基準端子）。アナログ部分の電流帰路。現図では共通GNDへ接続されるが、実装時の電流経路への配慮は別途必要。
      | 用語10　　　　　　　; DGND：Digital Ground（デジタル回路の基準端子）。デジタル部分の電流帰路。現図では共通GNDへ接続される。
      | 用語11　　　　　　　; VREF/REF：基準電圧を表す端子名。REFはReference（基準）の意味。ADCの変換尺度や電流アンプの出力基準に使う。REF1/REF2の接続電位は個別に確認する。
      | 用語12　　　　　　　; VCC/VDD/VEE/VS：ICの電源端子名。文字の歴史的な由来を現在の接続機能へ当てはめない。現回路のVEEはU8/U10では浮動基準SW、U9ではGND。各電圧・基準は端子と接続を参照する。
      | 用語13　　　　　　　; GNDP：U10の一次側電源の基準端子。絶縁電源の入力側GND。二次側基準VEE=SWと直接同一の導体ではない。
      | 用語14　　　　　　　; SW：Switching Node（スイッチング点）。主電力段の上下MOSFETとL1がつながる、電圧が高速に切り替わる点。GNDとは別電位。
  GND_Label_017 : ConnectionLabel  Description=|  Label=GND
      | この回路での名前　　; GND
      | 種別　　　　　　　　; ConnectionLabel
      | この回路での役割　　; 電池BT1の負極、太陽電池列の負極、制御・測定・保護回路のGNDを結ぶ共通の帰路。高側駆動の浮動帰路SWとは別のノード。
      | 共通帰路の代表接続　; BT1（充電先の蓄電池／51.2V 100Ah LiFePO4）: -
      |                     ; PV1（直列太陽電池列の負極側パネル／400W panel 1/2）: -
      |                     ; U7（RP2040搭載Pico W／SC0918）: 3(GND), 8(GND), 13(GND), 18(GND), 23(GND), 28(GND), 33(AGND), 38(GND)
      |                     ; U1（外付けADC／MCP3208-CI/SL）: 8(CH7), 9(DGND), 14(AGND)
      |                     ; P_U1（保護MOSFETを制御する保護IC／LTC4364IMS-1#PBF）: GND
      |                     ; Q2（同期整流降圧回路の下側スイッチ／TK9R6E15Q5,S1X）: 3(S)
      |                     ; U9（低側の光ゲートドライバ／ACPL-P346-560E）: 4(VEE)
      |                     ; U10（高側ゲート用の浮動電源を作る絶縁DC/DC／UCC14131QDWNRQ1）: 1(GNDP), 2(GNDP), 5(GNDP), 8(GNDP), 9(GNDP), 10(GNDP), 11(GNDP), 12(GNDP), 13(GNDP), 14(GNDP), 15(GNDP), 16(GNDP), 17(GNDP), 18(GNDP)
      | この場所の直接接続　; C23（PV電流の測定信号を平滑するコンデンサ／100 nF）: 2
      | 直接接続の範囲　　　; このラベルから実際の線・分岐・明示的な境界端子だけを追った接続。同名ラベルによる離れた場所への接続はこの欄に含めない。
      | 同一ネット全端子　　; BT1: -
      |                     ; C1: 2(n)
      |                     ; C2: 2(n)
      |                     ; C3: 2(n)
      |                     ; C4: 2(n)
      |                     ; C7: 2(n)
      |                     ; C8: 2(n)
      |                     ; C9: 2(n)
      |                     ; C10: 2(n)
      |                     ; C13: 2(n)
      |                     ; C14: 2(n)
      |                     ; C15: 2(n)
      |                     ; C16: 2(n)
      |                     ; C17: 2
      |                     ; C18: 2
      |                     ; C19: 2
      |                     ; C20: 2
      |                     ; C21: 2
      |                     ; C22: 2
      |                     ; C23: 2
      |                     ; C24: 2
      |                     ; C25: 2
      |                     ; C26: 2
      |                     ; C27: 2
      |                     ; C28: 2
      |                     ; C29: 2
      |                     ; C30: 2
      |                     ; C31: 2
      |                     ; C33: 2
      |                     ; C34: 2
      |                     ; C35: 2
      |                     ; C36: 2
      |                     ; C40: 2
      |                     ; C41: 2
      |                     ; C42: 2
      |                     ; C43: 2
      |                     ; C44: 2
      |                     ; C45: 2
      |                     ; C46: 2
      |                     ; C47: 2
      |                     ; C48: 2
      |                     ; D2: 2(A)
      |                     ; PV1: -
      |                     ; P_CHG: N
      |                     ; P_COUT: N
      |                     ; P_CTMR: N
      |                     ; P_D1: A
      |                     ; P_R3: 2
      |                     ; P_R8: 2
      |                     ; P_RSHDN_PD: 2
      |                     ; P_U1: GND
      |                     ; Q2: 3(S)
      |                     ; Q3: 1(S1), 4(S2)
      |                     ; R1: 2(n)
      |                     ; R18: 2
      |                     ; R21: 2
      |                     ; R24: 2
      |                     ; R35: 2
      |                     ; R42: 2
      |                     ; R44: 2
      |                     ; R48: 2
      |                     ; U1: 8(CH7), 9(DGND), 14(AGND)
      |                     ; U2: 2(GND), 3(REF2), 4(RESERVED_GND)
      |                     ; U3: 2(GND), 3(REF2), 4(RESERVED_GND)
      |                     ; U4: 3(GND)
      |                     ; U5: 3(GND)
      |                     ; U6: 3(GND)
      |                     ; U7: 3(GND), 8(GND), 13(GND), 18(GND), 23(GND), 28(GND), 33(AGND), 38(GND)
      |                     ; U9: 4(VEE)
      |                     ; U10: 1(GNDP), 2(GNDP), 5(GNDP), 8(GNDP), 9(GNDP), 10(GNDP), 11(GNDP), 12(GNDP), 13(GNDP), 14(GNDP), 15(GNDP), 16(GNDP), 17(GNDP), 18(GNDP)
      |                     ; U11: 2(GND)
      |                     ; U12: 2(GND)
      | 接続部品数　　　　　; 72部品（部品番号で集計。同一ネット全体）
      | 接続端子数　　　　　; 99端子（423端子の部品対応表で集計。ラベル・境界ポートの重複は含めない）
      | この場所の端子数　　; 1端子／1部品（同名ラベルによる接続を除く）
      | 同階層同名ラベル数　; 75個（このラベル自身を含む）
      | 全階層の接続ラベル　; 87個（実際に同じノードへつながるラベル。名前が違う別名も含む）
      | 接続ルール　　　　　; 同じ階層の同じラベル名を仮想配線として結ぶ。別のSubsystem内とは名前だけでつながらず、明示的なConnection Portと配線をたどる。色は用途の表示であり接続を決めない。
      | 確認の範囲　　　　　; 現在の保存回路の端子・配線から求めた静的接続。抵抗やICの内部を導線として短絡せずに集計した。説明の更新は動作シミュレーション、タイミング、実部品の性能・実機動作を保証するものではない。
      | 記録の基準　　　　　; measurement_label_layout_20261022_r01/after_layout_graph.json。部品対応表は端子名の対応付けにのみ使用。
      | 
      | 【この説明欄の略語・記号】
      | 用語1　　　　　　　 ; DC：Direct Current（直流）。ここでは直流電源または直流成分。DCバイアスはコンデンサに重なる直流電圧を指す。
      | 用語2　　　　　　　 ; DC/DC：DC-to-DC Converter（直流電圧変換器）。直流入力を別の直流電圧へ変換する電源回路。絶縁の有無は個々の部品説明で確認する。
      | 用語3　　　　　　　 ; ADC：Analog-to-Digital Converter（アナログ・デジタル変換器）。測定電圧をデジタル値へ変換する回路。電流や温度も、センサーで電圧へ変換した後に読み取る。
      | 用語4　　　　　　　 ; IC：Integrated Circuit（集積回路）。複数の電子素子と機能を小さな半導体チップに集積した部品。
      | 用語5　　　　　　　 ; CH：Channel（測定チャネル）。CH0〜CH7はADCの入力番号であり、同時測定を意味しない。
      | 用語6　　　　　　　 ; MOSFET：Metal-Oxide-Semiconductor Field-Effect Transistor（金属・酸化膜・半導体構造の電界効果トランジスタ）。ゲートとソースの電圧でドレインとソースの導通を制御する素子。N-MOSはNチャネル型を表す。
      | 用語7　　　　　　　 ; LiFePO4：Lithium Iron Phosphate（リン酸鉄リチウム）。電池の正極材料を示す化学式。英語の頭文字を並べた略語ではない。
      | 用語8　　　　　　　 ; PV：Photovoltaic（太陽光発電）。光を電気へ変える発電方式。PVを含むネット名は太陽電池側の測定・電力経路を表す。
      | 用語9　　　　　　　 ; GND：Ground（回路の基準電位・電流帰路）。この図の共通基準。保護接地や大地への接続を意味するとは限らない。
      | 用語10　　　　　　　; AGND：Analog Ground（アナログ回路の基準端子）。アナログ部分の電流帰路。現図では共通GNDへ接続されるが、実装時の電流経路への配慮は別途必要。
      | 用語11　　　　　　　; DGND：Digital Ground（デジタル回路の基準端子）。デジタル部分の電流帰路。現図では共通GNDへ接続される。
      | 用語12　　　　　　　; VREF/REF：基準電圧を表す端子名。REFはReference（基準）の意味。ADCの変換尺度や電流アンプの出力基準に使う。REF1/REF2の接続電位は個別に確認する。
      | 用語13　　　　　　　; VCC/VDD/VEE/VS：ICの電源端子名。文字の歴史的な由来を現在の接続機能へ当てはめない。現回路のVEEはU8/U10では浮動基準SW、U9ではGND。各電圧・基準は端子と接続を参照する。
      | 用語14　　　　　　　; GNDP：U10の一次側電源の基準端子。絶縁電源の入力側GND。二次側基準VEE=SWと直接同一の導体ではない。
      | 用語15　　　　　　　; SW：Switching Node（スイッチング点）。主電力段の上下MOSFETとL1がつながる、電圧が高速に切り替わる点。GNDとは別電位。
  GND_Label_018 : ConnectionLabel  Description=|  Label=GND
      | この回路での名前　　; GND
      | 種別　　　　　　　　; ConnectionLabel
      | この回路での役割　　; 電池BT1の負極、太陽電池列の負極、制御・測定・保護回路のGNDを結ぶ共通の帰路。高側駆動の浮動帰路SWとは別のノード。
      | 共通帰路の代表接続　; BT1（充電先の蓄電池／51.2V 100Ah LiFePO4）: -
      |                     ; PV1（直列太陽電池列の負極側パネル／400W panel 1/2）: -
